simulink model "Hexalock.slx"  (R2026b)
(part 2 of 5)

  MultiStateImage8 : CustomWebBlock  LabelPosition=Hide  ShowInitialText=on  Configuration="{\"components\":[{\"name\":\"BackgroundImageComponent\",\"settings\":{\"image\":{\"size\":[0,0],\"src\":\"default\",\"srcOrientation\":\"Right\"},\"position\":[0,0,1,1],\"scaleMode\":\"0\"}},{\"name\":\"MultistateImageStateComponent\",\"settings\":{\"applyDefaults\":true,\"position\":[0,0,1,1],\"states\":[{\"image\":{\"size\":[0.7746478873239436,1],\"src\":\"data:image\\/svg+xml;base64,PHN2ZyB4bWxucz0iaHR0cDovL3d3dy53My5vcmcvMjAwMC9zdmciIHdpZHRoPSIyMjAiIGhlaWdodD0iMjg0IiB2aWV3Qm94PSIwIDAgMjIwIDI4NCIgcm9sZT0iaW1nIiA+Cjx0aXRsZT5IRVhBTE9DSyBtb2R1bGFyIGludGVyZmFjZSBhc3NldDwvdGl0bGU+CjxkZWZzPjwvZGVmcz4KICAgICAgPHJlY3QgeD0iOCIgeT0iOCIgd2lkdGg9IjIwNCIgaGVpZ2h0PSIyNjgiIHJ4PSIxNCIgZmlsbD0iIzExMUMyMiIgc3Ryb2tlPSIjNTM2NjZFIiBzdHJva2Utd2lkdGg9IjIiLz4KICAgICAgPHJlY3QgeD0iMTIiIHk9IjEyIiB3aWR0 ...(+3224 chars)\",\"srcOrientation\":\"Right\"},\"position\":[0,0,1,1],\"value\":[]},{\"image\":{\"size\":[0,0],\"src\":\"data:image\\/svg+xml;base64,PHN2ZyB4bWxucz0iaHR0cDovL3d3dy53My5vcmcvMjAwMC9zdmciIHdpZHRoPSIyMjAiIGhlaWdodD0iMjg0IiB2aWV3Qm94PSIwIDAgMjIwIDI4NCIgcm9sZT0iaW1nIiA+Cjx0aXRsZT5IRVhBTE9DSyBtb2R1bGFyIGludGVyZmFjZSBhc3NldDwvdGl0bGU+CjxkZWZzPjwvZGVmcz4KICAgICAgPHJlY3QgeD0iOCIgeT0iOCIgd2lkdGg9IjIwNCIgaGVpZ2h0PSIyNjgiIHJ4PSIxNCIgZmlsbD0iIzExMUMyMiIgc3Ryb2tlPSIjNTM2NjZFIiBzdHJva2Utd2lkdGg9IjIiLz4KICAgICAgPHJlY3QgeD0iMTIiIHk9IjEyIiB3aWR0 ...(+3224 chars)\",\"srcOrientation\":\"Right\"},\"position\":[0,0,1,1],\"value\":\"0\"},{\"image\":{\"size\":[0,0],\"src\":\"data:image\\/svg+xml;base64,PHN2ZyB4bWxucz0iaHR0cDovL3d3dy53My5vcmcvMjAwMC9zdmciIHdpZHRoPSIyMjAiIGhlaWdodD0iMjg0IiB2aWV3Qm94PSIwIDAgMjIwIDI4NCIgcm9sZT0iaW1nIiA+Cjx0aXRsZT5IRVhBTE9DSyBtb2R1bGFyIGludGVyZmFjZSBhc3NldDwvdGl0bGU+CjxkZWZzPjwvZGVmcz4KICAgICAgPHJlY3QgeD0iOCIgeT0iOCIgd2lkdGg9IjIwNCIgaGVpZ2h0PSIyNjgiIHJ4PSIxNCIgZmlsbD0iIzExMUMyMiIgc3Ryb2tlPSIjNTM2NjZFIiBzdHJva2Utd2lkdGg9IjIiLz4KICAgICAgPHJlY3QgeD0iMTIiIHk9IjEyIiB3aWR0 ...(+3220 chars)\",\"srcOrientation\":\"Right\"},\"position\":[0,0,1,1],\"value\":\"1\"},{\"image\":{\"size\":[0,0],\"src\":\"data:image\\/svg+xml;base64,PHN2ZyB4bWxucz0iaHR0cDovL3d3dy53My5vcmcvMjAwMC9zdmciIHdpZHRoPSIyMjAiIGhlaWdodD0iMjg0IiB2aWV3Qm94PSIwIDAgMjIwIDI4NCIgcm9sZT0iaW1nIiA+Cjx0aXRsZT5IRVhBTE9DSyBtb2R1bGFyIGludGVyZmFjZSBhc3NldDwvdGl0bGU+CjxkZWZzPjwvZGVmcz4KICAgICAgPHJlY3QgeD0iOCIgeT0iOCIgd2lkdGg9IjIwNCIgaGVpZ2h0PSIyNjgiIHJ4PSIxNCIgZmlsbD0iIzExMUMyMiIgc3Ryb2tlPSIjQjk4NTZFIiBzdHJva2Utd2lkdGg9IjIuNiIvPgogICAgICA8cmVjdCB4PSIxMiIgeT0iMTIiIHdp ...(+3488 chars)\",\"srcOrientation\":\"Right\"},\"position\":[0,0,1,1],\"value\":\"2\"},{\"image\":{\"size\":[0,0],\"src\":\"data:image\\/svg+xml;base64,PHN2ZyB4bWxucz0iaHR0cDovL3d3dy53My5vcmcvMjAwMC9zdmciIHdpZHRoPSIyMjAiIGhlaWdodD0iMjg0IiB2aWV3Qm94PSIwIDAgMjIwIDI4NCIgcm9sZT0iaW1nIiA+Cjx0aXRsZT5IRVhBTE9DSyBtb2R1bGFyIGludGVyZmFjZSBhc3NldDwvdGl0bGU+CjxkZWZzPjwvZGVmcz4KICAgICAgPHJlY3QgeD0iOCIgeT0iOCIgd2lkdGg9IjIwNCIgaGVpZ2h0PSIyNjgiIHJ4PSIxNCIgZmlsbD0iIzExMUMyMiIgc3Ryb2tlPSIjQjk4NTZFIiBzdHJva2Utd2lkdGg9IjIuNiIvPgogICAgICA8cmVjdCB4PSIxMiIgeT0iMTIiIHdp ...(+3484 chars)\",\"srcOrientation\":\"Right\"},\"position\":[0,0,1,1],\"value\":\"3\"},{\"image\":{\"size\":[0,0],\"src\":\"data:image\\/svg+xml;base64,PHN2ZyB4bWxucz0iaHR0cDovL3d3dy53My5vcmcvMjAwMC9zdmciIHdpZHRoPSIyMjAiIGhlaWdodD0iMjg0IiB2aWV3Qm94PSIwIDAgMjIwIDI4NCIgcm9sZT0iaW1nIiA+Cjx0aXRsZT5IRVhBTE9DSyBtb2R1bGFyIGludGVyZmFjZSBhc3NldDwvdGl0bGU+CjxkZWZzPjwvZGVmcz4KICAgICAgPHJlY3QgeD0iOCIgeT0iOCIgd2lkdGg9IjIwNCIgaGVpZ2h0PSIyNjgiIHJ4PSIxNCIgZmlsbD0iIzExMUMyMiIgc3Ryb2tlPSIjQjk4NTZFIiBzdHJva2Utd2lkdGg9IjIuNiIvPgogICAgICA8cmVjdCB4PSIxMiIgeT0iMTIiIHdp ...(+3532 chars)\",\"srcOrientation\":\"Right\"},\"position\":[0,0,1,1],\"value\":\"4\"},{\"image\":{\"size\":[0,0],\"src\":\"data:image\\/svg+xml;base64,PHN2ZyB4bWxucz0iaHR0cDovL3d3dy53My5vcmcvMjAwMC9zdmciIHdpZHRoPSIyMjAiIGhlaWdodD0iMjg0IiB2aWV3Qm94PSIwIDAgMjIwIDI4NCIgcm9sZT0iaW1nIiA+Cjx0aXRsZT5IRVhBTE9DSyBtb2R1bGFyIGludGVyZmFjZSBhc3NldDwvdGl0bGU+CjxkZWZzPjwvZGVmcz4KICAgICAgPHJlY3QgeD0iOCIgeT0iOCIgd2lkdGg9IjIwNCIgaGVpZ2h0PSIyNjgiIHJ4PSIxNCIgZmlsbD0iIzExMUMyMiIgc3Ryb2tlPSIjQjk4NTZFIiBzdHJva2Utd2lkdGg9IjIuNiIvPgogICAgICA8cmVjdCB4PSIxMiIgeT0iMTIiIHdp ...(+3532 chars)\",\"srcOrientation\":\"Right\"},\"position\":[0,0,1,1],\"value\":\"5\"},{\"image\":{\"size\":[0,0],\"src\":\"data:image\\/svg+xml;base64,PHN2ZyB4bWxucz0iaHR0cDovL3d3dy53My5vcmcvMjAwMC9zdmciIHdpZHRoPSIyMjAiIGhlaWdodD0iMjg0IiB2aWV3Qm94PSIwIDAgMjIwIDI4NCIgcm9sZT0iaW1nIiA+Cjx0aXRsZT5IRVhBTE9DSyBtb2R1bGFyIGludGVyZmFjZSBhc3NldDwvdGl0bGU+CjxkZWZzPjwvZGVmcz4KICAgICAgPHJlY3QgeD0iOCIgeT0iOCIgd2lkdGg9IjIwNCIgaGVpZ2h0PSIyNjgiIHJ4PSIxNCIgZmlsbD0iIzExMUMyMiIgc3Ryb2tlPSIjQjk4NTZFIiBzdHJva2Utd2lkdGg9IjIuNiIvPgogICAgICA8cmVjdCB4PSIxMiIgeT0iMTIiIHdp ...(+3532 chars)\",\"srcOrientation\":\"Right\"},\"position\":[0,0,1,1],\"value\":\"6\"},{\"image\":{\"size\":[0,0],\"src\":\"data:image\\/svg+xml;base64,PHN2ZyB4bWxucz0iaHR0cDovL3d3dy53My5vcmcvMjAwMC9zdmciIHdpZHRoPSIyMjAiIGhlaWdodD0iMjg0IiB2aWV3Qm94PSIwIDAgMjIwIDI4NCIgcm9sZT0iaW1nIiA+Cjx0aXRsZT5IRVhBTE9DSyBtb2R1bGFyIGludGVyZmFjZSBhc3NldDwvdGl0bGU+CjxkZWZzPjwvZGVmcz4KICAgICAgPHJlY3QgeD0iOCIgeT0iOCIgd2lkdGg9IjIwNCIgaGVpZ2h0PSIyNjgiIHJ4PSIxNCIgZmlsbD0iIzExMUMyMiIgc3Ryb2tlPSIjQjk4NTZFIiBzdHJva2Utd2lkdGg9IjIuNiIvPgogICAgICA8cmVjdCB4PSIxMiIgeT0iMTIiIHdp ...(+3524 chars)\",\"srcOrientation\":\"Right\"},\"position\":[0,0,1,1],\"value\":\"7\"},{\"image\":{\"size\":[0,0],\"src\":\"data:image\\/svg+xml;base64,PHN2ZyB4bWxucz0iaHR0cDovL3d3dy53My5vcmcvMjAwMC9zdmciIHdpZHRoPSIyMjAiIGhlaWdodD0iMjg0IiB2aWV3Qm94PSIwIDAgMjIwIDI4NCIgcm9sZT0iaW1nIiA+Cjx0aXRsZT5IRVhBTE9DSyBtb2R1bGFyIGludGVyZmFjZSBhc3NldDwvdGl0bGU+CjxkZWZzPjwvZGVmcz4KICAgICAgPHJlY3QgeD0iOCIgeT0iOCIgd2lkdGg9IjIwNCIgaGVpZ2h0PSIyNjgiIHJ4PSIxNCIgZmlsbD0iIzExMUMyMiIgc3Ryb2tlPSIjQjk4NTZFIiBzdHJva2Utd2lkdGg9IjIuNiIvPgogICAgICA8cmVjdCB4PSIxMiIgeT0iMTIiIHdp ...(+3532 chars)\",\"srcOrientation\":\"Right\"},\"position\":[0,0,1,1],\"value\":\"8\"},{\"image\":{\"size\":[0,0],\"src\":\"data:image\\/svg+xml;base64,PHN2ZyB4bWxucz0iaHR0cDovL3d3dy53My5vcmcvMjAwMC9zdmciIHdpZHRoPSIyMjAiIGhlaWdodD0iMjg0IiB2aWV3Qm94PSIwIDAgMjIwIDI4NCIgcm9sZT0iaW1nIiA+Cjx0aXRsZT5IRVhBTE9DSyBtb2R1bGFyIGludGVyZmFjZSBhc3NldDwvdGl0bGU+CjxkZWZzPjwvZGVmcz4KICAgICAgPHJlY3QgeD0iOCIgeT0iOCIgd2lkdGg9IjIwNCIgaGVpZ2h0PSIyNjgiIHJ4PSIxNCIgZmlsbD0iIzExMUMyMiIgc3Ryb2tlPSIjQjk4NTZFIiBzdHJva2Utd2lkdGg9IjIuNiIvPgogICAgICA8cmVjdCB4PSIxMiIgeT0iMTIiIHdp ...(+3532 chars)\",\"srcOrientation\":\"Right\"},\"position\":[0,0,1,1],\"value\":\"9\"},{\"image\":{\"size\":[0,0],\"src\":\"data:image\\/svg+xml;base64,PHN2ZyB4bWxucz0iaHR0cDovL3d3dy53My5vcmcvMjAwMC9zdmciIHdpZHRoPSIyMjAiIGhlaWdodD0iMjg0IiB2aWV3Qm94PSIwIDAgMjIwIDI4NCIgcm9sZT0iaW1nIiA+Cjx0aXRsZT5IRVhBTE9DSyBtb2R1bGFyIGludGVyZmFjZSBhc3NldDwvdGl0bGU+CjxkZWZzPjwvZGVmcz4KICAgICAgPHJlY3QgeD0iOCIgeT0iOCIgd2lkdGg9IjIwNCIgaGVpZ2h0PSIyNjgiIHJ4PSIxNCIgZmlsbD0iIzExMUMyMiIgc3Ryb2tlPSIjQjk4NTZFIiBzdHJva2Utd2lkdGg9IjIuNiIvPgogICAgICA8cmVjdCB4PSIxMiIgeT0iMTIiIHdp ...(+3532 chars)\",\"srcOrientation\":\"Right\"},\"position\":[0,0,1,1],\"value\":\"10\"},{\"image\":{\"size\":[0,0],\"src\":\"data:image\\/svg+xml;base64,PHN2ZyB4bWxucz0iaHR0cDovL3d3dy53My5vcmcvMjAwMC9zdmciIHdpZHRoPSIyMjAiIGhlaWdodD0iMjg0IiB2aWV3Qm94PSIwIDAgMjIwIDI4NCIgcm9sZT0iaW1nIiA+Cjx0aXRsZT5IRVhBTE9DSyBtb2R1bGFyIGludGVyZmFjZSBhc3NldDwvdGl0bGU+CjxkZWZzPjwvZGVmcz4KICAgICAgPHJlY3QgeD0iOCIgeT0iOCIgd2lkdGg9IjIwNCIgaGVpZ2h0PSIyNjgiIHJ4PSIxNCIgZmlsbD0iIzExMUMyMiIgc3Ryb2tlPSIjNTM2NjZFIiBzdHJva2Utd2lkdGg9IjIiLz4KICAgICAgPHJlY3QgeD0iMTIiIHk9IjEyIiB3aWR0 ...(+3220 chars)\",\"srcOrientation\":\"Right\"},\"position\":[0,0,1,1],\"value\":\"11\"},{\"image\":{\"size\":[0,0],\"src\":\"data:image\\/svg+xml;base64,PHN2ZyB4bWxucz0iaHR0cDovL3d3dy53My5vcmcvMjAwMC9zdmciIHdpZHRoPSIyMjAiIGhlaWdodD0iMjg0IiB2aWV3Qm94PSIwIDAgMjIwIDI4NCIgcm9sZT0iaW1nIiA+Cjx0aXRsZT5IRVhBTE9DSyBtb2R1bGFyIGludGVyZmFjZSBhc3NldDwvdGl0bGU+CjxkZWZzPjxsaW5lYXJHcmFkaWVudCBpZD0ia3JhZnRGcm9udCIgeDE9IjAiIHkxPSIwIiB4Mj0iMSIgeTI9IjEiPjxzdG9wIHN0b3AtY29sb3I9IiNEM0I5OUEiLz48c3RvcCBvZmZzZXQ9IjEiIHN0b3AtY29sb3I9IiNBMzgzNjMiLz48L2xpbmVhckdyYWRpZW50Pjxs ...(+4752 chars)\",\"srcOrientation\":\"Right\"},\"position\":[0,0,1,1],\"value\":\"20\"},{\"image\":{\"size\":[0,0],\"src\":\"data:image\\/svg+xml;base64,PHN2ZyB4bWxucz0iaHR0cDovL3d3dy53My5vcmcvMjAwMC9zdmciIHdpZHRoPSIyMjAiIGhlaWdodD0iMjg0IiB2aWV3Qm94PSIwIDAgMjIwIDI4NCIgcm9sZT0iaW1nIiA+Cjx0aXRsZT5IRVhBTE9DSyBtb2R1bGFyIGludGVyZmFjZSBhc3NldDwvdGl0bGU+CjxkZWZzPjxsaW5lYXJHcmFkaWVudCBpZD0ia3JhZnRGcm9udCIgeDE9IjAiIHkxPSIwIiB4Mj0iMSIgeTI9IjEiPjxzdG9wIHN0b3AtY29sb3I9IiNEM0I5OUEiLz48c3RvcCBvZmZzZXQ9IjEiIHN0b3AtY29sb3I9IiNBMzgzNjMiLz48L2xpbmVhckdyYWRpZW50Pjxs ...(+7264 chars)\",\"srcOrientation\":\"Right\"},\"position\":[0,0,1,1],\"value\":\"21\"},{\"image\":{\"size\":[0,0],\"src\":\"data:image\\/svg+xml;base64,PHN2ZyB4bWxucz0iaHR0cDovL3d3dy53My5vcmcvMjAwMC9zdmciIHdpZHRoPSIyMjAiIGhlaWdodD0iMjg0IiB2aWV3Qm94PSIwIDAgMjIwIDI4NCIgcm9sZT0iaW1nIiA+Cjx0aXRsZT5IRVhBTE9DSyBtb2R1bGFyIGludGVyZmFjZSBhc3NldDwvdGl0bGU+CjxkZWZzPjxsaW5lYXJHcmFkaWVudCBpZD0ia3JhZnRGcm9udCIgeDE9IjAiIHkxPSIwIiB4Mj0iMSIgeTI9IjEiPjxzdG9wIHN0b3AtY29sb3I9IiNEM0I5OUEiLz48c3RvcCBvZmZzZXQ9IjEiIHN0b3AtY29sb3I9IiNBMzgzNjMiLz48L2xpbmVhckdyYWRpZW50Pjxs ...(+7264 chars)\",\"srcOrientation\":\"Right\"},\"position\":[0,0,1,1],\"value\":\"22\"},{\"image\":{\"size\":[0,0],\"src\":\"data:image\\/svg+xml;base64,PHN2ZyB4bWxucz0iaHR0cDovL3d3dy53My5vcmcvMjAwMC9zdmciIHdpZHRoPSIyMjAiIGhlaWdodD0iMjg0IiB2aWV3Qm94PSIwIDAgMjIwIDI4NCIgcm9sZT0iaW1nIiA+Cjx0aXRsZT5IRVhBTE9DSyBtb2R1bGFyIGludGVyZmFjZSBhc3NldDwvdGl0bGU+CjxkZWZzPjxsaW5lYXJHcmFkaWVudCBpZD0ia3JhZnRGcm9udCIgeDE9IjAiIHkxPSIwIiB4Mj0iMSIgeTI9IjEiPjxzdG9wIHN0b3AtY29sb3I9IiNEM0I5OUEiLz48c3RvcCBvZmZzZXQ9IjEiIHN0b3AtY29sb3I9IiNBMzgzNjMiLz48L2xpbmVhckdyYWRpZW50Pjxs ...(+7264 chars)\",\"srcOrientation\":\"Right\"},\"position\":[0,0,1,1],\"value\":\"23\"},{\"image\":{\"size\":[0,0],\"src\":\"data:image\\/svg+xml;base64,PHN2ZyB4bWxucz0iaHR0cDovL3d3dy53My5vcmcvMjAwMC9zdmciIHdpZHRoPSIyMjAiIGhlaWdodD0iMjg0IiB2aWV3Qm94PSIwIDAgMjIwIDI4NCIgcm9sZT0iaW1nIiA+Cjx0aXRsZT5IRVhBTE9DSyBtb2R1bGFyIGludGVyZmFjZSBhc3NldDwvdGl0bGU+CjxkZWZzPjxsaW5lYXJHcmFkaWVudCBpZD0ia3JhZnRGcm9udCIgeDE9IjAiIHkxPSIwIiB4Mj0iMSIgeTI9IjEiPjxzdG9wIHN0b3AtY29sb3I9IiNEM0I5OUEiLz48c3RvcCBvZmZzZXQ9IjEiIHN0b3AtY29sb3I9IiNBMzgzNjMiLz48L2xpbmVhckdyYWRpZW50Pjxs ...(+7260 chars)\",\"srcOrientation\":\"Right\"},\"position\":[0,0,1,1],\"value\":\"24\"},{\"image\":{\"size\":[0,0],\"src\":\"data:image\\/svg+xml;base64,PHN2ZyB4bWxucz0iaHR0cDovL3d3dy53My5vcmcvMjAwMC9zdmciIHdpZHRoPSIyMjAiIGhlaWdodD0iMjg0IiB2aWV3Qm94PSIwIDAgMjIwIDI4NCIgcm9sZT0iaW1nIiA+Cjx0aXRsZT5IRVhBTE9DSyBtb2R1bGFyIGludGVyZmFjZSBhc3NldDwvdGl0bGU+CjxkZWZzPjxsaW5lYXJHcmFkaWVudCBpZD0ia3JhZnRGcm9udCIgeDE9IjAiIHkxPSIwIiB4Mj0iMSIgeTI9IjEiPjxzdG9wIHN0b3AtY29sb3I9IiNEM0I5OUEiLz48c3RvcCBvZmZzZXQ9IjEiIHN0b3AtY29sb3I9IiNBMzgzNjMiLz48L2xpbmVhckdyYWRpZW50Pjxs ...(+7264 chars)\",\"srcOrientation\":\"Right\"},\"position\":[0,0,1,1],\"value\":\"25\"},{\"image\":{\"size\":[0,0],\"src\":\"data:image\\/svg+xml;base64,PHN2ZyB4bWxucz0iaHR0cDovL3d3dy53My5vcmcvMjAwMC9zdmciIHdpZHRoPSIyMjAiIGhlaWdodD0iMjg0IiB2aWV3Qm94PSIwIDAgMjIwIDI4NCIgcm9sZT0iaW1nIiA+Cjx0aXRsZT5IRVhBTE9DSyBtb2R1bGFyIGludGVyZmFjZSBhc3NldDwvdGl0bGU+CjxkZWZzPjxsaW5lYXJHcmFkaWVudCBpZD0ia3JhZnRGcm9udCIgeDE9IjAiIHkxPSIwIiB4Mj0iMSIgeTI9IjEiPjxzdG9wIHN0b3AtY29sb3I9IiNEM0I5OUEiLz48c3RvcCBvZmZzZXQ9IjEiIHN0b3AtY29sb3I9IiNBMzgzNjMiLz48L2xpbmVhckdyYWRpZW50Pjxs ...(+7272 chars)\",\"srcOrientation\":\"Right\"},\"position\":[0,0,1,1],\"value\":\"26\"},{\"image\":{\"size\":[0,0],\"src\":\"data:image\\/svg+xml;base64,PHN2ZyB4bWxucz0iaHR0cDovL3d3dy53My5vcmcvMjAwMC9zdmciIHdpZHRoPSIyMjAiIGhlaWdodD0iMjg0IiB2aWV3Qm94PSIwIDAgMjIwIDI4NCIgcm9sZT0iaW1nIiA+Cjx0aXRsZT5IRVhBTE9DSyBtb2R1bGFyIGludGVyZmFjZSBhc3NldDwvdGl0bGU+CjxkZWZzPjxsaW5lYXJHcmFkaWVudCBpZD0ia3JhZnRGcm9udCIgeDE9IjAiIHkxPSIwIiB4Mj0iMSIgeTI9IjEiPjxzdG9wIHN0b3AtY29sb3I9IiNEM0I5OUEiLz48c3RvcCBvZmZzZXQ9IjEiIHN0b3AtY29sb3I9IiNBMzgzNjMiLz48L2xpbmVhckdyYWRpZW50Pjxs ...(+7264 chars)\",\"srcOrientation\":\"Right\"},\"position\":[0,0,1,1],\"value\":\"27\"},{\"image\":{\"size\":[0,0],\"src\":\"data:image\\/svg+xml;base64,PHN2ZyB4bWxucz0iaHR0cDovL3d3dy53My5vcmcvMjAwMC9zdmciIHdpZHRoPSIyMjAiIGhlaWdodD0iMjg0IiB2aWV3Qm94PSIwIDAgMjIwIDI4NCIgcm9sZT0iaW1nIiA+Cjx0aXRsZT5IRVhBTE9DSyBtb2R1bGFyIGludGVyZmFjZSBhc3NldDwvdGl0bGU+CjxkZWZzPjxsaW5lYXJHcmFkaWVudCBpZD0ia3JhZnRGcm9udCIgeDE9IjAiIHkxPSIwIiB4Mj0iMSIgeTI9IjEiPjxzdG9wIHN0b3AtY29sb3I9IiNEM0I5OUEiLz48c3RvcCBvZmZzZXQ9IjEiIHN0b3AtY29sb3I9IiNBMzgzNjMiLz48L2xpbmVhckdyYWRpZW50Pjxs ...(+7268 chars)\",\"srcOrientation\":\"Right\"},\"position\":[0,0,1,1],\"value\":\"28\"},{\"image\":{\"size\":[0,0],\"src\":\"data:image\\/svg+xml;base64,PHN2ZyB4bWxucz0iaHR0cDovL3d3dy53My5vcmcvMjAwMC9zdmciIHdpZHRoPSIyMjAiIGhlaWdodD0iMjg0IiB2aWV3Qm94PSIwIDAgMjIwIDI4NCIgcm9sZT0iaW1nIiA+Cjx0aXRsZT5IRVhBTE9DSyBtb2R1bGFyIGludGVyZmFjZSBhc3NldDwvdGl0bGU+CjxkZWZzPjxsaW5lYXJHcmFkaWVudCBpZD0ia3JhZnRGcm9udCIgeDE9IjAiIHkxPSIwIiB4Mj0iMSIgeTI9IjEiPjxzdG9wIHN0b3AtY29sb3I9IiNEM0I5OUEiLz48c3RvcCBvZmZzZXQ9IjEiIHN0b3AtY29sb3I9IiNBMzgzNjMiLz48L2xpbmVhckdyYWRpZW50Pjxs ...(+7268 chars)\",\"srcOrientation\":\"Right\"},\"position\":[0,0,1,1],\"value\":\"29\"},{\"image\":{\"size\":[0,0],\"src\":\"data:image\\/svg+xml;base64,PHN2ZyB4bWxucz0iaHR0cDovL3d3dy53My5vcmcvMjAwMC9zdmciIHdpZHRoPSIyMjAiIGhlaWdodD0iMjg0IiB2aWV3Qm94PSIwIDAgMjIwIDI4NCIgcm9sZT0iaW1nIiA+Cjx0aXRsZT5IRVhBTE9DSyBtb2R1bGFyIGludGVyZmFjZSBhc3NldDwvdGl0bGU+CjxkZWZzPjxsaW5lYXJHcmFkaWVudCBpZD0ia3JhZnRGcm9udCIgeDE9IjAiIHkxPSIwIiB4Mj0iMSIgeTI9IjEiPjxzdG9wIHN0b3AtY29sb3I9IiNEM0I5OUEiLz48c3RvcCBvZmZzZXQ9IjEiIHN0b3AtY29sb3I9IiNBMzgzNjMiLz48L2xpbmVhckdyYWRpZW50Pjxs ...(+7268 chars)\",\"srcOrientation\":\"Right\"},\"position\":[0,0,1,1],\"value\":\"30\"},{\"image\":{\"size\":[0,0],\"src\":\"data:image\\/svg+xml;base64,PHN2ZyB4bWxucz0iaHR0cDovL3d3dy53My5vcmcvMjAwMC9zdmciIHdpZHRoPSIyMjAiIGhlaWdodD0iMjg0IiB2aWV3Qm94PSIwIDAgMjIwIDI4NCIgcm9sZT0iaW1nIiA+Cjx0aXRsZT5IRVhBTE9DSyBtb2R1bGFyIGludGVyZmFjZSBhc3NldDwvdGl0bGU+CjxkZWZzPjxsaW5lYXJHcmFkaWVudCBpZD0ia3JhZnRGcm9udCIgeDE9IjAiIHkxPSIwIiB4Mj0iMSIgeTI9IjEiPjxzdG9wIHN0b3AtY29sb3I9IiNEM0I5OUEiLz48c3RvcCBvZmZzZXQ9IjEiIHN0b3AtY29sb3I9IiNBMzgzNjMiLz48L2xpbmVhckdyYWRpZW50Pjxs ...(+4756 chars)\",\"srcOrientation\":\"Right\"},\"position\":[0,0,1,1],\"value\":\"31\"},{\"image\":{\"size\":[0,0],\"src\":\"data:image\\/svg+xml;base64,PHN2ZyB4bWxucz0iaHR0cDovL3d3dy53My5vcmcvMjAwMC9zdmciIHdpZHRoPSIyMjAiIGhlaWdodD0iMjg0IiB2aWV3Qm94PSIwIDAgMjIwIDI4NCIgcm9sZT0iaW1nIiA+Cjx0aXRsZT5IRVhBTE9DSyBtb2R1bGFyIGludGVyZmFjZSBhc3NldDwvdGl0bGU+CjxkZWZzPjxsaW5lYXJHcmFkaWVudCBpZD0ia3JhZnRGcm9udCIgeDE9IjAiIHkxPSIwIiB4Mj0iMSIgeTI9IjEiPjxzdG9wIHN0b3AtY29sb3I9IiNEM0I5OUEiLz48c3RvcCBvZmZzZXQ9IjEiIHN0b3AtY29sb3I9IiNBMzgzNjMiLz48L2xpbmVhckdyYWRpZW50Pjxs ...(+4752 chars)\",\"srcOrientation\":\"Right\"},\"position\":[0,0,1,1],\"value\":\"32\"},{\"image\":{\"size\":[0,0],\"src\":\"data:image\\/svg+xml;base64,PHN2ZyB4bWxucz0iaHR0cDovL3d3dy53My5vcmcvMjAwMC9zdmciIHdpZHRoPSIyMjAiIGhlaWdodD0iMjg0IiB2aWV3Qm94PSIwIDAgMjIwIDI4NCIgcm9sZT0iaW1nIiA+Cjx0aXRsZT5IRVhBTE9DSyBtb2R1bGFyIGludGVyZmFjZSBhc3NldDwvdGl0bGU+CjxkZWZzPjxsaW5lYXJHcmFkaWVudCBpZD0ia3JhZnRGcm9udCIgeDE9IjAiIHkxPSIwIiB4Mj0iMSIgeTI9IjEiPjxzdG9wIHN0b3AtY29sb3I9IiNEM0I5OUEiLz48c3RvcCBvZmZzZXQ9IjEiIHN0b3AtY29sb3I9IiNBMzgzNjMiLz48L2xpbmVhckdyYWRpZW50Pjxs ...(+6860 chars)\",\"srcOrientation\":\"Right\"},\"position\":[0,0,1,1],\"value\":\"33\"},{\"image\":{\"size\":[0,0],\"src\":\"data:image\\/svg+xml;base64,PHN2ZyB4bWxucz0iaHR0cDovL3d3dy53My5vcmcvMjAwMC9zdmciIHdpZHRoPSIyMjAiIGhlaWdodD0iMjg0IiB2aWV3Qm94PSIwIDAgMjIwIDI4NCIgcm9sZT0iaW1nIiA+Cjx0aXRsZT5IRVhBTE9DSyBtb2R1bGFyIGludGVyZmFjZSBhc3NldDwvdGl0bGU+CjxkZWZzPjxsaW5lYXJHcmFkaWVudCBpZD0ia3JhZnRGcm9udCIgeDE9IjAiIHkxPSIwIiB4Mj0iMSIgeTI9IjEiPjxzdG9wIHN0b3AtY29sb3I9IiNEM0I5OUEiLz48c3RvcCBvZmZzZXQ9IjEiIHN0b3AtY29sb3I9IiNBMzgzNjMiLz48L2xpbmVhckdyYWRpZW50Pjxs ...(+6860 chars)\",\"srcOrientation\":\"Right\"},\"position\":[0,0,1,1],\"value\":\"34\"},{\"image\":{\"size\":[0,0],\"src\":\"data:image\\/svg+xml;base64,PHN2ZyB4bWxucz0iaHR0cDovL3d3dy53My5vcmcvMjAwMC9zdmciIHdpZHRoPSIyMjAiIGhlaWdodD0iMjg0IiB2aWV3Qm94PSIwIDAgMjIwIDI4NCIgcm9sZT0iaW1nIiA+Cjx0aXRsZT5IRVhBTE9DSyBtb2R1bGFyIGludGVyZmFjZSBhc3NldDwvdGl0bGU+CjxkZWZzPjxsaW5lYXJHcmFkaWVudCBpZD0ia3JhZnRGcm9udCIgeDE9IjAiIHkxPSIwIiB4Mj0iMSIgeTI9IjEiPjxzdG9wIHN0b3AtY29sb3I9IiNEM0I5OUEiLz48c3RvcCBvZmZzZXQ9IjEiIHN0b3AtY29sb3I9IiNBMzgzNjMiLz48L2xpbmVhckdyYWRpZW50Pjxs ...(+6860 chars)\",\"srcOrientation\":\"Right\"},\"position\":[0,0,1,1],\"value\":\"35\"},{\"image\":{\"size\":[0,0],\"src\":\"data:image\\/svg+xml;base64,PHN2ZyB4bWxucz0iaHR0cDovL3d3dy53My5vcmcvMjAwMC9zdmciIHdpZHRoPSIyMjAiIGhlaWdodD0iMjg0IiB2aWV3Qm94PSIwIDAgMjIwIDI4NCIgcm9sZT0iaW1nIiA+DQo8dGl0bGU+SEVYQUxPQ0sgbW9kdWxhciBpbnRlcmZhY2UgYXNzZXQ8L3RpdGxlPg0KPGRlZnM+PGxpbmVhckdyYWRpZW50IGlkPSJrcmFmdEZyb250IiB4MT0iMCIgeTE9IjAiIHgyPSIxIiB5Mj0iMSI+PHN0b3Agc3RvcC1jb2xvcj0iI0QzQjk5QSIvPjxzdG9wIG9mZnNldD0iMSIgc3RvcC1jb2xvcj0iI0EzODM2MyIvPjwvbGluZWFyR3JhZGllbnQ+ ...(+6912 chars)\",\"srcOrientation\":\"Right\"},\"position\":[0,0,1,1],\"value\":\"36\"},{\"image\":{\"size\":[0,0],\"src\":\"data:image\\/svg+xml;base64,PHN2ZyB4bWxucz0iaHR0cDovL3d3dy53My5vcmcvMjAwMC9zdmciIHdpZHRoPSIyMjAiIGhlaWdodD0iMjg0IiB2aWV3Qm94PSIwIDAgMjIwIDI4NCIgcm9sZT0iaW1nIiA+DQo8dGl0bGU+SEVYQUxPQ0sgbW9kdWxhciBpbnRlcmZhY2UgYXNzZXQ8L3RpdGxlPg0KPGRlZnM+PGxpbmVhckdyYWRpZW50IGlkPSJrcmFmdEZyb250IiB4MT0iMCIgeTE9IjAiIHgyPSIxIiB5Mj0iMSI+PHN0b3Agc3RvcC1jb2xvcj0iI0QzQjk5QSIvPjxzdG9wIG9mZnNldD0iMSIgc3RvcC1jb2xvcj0iI0EzODM2MyIvPjwvbGluZWFyR3JhZGllbnQ+ ...(+6912 chars)\",\"srcOrientation\":\"Right\"},\"position\":[0,0,1,1],\"value\":\"37\"},{\"image\":{\"size\":[0,0],\"src\":\"data:image\\/svg+xml;base64,PHN2ZyB4bWxucz0iaHR0cDovL3d3dy53My5vcmcvMjAwMC9zdmciIHdpZHRoPSIyMjAiIGhlaWdodD0iMjg0IiB2aWV3Qm94PSIwIDAgMjIwIDI4NCIgcm9sZT0iaW1nIiA+DQo8dGl0bGU+SEVYQUxPQ0sgbW9kdWxhciBpbnRlcmZhY2UgYXNzZXQ8L3RpdGxlPg0KPGRlZnM+PGxpbmVhckdyYWRpZW50IGlkPSJrcmFmdEZyb250IiB4MT0iMCIgeTE9IjAiIHgyPSIxIiB5Mj0iMSI+PHN0b3Agc3RvcC1jb2xvcj0iI0QzQjk5QSIvPjxzdG9wIG9mZnNldD0iMSIgc3RvcC1jb2xvcj0iI0EzODM2MyIvPjwvbGluZWFyR3JhZGllbnQ+ ...(+6912 chars)\",\"srcOrientation\":\"Right\"},\"position\":[0,0,1,1],\"value\":\"38\"}],\"valueType\":\"discrete\"}},{\"name\":\"ForegroundImageComponent\",\"settings\":{\"image\":{\"size\":[0,0],\"src\":\"default\",\"srcOrientation\":\"Right\"},\"isForeground\":1,\"position\":[0,0,1,1],\"scaleMode\":\"0\"}}],\"derived\":{\"blockParameters\":{\"DefaultImage\":\"data:image\\/svg+xml;base64,PHN2ZyB4bWxucz0iaHR0cDovL3d3dy53My5vcmcvMjAwMC9zdmciIHdpZHRoPSIyMjAiIGhlaWdodD0iMjg0IiB2aWV3Qm94PSIwIDAgMjIwIDI4NCIgcm9sZT0iaW1nIiA+Cjx0aXRsZT5IRVhBTE9DSyBtb2R1bGFyIGludGVyZmFjZSBhc3NldDwvdGl0bGU+CjxkZWZzPjwvZGVmcz4KICAgICAgPHJlY3QgeD0iOCIgeT0iOCIgd2lkdGg9IjIwNCIgaGVpZ2h0PSIyNjgiIHJ4PSIxNCIgZmlsbD0iIzExMUMyMiIgc3Ryb2tlPSIjNTM2NjZFIiBzdHJva2Utd2lkdGg9IjIiLz4KICAgICAgPHJlY3QgeD0iMTIiIHk9IjEyIiB3aWR0 ...(+3224 chars)\",\"StateValueType\":\"discrete\",\"States\":[{\"image\":\"data:image\\/svg+xml;base64,PHN2ZyB4bWxucz0iaHR0cDovL3d3dy53My5vcmcvMjAwMC9zdmciIHdpZHRoPSIyMjAiIGhlaWdodD0iMjg0IiB2aWV3Qm94PSIwIDAgMjIwIDI4NCIgcm9sZT0iaW1nIiA+Cjx0aXRsZT5IRVhBTE9DSyBtb2R1bGFyIGludGVyZmFjZSBhc3NldDwvdGl0bGU+CjxkZWZzPjwvZGVmcz4KICAgICAgPHJlY3QgeD0iOCIgeT0iOCIgd2lkdGg9IjIwNCIgaGVpZ2h0PSIyNjgiIHJ4PSIxNCIgZmlsbD0iIzExMUMyMiIgc3Ryb2tlPSIjNTM2NjZFIiBzdHJva2Utd2lkdGg9IjIiLz4KICAgICAgPHJlY3QgeD0iMTIiIHk9IjEyIiB3aWR0 ...(+3224 chars)\",\"value\":\"0\"},{\"image\":\"data:image\\/svg+xml;base64,PHN2ZyB4bWxucz0iaHR0cDovL3d3dy53My5vcmcvMjAwMC9zdmciIHdpZHRoPSIyMjAiIGhlaWdodD0iMjg0IiB2aWV3Qm94PSIwIDAgMjIwIDI4NCIgcm9sZT0iaW1nIiA+Cjx0aXRsZT5IRVhBTE9DSyBtb2R1bGFyIGludGVyZmFjZSBhc3NldDwvdGl0bGU+CjxkZWZzPjwvZGVmcz4KICAgICAgPHJlY3QgeD0iOCIgeT0iOCIgd2lkdGg9IjIwNCIgaGVpZ2h0PSIyNjgiIHJ4PSIxNCIgZmlsbD0iIzExMUMyMiIgc3Ryb2tlPSIjNTM2NjZFIiBzdHJva2Utd2lkdGg9IjIiLz4KICAgICAgPHJlY3QgeD0iMTIiIHk9IjEyIiB3aWR0 ...(+3220 chars)\",\"value\":\"1\"},{\"image\":\"data:image\\/svg+xml;base64,PHN2ZyB4bWxucz0iaHR0cDovL3d3dy53My5vcmcvMjAwMC9zdmciIHdpZHRoPSIyMjAiIGhlaWdodD0iMjg0IiB2aWV3Qm94PSIwIDAgMjIwIDI4NCIgcm9sZT0iaW1nIiA+Cjx0aXRsZT5IRVhBTE9DSyBtb2R1bGFyIGludGVyZmFjZSBhc3NldDwvdGl0bGU+CjxkZWZzPjwvZGVmcz4KICAgICAgPHJlY3QgeD0iOCIgeT0iOCIgd2lkdGg9IjIwNCIgaGVpZ2h0PSIyNjgiIHJ4PSIxNCIgZmlsbD0iIzExMUMyMiIgc3Ryb2tlPSIjQjk4NTZFIiBzdHJva2Utd2lkdGg9IjIuNiIvPgogICAgICA8cmVjdCB4PSIxMiIgeT0iMTIiIHdp ...(+3488 chars)\",\"value\":\"2\"},{\"image\":\"data:image\\/svg+xml;base64,PHN2ZyB4bWxucz0iaHR0cDovL3d3dy53My5vcmcvMjAwMC9zdmciIHdpZHRoPSIyMjAiIGhlaWdodD0iMjg0IiB2aWV3Qm94PSIwIDAgMjIwIDI4NCIgcm9sZT0iaW1nIiA+Cjx0aXRsZT5IRVhBTE9DSyBtb2R1bGFyIGludGVyZmFjZSBhc3NldDwvdGl0bGU+CjxkZWZzPjwvZGVmcz4KICAgICAgPHJlY3QgeD0iOCIgeT0iOCIgd2lkdGg9IjIwNCIgaGVpZ2h0PSIyNjgiIHJ4PSIxNCIgZmlsbD0iIzExMUMyMiIgc3Ryb2tlPSIjQjk4NTZFIiBzdHJva2Utd2lkdGg9IjIuNiIvPgogICAgICA8cmVjdCB4PSIxMiIgeT0iMTIiIHdp ...(+3484 chars)\",\"value\":\"3\"},{\"image\":\"data:image\\/svg+xml;base64,PHN2ZyB4bWxucz0iaHR0cDovL3d3dy53My5vcmcvMjAwMC9zdmciIHdpZHRoPSIyMjAiIGhlaWdodD0iMjg0IiB2aWV3Qm94PSIwIDAgMjIwIDI4NCIgcm9sZT0iaW1nIiA+Cjx0aXRsZT5IRVhBTE9DSyBtb2R1bGFyIGludGVyZmFjZSBhc3NldDwvdGl0bGU+CjxkZWZzPjwvZGVmcz4KICAgICAgPHJlY3QgeD0iOCIgeT0iOCIgd2lkdGg9IjIwNCIgaGVpZ2h0PSIyNjgiIHJ4PSIxNCIgZmlsbD0iIzExMUMyMiIgc3Ryb2tlPSIjQjk4NTZFIiBzdHJva2Utd2lkdGg9IjIuNiIvPgogICAgICA8cmVjdCB4PSIxMiIgeT0iMTIiIHdp ...(+3532 chars)\",\"value\":\"4\"},{\"image\":\"data:image\\/svg+xml;base64,PHN2ZyB4bWxucz0iaHR0cDovL3d3dy53My5vcmcvMjAwMC9zdmciIHdpZHRoPSIyMjAiIGhlaWdodD0iMjg0IiB2aWV3Qm94PSIwIDAgMjIwIDI4NCIgcm9sZT0iaW1nIiA+Cjx0aXRsZT5IRVhBTE9DSyBtb2R1bGFyIGludGVyZmFjZSBhc3NldDwvdGl0bGU+CjxkZWZzPjwvZGVmcz4KICAgICAgPHJlY3QgeD0iOCIgeT0iOCIgd2lkdGg9IjIwNCIgaGVpZ2h0PSIyNjgiIHJ4PSIxNCIgZmlsbD0iIzExMUMyMiIgc3Ryb2tlPSIjQjk4NTZFIiBzdHJva2Utd2lkdGg9IjIuNiIvPgogICAgICA8cmVjdCB4PSIxMiIgeT0iMTIiIHdp ...(+3532 chars)\",\"value\":\"5\"},{\"image\":\"data:image\\/svg+xml;base64,PHN2ZyB4bWxucz0iaHR0cDovL3d3dy53My5vcmcvMjAwMC9zdmciIHdpZHRoPSIyMjAiIGhlaWdodD0iMjg0IiB2aWV3Qm94PSIwIDAgMjIwIDI4NCIgcm9sZT0iaW1nIiA+Cjx0aXRsZT5IRVhBTE9DSyBtb2R1bGFyIGludGVyZmFjZSBhc3NldDwvdGl0bGU+CjxkZWZzPjwvZGVmcz4KICAgICAgPHJlY3QgeD0iOCIgeT0iOCIgd2lkdGg9IjIwNCIgaGVpZ2h0PSIyNjgiIHJ4PSIxNCIgZmlsbD0iIzExMUMyMiIgc3Ryb2tlPSIjQjk4NTZFIiBzdHJva2Utd2lkdGg9IjIuNiIvPgogICAgICA8cmVjdCB4PSIxMiIgeT0iMTIiIHdp ...(+3532 chars)\",\"value\":\"6\"},{\"image\":\"data:image\\/svg+xml;base64,PHN2ZyB4bWxucz0iaHR0cDovL3d3dy53My5vcmcvMjAwMC9zdmciIHdpZHRoPSIyMjAiIGhlaWdodD0iMjg0IiB2aWV3Qm94PSIwIDAgMjIwIDI4NCIgcm9sZT0iaW1nIiA+Cjx0aXRsZT5IRVhBTE9DSyBtb2R1bGFyIGludGVyZmFjZSBhc3NldDwvdGl0bGU+CjxkZWZzPjwvZGVmcz4KICAgICAgPHJlY3QgeD0iOCIgeT0iOCIgd2lkdGg9IjIwNCIgaGVpZ2h0PSIyNjgiIHJ4PSIxNCIgZmlsbD0iIzExMUMyMiIgc3Ryb2tlPSIjQjk4NTZFIiBzdHJva2Utd2lkdGg9IjIuNiIvPgogICAgICA8cmVjdCB4PSIxMiIgeT0iMTIiIHdp ...(+3524 chars)\",\"value\":\"7\"},{\"image\":\"data:image\\/svg+xml;base64,PHN2ZyB4bWxucz0iaHR0cDovL3d3dy53My5vcmcvMjAwMC9zdmciIHdpZHRoPSIyMjAiIGhlaWdodD0iMjg0IiB2aWV3Qm94PSIwIDAgMjIwIDI4NCIgcm9sZT0iaW1nIiA+Cjx0aXRsZT5IRVhBTE9DSyBtb2R1bGFyIGludGVyZmFjZSBhc3NldDwvdGl0bGU+CjxkZWZzPjwvZGVmcz4KICAgICAgPHJlY3QgeD0iOCIgeT0iOCIgd2lkdGg9IjIwNCIgaGVpZ2h0PSIyNjgiIHJ4PSIxNCIgZmlsbD0iIzExMUMyMiIgc3Ryb2tlPSIjQjk4NTZFIiBzdHJva2Utd2lkdGg9IjIuNiIvPgogICAgICA8cmVjdCB4PSIxMiIgeT0iMTIiIHdp ...(+3532 chars)\",\"value\":\"8\"},{\"image\":\"data:image\\/svg+xml;base64,PHN2ZyB4bWxucz0iaHR0cDovL3d3dy53My5vcmcvMjAwMC9zdmciIHdpZHRoPSIyMjAiIGhlaWdodD0iMjg0IiB2aWV3Qm94PSIwIDAgMjIwIDI4NCIgcm9sZT0iaW1nIiA+Cjx0aXRsZT5IRVhBTE9DSyBtb2R1bGFyIGludGVyZmFjZSBhc3NldDwvdGl0bGU+CjxkZWZzPjwvZGVmcz4KICAgICAgPHJlY3QgeD0iOCIgeT0iOCIgd2lkdGg9IjIwNCIgaGVpZ2h0PSIyNjgiIHJ4PSIxNCIgZmlsbD0iIzExMUMyMiIgc3Ryb2tlPSIjQjk4NTZFIiBzdHJva2Utd2lkdGg9IjIuNiIvPgogICAgICA8cmVjdCB4PSIxMiIgeT0iMTIiIHdp ...(+3532 chars)\",\"value\":\"9\"},{\"image\":\"data:image\\/svg+xml;base64,PHN2ZyB4bWxucz0iaHR0cDovL3d3dy53My5vcmcvMjAwMC9zdmciIHdpZHRoPSIyMjAiIGhlaWdodD0iMjg0IiB2aWV3Qm94PSIwIDAgMjIwIDI4NCIgcm9sZT0iaW1nIiA+Cjx0aXRsZT5IRVhBTE9DSyBtb2R1bGFyIGludGVyZmFjZSBhc3NldDwvdGl0bGU+CjxkZWZzPjwvZGVmcz4KICAgICAgPHJlY3QgeD0iOCIgeT0iOCIgd2lkdGg9IjIwNCIgaGVpZ2h0PSIyNjgiIHJ4PSIxNCIgZmlsbD0iIzExMUMyMiIgc3Ryb2tlPSIjQjk4NTZFIiBzdHJva2Utd2lkdGg9IjIuNiIvPgogICAgICA8cmVjdCB4PSIxMiIgeT0iMTIiIHdp ...(+3532 chars)\",\"value\":\"10\"},{\"image\":\"data:image\\/svg+xml;base64,PHN2ZyB4bWxucz0iaHR0cDovL3d3dy53My5vcmcvMjAwMC9zdmciIHdpZHRoPSIyMjAiIGhlaWdodD0iMjg0IiB2aWV3Qm94PSIwIDAgMjIwIDI4NCIgcm9sZT0iaW1nIiA+Cjx0aXRsZT5IRVhBTE9DSyBtb2R1bGFyIGludGVyZmFjZSBhc3NldDwvdGl0bGU+CjxkZWZzPjwvZGVmcz4KICAgICAgPHJlY3QgeD0iOCIgeT0iOCIgd2lkdGg9IjIwNCIgaGVpZ2h0PSIyNjgiIHJ4PSIxNCIgZmlsbD0iIzExMUMyMiIgc3Ryb2tlPSIjNTM2NjZFIiBzdHJva2Utd2lkdGg9IjIiLz4KICAgICAgPHJlY3QgeD0iMTIiIHk9IjEyIiB3aWR0 ...(+3220 chars)\",\"value\":\"11\"},{\"image\":\"data:image\\/svg+xml;base64,PHN2ZyB4bWxucz0iaHR0cDovL3d3dy53My5vcmcvMjAwMC9zdmciIHdpZHRoPSIyMjAiIGhlaWdodD0iMjg0IiB2aWV3Qm94PSIwIDAgMjIwIDI4NCIgcm9sZT0iaW1nIiA+Cjx0aXRsZT5IRVhBTE9DSyBtb2R1bGFyIGludGVyZmFjZSBhc3NldDwvdGl0bGU+CjxkZWZzPjxsaW5lYXJHcmFkaWVudCBpZD0ia3JhZnRGcm9udCIgeDE9IjAiIHkxPSIwIiB4Mj0iMSIgeTI9IjEiPjxzdG9wIHN0b3AtY29sb3I9IiNEM0I5OUEiLz48c3RvcCBvZmZzZXQ9IjEiIHN0b3AtY29sb3I9IiNBMzgzNjMiLz48L2xpbmVhckdyYWRpZW50Pjxs ...(+4752 chars)\",\"value\":\"20\"},{\"image\":\"data:image\\/svg+xml;base64,PHN2ZyB4bWxucz0iaHR0cDovL3d3dy53My5vcmcvMjAwMC9zdmciIHdpZHRoPSIyMjAiIGhlaWdodD0iMjg0IiB2aWV3Qm94PSIwIDAgMjIwIDI4NCIgcm9sZT0iaW1nIiA+Cjx0aXRsZT5IRVhBTE9DSyBtb2R1bGFyIGludGVyZmFjZSBhc3NldDwvdGl0bGU+CjxkZWZzPjxsaW5lYXJHcmFkaWVudCBpZD0ia3JhZnRGcm9udCIgeDE9IjAiIHkxPSIwIiB4Mj0iMSIgeTI9IjEiPjxzdG9wIHN0b3AtY29sb3I9IiNEM0I5OUEiLz48c3RvcCBvZmZzZXQ9IjEiIHN0b3AtY29sb3I9IiNBMzgzNjMiLz48L2xpbmVhckdyYWRpZW50Pjxs ...(+7264 chars)\",\"value\":\"21\"},{\"image\":\"data:image\\/svg+xml;base64,PHN2ZyB4bWxucz0iaHR0cDovL3d3dy53My5vcmcvMjAwMC9zdmciIHdpZHRoPSIyMjAiIGhlaWdodD0iMjg0IiB2aWV3Qm94PSIwIDAgMjIwIDI4NCIgcm9sZT0iaW1nIiA+Cjx0aXRsZT5IRVhBTE9DSyBtb2R1bGFyIGludGVyZmFjZSBhc3NldDwvdGl0bGU+CjxkZWZzPjxsaW5lYXJHcmFkaWVudCBpZD0ia3JhZnRGcm9udCIgeDE9IjAiIHkxPSIwIiB4Mj0iMSIgeTI9IjEiPjxzdG9wIHN0b3AtY29sb3I9IiNEM0I5OUEiLz48c3RvcCBvZmZzZXQ9IjEiIHN0b3AtY29sb3I9IiNBMzgzNjMiLz48L2xpbmVhckdyYWRpZW50Pjxs ...(+7264 chars)\",\"value\":\"22\"},{\"image\":\"data:image\\/svg+xml;base64,PHN2ZyB4bWxucz0iaHR0cDovL3d3dy53My5vcmcvMjAwMC9zdmciIHdpZHRoPSIyMjAiIGhlaWdodD0iMjg0IiB2aWV3Qm94PSIwIDAgMjIwIDI4NCIgcm9sZT0iaW1nIiA+Cjx0aXRsZT5IRVhBTE9DSyBtb2R1bGFyIGludGVyZmFjZSBhc3NldDwvdGl0bGU+CjxkZWZzPjxsaW5lYXJHcmFkaWVudCBpZD0ia3JhZnRGcm9udCIgeDE9IjAiIHkxPSIwIiB4Mj0iMSIgeTI9IjEiPjxzdG9wIHN0b3AtY29sb3I9IiNEM0I5OUEiLz48c3RvcCBvZmZzZXQ9IjEiIHN0b3AtY29sb3I9IiNBMzgzNjMiLz48L2xpbmVhckdyYWRpZW50Pjxs ...(+7264 chars)\",\"value\":\"23\"},{\"image\":\"data:image\\/svg+xml;base64,PHN2ZyB4bWxucz0iaHR0cDovL3d3dy53My5vcmcvMjAwMC9zdmciIHdpZHRoPSIyMjAiIGhlaWdodD0iMjg0IiB2aWV3Qm94PSIwIDAgMjIwIDI4NCIgcm9sZT0iaW1nIiA+Cjx0aXRsZT5IRVhBTE9DSyBtb2R1bGFyIGludGVyZmFjZSBhc3NldDwvdGl0bGU+CjxkZWZzPjxsaW5lYXJHcmFkaWVudCBpZD0ia3JhZnRGcm9udCIgeDE9IjAiIHkxPSIwIiB4Mj0iMSIgeTI9IjEiPjxzdG9wIHN0b3AtY29sb3I9IiNEM0I5OUEiLz48c3RvcCBvZmZzZXQ9IjEiIHN0b3AtY29sb3I9IiNBMzgzNjMiLz48L2xpbmVhckdyYWRpZW50Pjxs ...(+7260 chars)\",\"value\":\"24\"},{\"image\":\"data:image\\/svg+xml;base64,PHN2ZyB4bWxucz0iaHR0cDovL3d3dy53My5vcmcvMjAwMC9zdmciIHdpZHRoPSIyMjAiIGhlaWdodD0iMjg0IiB2aWV3Qm94PSIwIDAgMjIwIDI4NCIgcm9sZT0iaW1nIiA+Cjx0aXRsZT5IRVhBTE9DSyBtb2R1bGFyIGludGVyZmFjZSBhc3NldDwvdGl0bGU+CjxkZWZzPjxsaW5lYXJHcmFkaWVudCBpZD0ia3JhZnRGcm9udCIgeDE9IjAiIHkxPSIwIiB4Mj0iMSIgeTI9IjEiPjxzdG9wIHN0b3AtY29sb3I9IiNEM0I5OUEiLz48c3RvcCBvZmZzZXQ9IjEiIHN0b3AtY29sb3I9IiNBMzgzNjMiLz48L2xpbmVhckdyYWRpZW50Pjxs ...(+7264 chars)\",\"value\":\"25\"},{\"image\":\"data:image\\/svg+xml;base64,PHN2ZyB4bWxucz0iaHR0cDovL3d3dy53My5vcmcvMjAwMC9zdmciIHdpZHRoPSIyMjAiIGhlaWdodD0iMjg0IiB2aWV3Qm94PSIwIDAgMjIwIDI4NCIgcm9sZT0iaW1nIiA+Cjx0aXRsZT5IRVhBTE9DSyBtb2R1bGFyIGludGVyZmFjZSBhc3NldDwvdGl0bGU+CjxkZWZzPjxsaW5lYXJHcmFkaWVudCBpZD0ia3JhZnRGcm9udCIgeDE9IjAiIHkxPSIwIiB4Mj0iMSIgeTI9IjEiPjxzdG9wIHN0b3AtY29sb3I9IiNEM0I5OUEiLz48c3RvcCBvZmZzZXQ9IjEiIHN0b3AtY29sb3I9IiNBMzgzNjMiLz48L2xpbmVhckdyYWRpZW50Pjxs ...(+7272 chars)\",\"value\":\"26\"},{\"image\":\"data:image\\/svg+xml;base64,PHN2ZyB4bWxucz0iaHR0cDovL3d3dy53My5vcmcvMjAwMC9zdmciIHdpZHRoPSIyMjAiIGhlaWdodD0iMjg0IiB2aWV3Qm94PSIwIDAgMjIwIDI4NCIgcm9sZT0iaW1nIiA+Cjx0aXRsZT5IRVhBTE9DSyBtb2R1bGFyIGludGVyZmFjZSBhc3NldDwvdGl0bGU+CjxkZWZzPjxsaW5lYXJHcmFkaWVudCBpZD0ia3JhZnRGcm9udCIgeDE9IjAiIHkxPSIwIiB4Mj0iMSIgeTI9IjEiPjxzdG9wIHN0b3AtY29sb3I9IiNEM0I5OUEiLz48c3RvcCBvZmZzZXQ9IjEiIHN0b3AtY29sb3I9IiNBMzgzNjMiLz48L2xpbmVhckdyYWRpZW50Pjxs ...(+7264 chars)\",\"value\":\"27\"},{\"image\":\"data:image\\/svg+xml;base64,PHN2ZyB4bWxucz0iaHR0cDovL3d3dy53My5vcmcvMjAwMC9zdmciIHdpZHRoPSIyMjAiIGhlaWdodD0iMjg0IiB2aWV3Qm94PSIwIDAgMjIwIDI4NCIgcm9sZT0iaW1nIiA+Cjx0aXRsZT5IRVhBTE9DSyBtb2R1bGFyIGludGVyZmFjZSBhc3NldDwvdGl0bGU+CjxkZWZzPjxsaW5lYXJHcmFkaWVudCBpZD0ia3JhZnRGcm9udCIgeDE9IjAiIHkxPSIwIiB4Mj0iMSIgeTI9IjEiPjxzdG9wIHN0b3AtY29sb3I9IiNEM0I5OUEiLz48c3RvcCBvZmZzZXQ9IjEiIHN0b3AtY29sb3I9IiNBMzgzNjMiLz48L2xpbmVhckdyYWRpZW50Pjxs ...(+7268 chars)\",\"value\":\"28\"},{\"image\":\"data:image\\/svg+xml;base64,PHN2ZyB4bWxucz0iaHR0cDovL3d3dy53My5vcmcvMjAwMC9zdmciIHdpZHRoPSIyMjAiIGhlaWdodD0iMjg0IiB2aWV3Qm94PSIwIDAgMjIwIDI4NCIgcm9sZT0iaW1nIiA+Cjx0aXRsZT5IRVhBTE9DSyBtb2R1bGFyIGludGVyZmFjZSBhc3NldDwvdGl0bGU+CjxkZWZzPjxsaW5lYXJHcmFkaWVudCBpZD0ia3JhZnRGcm9udCIgeDE9IjAiIHkxPSIwIiB4Mj0iMSIgeTI9IjEiPjxzdG9wIHN0b3AtY29sb3I9IiNEM0I5OUEiLz48c3RvcCBvZmZzZXQ9IjEiIHN0b3AtY29sb3I9IiNBMzgzNjMiLz48L2xpbmVhckdyYWRpZW50Pjxs ...(+7268 chars)\",\"value\":\"29\"},{\"image\":\"data:image\\/svg+xml;base64,PHN2ZyB4bWxucz0iaHR0cDovL3d3dy53My5vcmcvMjAwMC9zdmciIHdpZHRoPSIyMjAiIGhlaWdodD0iMjg0IiB2aWV3Qm94PSIwIDAgMjIwIDI4NCIgcm9sZT0iaW1nIiA+Cjx0aXRsZT5IRVhBTE9DSyBtb2R1bGFyIGludGVyZmFjZSBhc3NldDwvdGl0bGU+CjxkZWZzPjxsaW5lYXJHcmFkaWVudCBpZD0ia3JhZnRGcm9udCIgeDE9IjAiIHkxPSIwIiB4Mj0iMSIgeTI9IjEiPjxzdG9wIHN0b3AtY29sb3I9IiNEM0I5OUEiLz48c3RvcCBvZmZzZXQ9IjEiIHN0b3AtY29sb3I9IiNBMzgzNjMiLz48L2xpbmVhckdyYWRpZW50Pjxs ...(+7268 chars)\",\"value\":\"30\"},{\"image\":\"data:image\\/svg+xml;base64,PHN2ZyB4bWxucz0iaHR0cDovL3d3dy53My5vcmcvMjAwMC9zdmciIHdpZHRoPSIyMjAiIGhlaWdodD0iMjg0IiB2aWV3Qm94PSIwIDAgMjIwIDI4NCIgcm9sZT0iaW1nIiA+Cjx0aXRsZT5IRVhBTE9DSyBtb2R1bGFyIGludGVyZmFjZSBhc3NldDwvdGl0bGU+CjxkZWZzPjxsaW5lYXJHcmFkaWVudCBpZD0ia3JhZnRGcm9udCIgeDE9IjAiIHkxPSIwIiB4Mj0iMSIgeTI9IjEiPjxzdG9wIHN0b3AtY29sb3I9IiNEM0I5OUEiLz48c3RvcCBvZmZzZXQ9IjEiIHN0b3AtY29sb3I9IiNBMzgzNjMiLz48L2xpbmVhckdyYWRpZW50Pjxs ...(+4756 chars)\",\"value\":\"31\"},{\"image\":\"data:image\\/svg+xml;base64,PHN2ZyB4bWxucz0iaHR0cDovL3d3dy53My5vcmcvMjAwMC9zdmciIHdpZHRoPSIyMjAiIGhlaWdodD0iMjg0IiB2aWV3Qm94PSIwIDAgMjIwIDI4NCIgcm9sZT0iaW1nIiA+Cjx0aXRsZT5IRVhBTE9DSyBtb2R1bGFyIGludGVyZmFjZSBhc3NldDwvdGl0bGU+CjxkZWZzPjxsaW5lYXJHcmFkaWVudCBpZD0ia3JhZnRGcm9udCIgeDE9IjAiIHkxPSIwIiB4Mj0iMSIgeTI9IjEiPjxzdG9wIHN0b3AtY29sb3I9IiNEM0I5OUEiLz48c3RvcCBvZmZzZXQ9IjEiIHN0b3AtY29sb3I9IiNBMzgzNjMiLz48L2xpbmVhckdyYWRpZW50Pjxs ...(+4752 chars)\",\"value\":\"32\"},{\"image\":\"data:image\\/svg+xml;base64,PHN2ZyB4bWxucz0iaHR0cDovL3d3dy53My5vcmcvMjAwMC9zdmciIHdpZHRoPSIyMjAiIGhlaWdodD0iMjg0IiB2aWV3Qm94PSIwIDAgMjIwIDI4NCIgcm9sZT0iaW1nIiA+Cjx0aXRsZT5IRVhBTE9DSyBtb2R1bGFyIGludGVyZmFjZSBhc3NldDwvdGl0bGU+CjxkZWZzPjxsaW5lYXJHcmFkaWVudCBpZD0ia3JhZnRGcm9udCIgeDE9IjAiIHkxPSIwIiB4Mj0iMSIgeTI9IjEiPjxzdG9wIHN0b3AtY29sb3I9IiNEM0I5OUEiLz48c3RvcCBvZmZzZXQ9IjEiIHN0b3AtY29sb3I9IiNBMzgzNjMiLz48L2xpbmVhckdyYWRpZW50Pjxs ...(+6860 chars)\",\"value\":\"33\"},{\"image\":\"data:image\\/svg+xml;base64,PHN2ZyB4bWxucz0iaHR0cDovL3d3dy53My5vcmcvMjAwMC9zdmciIHdpZHRoPSIyMjAiIGhlaWdodD0iMjg0IiB2aWV3Qm94PSIwIDAgMjIwIDI4NCIgcm9sZT0iaW1nIiA+Cjx0aXRsZT5IRVhBTE9DSyBtb2R1bGFyIGludGVyZmFjZSBhc3NldDwvdGl0bGU+CjxkZWZzPjxsaW5lYXJHcmFkaWVudCBpZD0ia3JhZnRGcm9udCIgeDE9IjAiIHkxPSIwIiB4Mj0iMSIgeTI9IjEiPjxzdG9wIHN0b3AtY29sb3I9IiNEM0I5OUEiLz48c3RvcCBvZmZzZXQ9IjEiIHN0b3AtY29sb3I9IiNBMzgzNjMiLz48L2xpbmVhckdyYWRpZW50Pjxs ...(+6860 chars)\",\"value\":\"34\"},{\"image\":\"data:image\\/svg+xml;base64,PHN2ZyB4bWxucz0iaHR0cDovL3d3dy53My5vcmcvMjAwMC9zdmciIHdpZHRoPSIyMjAiIGhlaWdodD0iMjg0IiB2aWV3Qm94PSIwIDAgMjIwIDI4NCIgcm9sZT0iaW1nIiA+Cjx0aXRsZT5IRVhBTE9DSyBtb2R1bGFyIGludGVyZmFjZSBhc3NldDwvdGl0bGU+CjxkZWZzPjxsaW5lYXJHcmFkaWVudCBpZD0ia3JhZnRGcm9udCIgeDE9IjAiIHkxPSIwIiB4Mj0iMSIgeTI9IjEiPjxzdG9wIHN0b3AtY29sb3I9IiNEM0I5OUEiLz48c3RvcCBvZmZzZXQ9IjEiIHN0b3AtY29sb3I9IiNBMzgzNjMiLz48L2xpbmVhckdyYWRpZW50Pjxs ...(+6860 chars)\",\"value\":\"35\"},{\"image\":\"data:image\\/svg+xml;base64,PHN2ZyB4bWxucz0iaHR0cDovL3d3dy53My5vcmcvMjAwMC9zdmciIHdpZHRoPSIyMjAiIGhlaWdodD0iMjg0IiB2aWV3Qm94PSIwIDAgMjIwIDI4NCIgcm9sZT0iaW1nIiA+DQo8dGl0bGU+SEVYQUxPQ0sgbW9kdWxhciBpbnRlcmZhY2UgYXNzZXQ8L3RpdGxlPg0KPGRlZnM+PGxpbmVhckdyYWRpZW50IGlkPSJrcmFmdEZyb250IiB4MT0iMCIgeTE9IjAiIHgyPSIxIiB5Mj0iMSI+PHN0b3Agc3RvcC1jb2xvcj0iI0QzQjk5QSIvPjxzdG9wIG9mZnNldD0iMSIgc3RvcC1jb2xvcj0iI0EzODM2MyIvPjwvbGluZWFyR3JhZGllbnQ+ ...(+6912 chars)\",\"value\":\"36\"},{\"image\":\"data:image\\/svg+xml;base64,PHN2ZyB4bWxucz0iaHR0cDovL3d3dy53My5vcmcvMjAwMC9zdmciIHdpZHRoPSIyMjAiIGhlaWdodD0iMjg0IiB2aWV3Qm94PSIwIDAgMjIwIDI4NCIgcm9sZT0iaW1nIiA+DQo8dGl0bGU+SEVYQUxPQ0sgbW9kdWxhciBpbnRlcmZhY2UgYXNzZXQ8L3RpdGxlPg0KPGRlZnM+PGxpbmVhckdyYWRpZW50IGlkPSJrcmFmdEZyb250IiB4MT0iMCIgeTE9IjAiIHgyPSIxIiB5Mj0iMSI+PHN0b3Agc3RvcC1jb2xvcj0iI0QzQjk5QSIvPjxzdG9wIG9mZnNldD0iMSIgc3RvcC1jb2xvcj0iI0EzODM2MyIvPjwvbGluZWFyR3JhZGllbnQ+ ...(+6912 chars)\",\"value\":\"37\"},{\"image\":\"data:image\\/svg+xml;base64,PHN2ZyB4bWxucz0iaHR0cDovL3d3dy53My5vcmcvMjAwMC9zdmciIHdpZHRoPSIyMjAiIGhlaWdodD0iMjg0IiB2aWV3Qm94PSIwIDAgMjIwIDI4NCIgcm9sZT0iaW1nIiA+DQo8dGl0bGU+SEVYQUxPQ0sgbW9kdWxhciBpbnRlcmZhY2UgYXNzZXQ8L3RpdGxlPg0KPGRlZnM+PGxpbmVhckdyYWRpZW50IGlkPSJrcmFmdEZyb250IiB4MT0iMCIgeTE9IjAiIHgyPSIxIiB5Mj0iMSI+PHN0b3Agc3RvcC1jb2xvcj0iI0QzQjk5QSIvPjxzdG9wIG9mZnNldD0iMSIgc3RvcC1jb2xvcj0iI0EzODM2MyIvPjwvbGluZWFyR3JhZGllbnQ+ ...(+6912 chars)\",\"value\":\"38\"}],\"fixedAspectRatio\":\"on\"}},\"settings\":{\"BindingType\":\"signal\",\"backgroundColor\":[0,0,0],\"backgroundOffset\":0.14,\"backgroundOpacity\":1,\"blockOrientation\":\"Right\",\"fixedAspectRatio\":\"on\",\"showBackgroundColor\":false,\"value\":0,\"version\":\"R2026b\"},\"type\":\"MultistateImage\"}"
  MultiStateImage9 : CustomWebBlock  LabelPosition=Hide  ShowInitialText=on  Configuration="{\"components\":[{\"name\":\"BackgroundImageComponent\",\"settings\":{\"image\":{\"size\":[0,0],\"src\":\"default\",\"srcOrientation\":\"Right\"},\"position\":[0,0,1,1],\"scaleMode\":\"0\"}},{\"name\":\"MultistateImageStateComponent\",\"settings\":{\"applyDefaults\":true,\"position\":[0,0,1,1],\"states\":[{\"image\":{\"size\":[0.7746478873239436,1],\"src\":\"data:image\\/svg+xml;base64,PHN2ZyB4bWxucz0iaHR0cDovL3d3dy53My5vcmcvMjAwMC9zdmciIHdpZHRoPSIyMjAiIGhlaWdodD0iMjg0IiB2aWV3Qm94PSIwIDAgMjIwIDI4NCIgcm9sZT0iaW1nIiA+Cjx0aXRsZT5IRVhBTE9DSyBtb2R1bGFyIGludGVyZmFjZSBhc3NldDwvdGl0bGU+CjxkZWZzPjwvZGVmcz4KICAgICAgPHJlY3QgeD0iOCIgeT0iOCIgd2lkdGg9IjIwNCIgaGVpZ2h0PSIyNjgiIHJ4PSIxNCIgZmlsbD0iIzExMUMyMiIgc3Ryb2tlPSIjNTM2NjZFIiBzdHJva2Utd2lkdGg9IjIiLz4KICAgICAgPHJlY3QgeD0iMTIiIHk9IjEyIiB3aWR0 ...(+3224 chars)\",\"srcOrientation\":\"Right\"},\"position\":[0,0,1,1],\"value\":[]},{\"image\":{\"size\":[0,0],\"src\":\"data:image\\/svg+xml;base64,PHN2ZyB4bWxucz0iaHR0cDovL3d3dy53My5vcmcvMjAwMC9zdmciIHdpZHRoPSIyMjAiIGhlaWdodD0iMjg0IiB2aWV3Qm94PSIwIDAgMjIwIDI4NCIgcm9sZT0iaW1nIiA+Cjx0aXRsZT5IRVhBTE9DSyBtb2R1bGFyIGludGVyZmFjZSBhc3NldDwvdGl0bGU+CjxkZWZzPjwvZGVmcz4KICAgICAgPHJlY3QgeD0iOCIgeT0iOCIgd2lkdGg9IjIwNCIgaGVpZ2h0PSIyNjgiIHJ4PSIxNCIgZmlsbD0iIzExMUMyMiIgc3Ryb2tlPSIjNTM2NjZFIiBzdHJva2Utd2lkdGg9IjIiLz4KICAgICAgPHJlY3QgeD0iMTIiIHk9IjEyIiB3aWR0 ...(+3224 chars)\",\"srcOrientation\":\"Right\"},\"position\":[0,0,1,1],\"value\":\"0\"},{\"image\":{\"size\":[0,0],\"src\":\"data:image\\/svg+xml;base64,PHN2ZyB4bWxucz0iaHR0cDovL3d3dy53My5vcmcvMjAwMC9zdmciIHdpZHRoPSIyMjAiIGhlaWdodD0iMjg0IiB2aWV3Qm94PSIwIDAgMjIwIDI4NCIgcm9sZT0iaW1nIiA+Cjx0aXRsZT5IRVhBTE9DSyBtb2R1bGFyIGludGVyZmFjZSBhc3NldDwvdGl0bGU+CjxkZWZzPjwvZGVmcz4KICAgICAgPHJlY3QgeD0iOCIgeT0iOCIgd2lkdGg9IjIwNCIgaGVpZ2h0PSIyNjgiIHJ4PSIxNCIgZmlsbD0iIzExMUMyMiIgc3Ryb2tlPSIjNTM2NjZFIiBzdHJva2Utd2lkdGg9IjIiLz4KICAgICAgPHJlY3QgeD0iMTIiIHk9IjEyIiB3aWR0 ...(+3220 chars)\",\"srcOrientation\":\"Right\"},\"position\":[0,0,1,1],\"value\":\"1\"},{\"image\":{\"size\":[0,0],\"src\":\"data:image\\/svg+xml;base64,PHN2ZyB4bWxucz0iaHR0cDovL3d3dy53My5vcmcvMjAwMC9zdmciIHdpZHRoPSIyMjAiIGhlaWdodD0iMjg0IiB2aWV3Qm94PSIwIDAgMjIwIDI4NCIgcm9sZT0iaW1nIiA+Cjx0aXRsZT5IRVhBTE9DSyBtb2R1bGFyIGludGVyZmFjZSBhc3NldDwvdGl0bGU+CjxkZWZzPjwvZGVmcz4KICAgICAgPHJlY3QgeD0iOCIgeT0iOCIgd2lkdGg9IjIwNCIgaGVpZ2h0PSIyNjgiIHJ4PSIxNCIgZmlsbD0iIzExMUMyMiIgc3Ryb2tlPSIjQjk4NTZFIiBzdHJva2Utd2lkdGg9IjIuNiIvPgogICAgICA8cmVjdCB4PSIxMiIgeT0iMTIiIHdp ...(+3488 chars)\",\"srcOrientation\":\"Right\"},\"position\":[0,0,1,1],\"value\":\"2\"},{\"image\":{\"size\":[0,0],\"src\":\"data:image\\/svg+xml;base64,PHN2ZyB4bWxucz0iaHR0cDovL3d3dy53My5vcmcvMjAwMC9zdmciIHdpZHRoPSIyMjAiIGhlaWdodD0iMjg0IiB2aWV3Qm94PSIwIDAgMjIwIDI4NCIgcm9sZT0iaW1nIiA+Cjx0aXRsZT5IRVhBTE9DSyBtb2R1bGFyIGludGVyZmFjZSBhc3NldDwvdGl0bGU+CjxkZWZzPjwvZGVmcz4KICAgICAgPHJlY3QgeD0iOCIgeT0iOCIgd2lkdGg9IjIwNCIgaGVpZ2h0PSIyNjgiIHJ4PSIxNCIgZmlsbD0iIzExMUMyMiIgc3Ryb2tlPSIjQjk4NTZFIiBzdHJva2Utd2lkdGg9IjIuNiIvPgogICAgICA8cmVjdCB4PSIxMiIgeT0iMTIiIHdp ...(+3484 chars)\",\"srcOrientation\":\"Right\"},\"position\":[0,0,1,1],\"value\":\"3\"},{\"image\":{\"size\":[0,0],\"src\":\"data:image\\/svg+xml;base64,PHN2ZyB4bWxucz0iaHR0cDovL3d3dy53My5vcmcvMjAwMC9zdmciIHdpZHRoPSIyMjAiIGhlaWdodD0iMjg0IiB2aWV3Qm94PSIwIDAgMjIwIDI4NCIgcm9sZT0iaW1nIiA+Cjx0aXRsZT5IRVhBTE9DSyBtb2R1bGFyIGludGVyZmFjZSBhc3NldDwvdGl0bGU+CjxkZWZzPjwvZGVmcz4KICAgICAgPHJlY3QgeD0iOCIgeT0iOCIgd2lkdGg9IjIwNCIgaGVpZ2h0PSIyNjgiIHJ4PSIxNCIgZmlsbD0iIzExMUMyMiIgc3Ryb2tlPSIjQjk4NTZFIiBzdHJva2Utd2lkdGg9IjIuNiIvPgogICAgICA8cmVjdCB4PSIxMiIgeT0iMTIiIHdp ...(+3532 chars)\",\"srcOrientation\":\"Right\"},\"position\":[0,0,1,1],\"value\":\"4\"},{\"image\":{\"size\":[0,0],\"src\":\"data:image\\/svg+xml;base64,PHN2ZyB4bWxucz0iaHR0cDovL3d3dy53My5vcmcvMjAwMC9zdmciIHdpZHRoPSIyMjAiIGhlaWdodD0iMjg0IiB2aWV3Qm94PSIwIDAgMjIwIDI4NCIgcm9sZT0iaW1nIiA+Cjx0aXRsZT5IRVhBTE9DSyBtb2R1bGFyIGludGVyZmFjZSBhc3NldDwvdGl0bGU+CjxkZWZzPjwvZGVmcz4KICAgICAgPHJlY3QgeD0iOCIgeT0iOCIgd2lkdGg9IjIwNCIgaGVpZ2h0PSIyNjgiIHJ4PSIxNCIgZmlsbD0iIzExMUMyMiIgc3Ryb2tlPSIjQjk4NTZFIiBzdHJva2Utd2lkdGg9IjIuNiIvPgogICAgICA8cmVjdCB4PSIxMiIgeT0iMTIiIHdp ...(+3532 chars)\",\"srcOrientation\":\"Right\"},\"position\":[0,0,1,1],\"value\":\"5\"},{\"image\":{\"size\":[0,0],\"src\":\"data:image\\/svg+xml;base64,PHN2ZyB4bWxucz0iaHR0cDovL3d3dy53My5vcmcvMjAwMC9zdmciIHdpZHRoPSIyMjAiIGhlaWdodD0iMjg0IiB2aWV3Qm94PSIwIDAgMjIwIDI4NCIgcm9sZT0iaW1nIiA+Cjx0aXRsZT5IRVhBTE9DSyBtb2R1bGFyIGludGVyZmFjZSBhc3NldDwvdGl0bGU+CjxkZWZzPjwvZGVmcz4KICAgICAgPHJlY3QgeD0iOCIgeT0iOCIgd2lkdGg9IjIwNCIgaGVpZ2h0PSIyNjgiIHJ4PSIxNCIgZmlsbD0iIzExMUMyMiIgc3Ryb2tlPSIjQjk4NTZFIiBzdHJva2Utd2lkdGg9IjIuNiIvPgogICAgICA8cmVjdCB4PSIxMiIgeT0iMTIiIHdp ...(+3532 chars)\",\"srcOrientation\":\"Right\"},\"position\":[0,0,1,1],\"value\":\"6\"},{\"image\":{\"size\":[0,0],\"src\":\"data:image\\/svg+xml;base64,PHN2ZyB4bWxucz0iaHR0cDovL3d3dy53My5vcmcvMjAwMC9zdmciIHdpZHRoPSIyMjAiIGhlaWdodD0iMjg0IiB2aWV3Qm94PSIwIDAgMjIwIDI4NCIgcm9sZT0iaW1nIiA+Cjx0aXRsZT5IRVhBTE9DSyBtb2R1bGFyIGludGVyZmFjZSBhc3NldDwvdGl0bGU+CjxkZWZzPjwvZGVmcz4KICAgICAgPHJlY3QgeD0iOCIgeT0iOCIgd2lkdGg9IjIwNCIgaGVpZ2h0PSIyNjgiIHJ4PSIxNCIgZmlsbD0iIzExMUMyMiIgc3Ryb2tlPSIjQjk4NTZFIiBzdHJva2Utd2lkdGg9IjIuNiIvPgogICAgICA8cmVjdCB4PSIxMiIgeT0iMTIiIHdp ...(+3524 chars)\",\"srcOrientation\":\"Right\"},\"position\":[0,0,1,1],\"value\":\"7\"},{\"image\":{\"size\":[0,0],\"src\":\"data:image\\/svg+xml;base64,PHN2ZyB4bWxucz0iaHR0cDovL3d3dy53My5vcmcvMjAwMC9zdmciIHdpZHRoPSIyMjAiIGhlaWdodD0iMjg0IiB2aWV3Qm94PSIwIDAgMjIwIDI4NCIgcm9sZT0iaW1nIiA+Cjx0aXRsZT5IRVhBTE9DSyBtb2R1bGFyIGludGVyZmFjZSBhc3NldDwvdGl0bGU+CjxkZWZzPjwvZGVmcz4KICAgICAgPHJlY3QgeD0iOCIgeT0iOCIgd2lkdGg9IjIwNCIgaGVpZ2h0PSIyNjgiIHJ4PSIxNCIgZmlsbD0iIzExMUMyMiIgc3Ryb2tlPSIjQjk4NTZFIiBzdHJva2Utd2lkdGg9IjIuNiIvPgogICAgICA8cmVjdCB4PSIxMiIgeT0iMTIiIHdp ...(+3532 chars)\",\"srcOrientation\":\"Right\"},\"position\":[0,0,1,1],\"value\":\"8\"},{\"image\":{\"size\":[0,0],\"src\":\"data:image\\/svg+xml;base64,PHN2ZyB4bWxucz0iaHR0cDovL3d3dy53My5vcmcvMjAwMC9zdmciIHdpZHRoPSIyMjAiIGhlaWdodD0iMjg0IiB2aWV3Qm94PSIwIDAgMjIwIDI4NCIgcm9sZT0iaW1nIiA+Cjx0aXRsZT5IRVhBTE9DSyBtb2R1bGFyIGludGVyZmFjZSBhc3NldDwvdGl0bGU+CjxkZWZzPjwvZGVmcz4KICAgICAgPHJlY3QgeD0iOCIgeT0iOCIgd2lkdGg9IjIwNCIgaGVpZ2h0PSIyNjgiIHJ4PSIxNCIgZmlsbD0iIzExMUMyMiIgc3Ryb2tlPSIjQjk4NTZFIiBzdHJva2Utd2lkdGg9IjIuNiIvPgogICAgICA8cmVjdCB4PSIxMiIgeT0iMTIiIHdp ...(+3532 chars)\",\"srcOrientation\":\"Right\"},\"position\":[0,0,1,1],\"value\":\"9\"},{\"image\":{\"size\":[0,0],\"src\":\"data:image\\/svg+xml;base64,PHN2ZyB4bWxucz0iaHR0cDovL3d3dy53My5vcmcvMjAwMC9zdmciIHdpZHRoPSIyMjAiIGhlaWdodD0iMjg0IiB2aWV3Qm94PSIwIDAgMjIwIDI4NCIgcm9sZT0iaW1nIiA+Cjx0aXRsZT5IRVhBTE9DSyBtb2R1bGFyIGludGVyZmFjZSBhc3NldDwvdGl0bGU+CjxkZWZzPjwvZGVmcz4KICAgICAgPHJlY3QgeD0iOCIgeT0iOCIgd2lkdGg9IjIwNCIgaGVpZ2h0PSIyNjgiIHJ4PSIxNCIgZmlsbD0iIzExMUMyMiIgc3Ryb2tlPSIjQjk4NTZFIiBzdHJva2Utd2lkdGg9IjIuNiIvPgogICAgICA8cmVjdCB4PSIxMiIgeT0iMTIiIHdp ...(+3532 chars)\",\"srcOrientation\":\"Right\"},\"position\":[0,0,1,1],\"value\":\"10\"},{\"image\":{\"size\":[0,0],\"src\":\"data:image\\/svg+xml;base64,PHN2ZyB4bWxucz0iaHR0cDovL3d3dy53My5vcmcvMjAwMC9zdmciIHdpZHRoPSIyMjAiIGhlaWdodD0iMjg0IiB2aWV3Qm94PSIwIDAgMjIwIDI4NCIgcm9sZT0iaW1nIiA+Cjx0aXRsZT5IRVhBTE9DSyBtb2R1bGFyIGludGVyZmFjZSBhc3NldDwvdGl0bGU+CjxkZWZzPjwvZGVmcz4KICAgICAgPHJlY3QgeD0iOCIgeT0iOCIgd2lkdGg9IjIwNCIgaGVpZ2h0PSIyNjgiIHJ4PSIxNCIgZmlsbD0iIzExMUMyMiIgc3Ryb2tlPSIjNTM2NjZFIiBzdHJva2Utd2lkdGg9IjIiLz4KICAgICAgPHJlY3QgeD0iMTIiIHk9IjEyIiB3aWR0 ...(+3220 chars)\",\"srcOrientation\":\"Right\"},\"position\":[0,0,1,1],\"value\":\"11\"},{\"image\":{\"size\":[0,0],\"src\":\"data:image\\/svg+xml;base64,PHN2ZyB4bWxucz0iaHR0cDovL3d3dy53My5vcmcvMjAwMC9zdmciIHdpZHRoPSIyMjAiIGhlaWdodD0iMjg0IiB2aWV3Qm94PSIwIDAgMjIwIDI4NCIgcm9sZT0iaW1nIiA+Cjx0aXRsZT5IRVhBTE9DSyBtb2R1bGFyIGludGVyZmFjZSBhc3NldDwvdGl0bGU+CjxkZWZzPjxsaW5lYXJHcmFkaWVudCBpZD0ia3JhZnRGcm9udCIgeDE9IjAiIHkxPSIwIiB4Mj0iMSIgeTI9IjEiPjxzdG9wIHN0b3AtY29sb3I9IiNEM0I5OUEiLz48c3RvcCBvZmZzZXQ9IjEiIHN0b3AtY29sb3I9IiNBMzgzNjMiLz48L2xpbmVhckdyYWRpZW50Pjxs ...(+4752 chars)\",\"srcOrientation\":\"Right\"},\"position\":[0,0,1,1],\"value\":\"20\"},{\"image\":{\"size\":[0,0],\"src\":\"data:image\\/svg+xml;base64,PHN2ZyB4bWxucz0iaHR0cDovL3d3dy53My5vcmcvMjAwMC9zdmciIHdpZHRoPSIyMjAiIGhlaWdodD0iMjg0IiB2aWV3Qm94PSIwIDAgMjIwIDI4NCIgcm9sZT0iaW1nIiA+Cjx0aXRsZT5IRVhBTE9DSyBtb2R1bGFyIGludGVyZmFjZSBhc3NldDwvdGl0bGU+CjxkZWZzPjxsaW5lYXJHcmFkaWVudCBpZD0ia3JhZnRGcm9udCIgeDE9IjAiIHkxPSIwIiB4Mj0iMSIgeTI9IjEiPjxzdG9wIHN0b3AtY29sb3I9IiNEM0I5OUEiLz48c3RvcCBvZmZzZXQ9IjEiIHN0b3AtY29sb3I9IiNBMzgzNjMiLz48L2xpbmVhckdyYWRpZW50Pjxs ...(+7264 chars)\",\"srcOrientation\":\"Right\"},\"position\":[0,0,1,1],\"value\":\"21\"},{\"image\":{\"size\":[0,0],\"src\":\"data:image\\/svg+xml;base64,PHN2ZyB4bWxucz0iaHR0cDovL3d3dy53My5vcmcvMjAwMC9zdmciIHdpZHRoPSIyMjAiIGhlaWdodD0iMjg0IiB2aWV3Qm94PSIwIDAgMjIwIDI4NCIgcm9sZT0iaW1nIiA+Cjx0aXRsZT5IRVhBTE9DSyBtb2R1bGFyIGludGVyZmFjZSBhc3NldDwvdGl0bGU+CjxkZWZzPjxsaW5lYXJHcmFkaWVudCBpZD0ia3JhZnRGcm9udCIgeDE9IjAiIHkxPSIwIiB4Mj0iMSIgeTI9IjEiPjxzdG9wIHN0b3AtY29sb3I9IiNEM0I5OUEiLz48c3RvcCBvZmZzZXQ9IjEiIHN0b3AtY29sb3I9IiNBMzgzNjMiLz48L2xpbmVhckdyYWRpZW50Pjxs ...(+7264 chars)\",\"srcOrientation\":\"Right\"},\"position\":[0,0,1,1],\"value\":\"22\"},{\"image\":{\"size\":[0,0],\"src\":\"data:image\\/svg+xml;base64,PHN2ZyB4bWxucz0iaHR0cDovL3d3dy53My5vcmcvMjAwMC9zdmciIHdpZHRoPSIyMjAiIGhlaWdodD0iMjg0IiB2aWV3Qm94PSIwIDAgMjIwIDI4NCIgcm9sZT0iaW1nIiA+Cjx0aXRsZT5IRVhBTE9DSyBtb2R1bGFyIGludGVyZmFjZSBhc3NldDwvdGl0bGU+CjxkZWZzPjxsaW5lYXJHcmFkaWVudCBpZD0ia3JhZnRGcm9udCIgeDE9IjAiIHkxPSIwIiB4Mj0iMSIgeTI9IjEiPjxzdG9wIHN0b3AtY29sb3I9IiNEM0I5OUEiLz48c3RvcCBvZmZzZXQ9IjEiIHN0b3AtY29sb3I9IiNBMzgzNjMiLz48L2xpbmVhckdyYWRpZW50Pjxs ...(+7264 chars)\",\"srcOrientation\":\"Right\"},\"position\":[0,0,1,1],\"value\":\"23\"},{\"image\":{\"size\":[0,0],\"src\":\"data:image\\/svg+xml;base64,PHN2ZyB4bWxucz0iaHR0cDovL3d3dy53My5vcmcvMjAwMC9zdmciIHdpZHRoPSIyMjAiIGhlaWdodD0iMjg0IiB2aWV3Qm94PSIwIDAgMjIwIDI4NCIgcm9sZT0iaW1nIiA+Cjx0aXRsZT5IRVhBTE9DSyBtb2R1bGFyIGludGVyZmFjZSBhc3NldDwvdGl0bGU+CjxkZWZzPjxsaW5lYXJHcmFkaWVudCBpZD0ia3JhZnRGcm9udCIgeDE9IjAiIHkxPSIwIiB4Mj0iMSIgeTI9IjEiPjxzdG9wIHN0b3AtY29sb3I9IiNEM0I5OUEiLz48c3RvcCBvZmZzZXQ9IjEiIHN0b3AtY29sb3I9IiNBMzgzNjMiLz48L2xpbmVhckdyYWRpZW50Pjxs ...(+7260 chars)\",\"srcOrientation\":\"Right\"},\"position\":[0,0,1,1],\"value\":\"24\"},{\"image\":{\"size\":[0,0],\"src\":\"data:image\\/svg+xml;base64,PHN2ZyB4bWxucz0iaHR0cDovL3d3dy53My5vcmcvMjAwMC9zdmciIHdpZHRoPSIyMjAiIGhlaWdodD0iMjg0IiB2aWV3Qm94PSIwIDAgMjIwIDI4NCIgcm9sZT0iaW1nIiA+Cjx0aXRsZT5IRVhBTE9DSyBtb2R1bGFyIGludGVyZmFjZSBhc3NldDwvdGl0bGU+CjxkZWZzPjxsaW5lYXJHcmFkaWVudCBpZD0ia3JhZnRGcm9udCIgeDE9IjAiIHkxPSIwIiB4Mj0iMSIgeTI9IjEiPjxzdG9wIHN0b3AtY29sb3I9IiNEM0I5OUEiLz48c3RvcCBvZmZzZXQ9IjEiIHN0b3AtY29sb3I9IiNBMzgzNjMiLz48L2xpbmVhckdyYWRpZW50Pjxs ...(+7264 chars)\",\"srcOrientation\":\"Right\"},\"position\":[0,0,1,1],\"value\":\"25\"},{\"image\":{\"size\":[0,0],\"src\":\"data:image\\/svg+xml;base64,PHN2ZyB4bWxucz0iaHR0cDovL3d3dy53My5vcmcvMjAwMC9zdmciIHdpZHRoPSIyMjAiIGhlaWdodD0iMjg0IiB2aWV3Qm94PSIwIDAgMjIwIDI4NCIgcm9sZT0iaW1nIiA+Cjx0aXRsZT5IRVhBTE9DSyBtb2R1bGFyIGludGVyZmFjZSBhc3NldDwvdGl0bGU+CjxkZWZzPjxsaW5lYXJHcmFkaWVudCBpZD0ia3JhZnRGcm9udCIgeDE9IjAiIHkxPSIwIiB4Mj0iMSIgeTI9IjEiPjxzdG9wIHN0b3AtY29sb3I9IiNEM0I5OUEiLz48c3RvcCBvZmZzZXQ9IjEiIHN0b3AtY29sb3I9IiNBMzgzNjMiLz48L2xpbmVhckdyYWRpZW50Pjxs ...(+7272 chars)\",\"srcOrientation\":\"Right\"},\"position\":[0,0,1,1],\"value\":\"26\"},{\"image\":{\"size\":[0,0],\"src\":\"data:image\\/svg+xml;base64,PHN2ZyB4bWxucz0iaHR0cDovL3d3dy53My5vcmcvMjAwMC9zdmciIHdpZHRoPSIyMjAiIGhlaWdodD0iMjg0IiB2aWV3Qm94PSIwIDAgMjIwIDI4NCIgcm9sZT0iaW1nIiA+Cjx0aXRsZT5IRVhBTE9DSyBtb2R1bGFyIGludGVyZmFjZSBhc3NldDwvdGl0bGU+CjxkZWZzPjxsaW5lYXJHcmFkaWVudCBpZD0ia3JhZnRGcm9udCIgeDE9IjAiIHkxPSIwIiB4Mj0iMSIgeTI9IjEiPjxzdG9wIHN0b3AtY29sb3I9IiNEM0I5OUEiLz48c3RvcCBvZmZzZXQ9IjEiIHN0b3AtY29sb3I9IiNBMzgzNjMiLz48L2xpbmVhckdyYWRpZW50Pjxs ...(+7264 chars)\",\"srcOrientation\":\"Right\"},\"position\":[0,0,1,1],\"value\":\"27\"},{\"image\":{\"size\":[0,0],\"src\":\"data:image\\/svg+xml;base64,PHN2ZyB4bWxucz0iaHR0cDovL3d3dy53My5vcmcvMjAwMC9zdmciIHdpZHRoPSIyMjAiIGhlaWdodD0iMjg0IiB2aWV3Qm94PSIwIDAgMjIwIDI4NCIgcm9sZT0iaW1nIiA+Cjx0aXRsZT5IRVhBTE9DSyBtb2R1bGFyIGludGVyZmFjZSBhc3NldDwvdGl0bGU+CjxkZWZzPjxsaW5lYXJHcmFkaWVudCBpZD0ia3JhZnRGcm9udCIgeDE9IjAiIHkxPSIwIiB4Mj0iMSIgeTI9IjEiPjxzdG9wIHN0b3AtY29sb3I9IiNEM0I5OUEiLz48c3RvcCBvZmZzZXQ9IjEiIHN0b3AtY29sb3I9IiNBMzgzNjMiLz48L2xpbmVhckdyYWRpZW50Pjxs ...(+7268 chars)\",\"srcOrientation\":\"Right\"},\"position\":[0,0,1,1],\"value\":\"28\"},{\"image\":{\"size\":[0,0],\"src\":\"data:image\\/svg+xml;base64,PHN2ZyB4bWxucz0iaHR0cDovL3d3dy53My5vcmcvMjAwMC9zdmciIHdpZHRoPSIyMjAiIGhlaWdodD0iMjg0IiB2aWV3Qm94PSIwIDAgMjIwIDI4NCIgcm9sZT0iaW1nIiA+Cjx0aXRsZT5IRVhBTE9DSyBtb2R1bGFyIGludGVyZmFjZSBhc3NldDwvdGl0bGU+CjxkZWZzPjxsaW5lYXJHcmFkaWVudCBpZD0ia3JhZnRGcm9udCIgeDE9IjAiIHkxPSIwIiB4Mj0iMSIgeTI9IjEiPjxzdG9wIHN0b3AtY29sb3I9IiNEM0I5OUEiLz48c3RvcCBvZmZzZXQ9IjEiIHN0b3AtY29sb3I9IiNBMzgzNjMiLz48L2xpbmVhckdyYWRpZW50Pjxs ...(+7268 chars)\",\"srcOrientation\":\"Right\"},\"position\":[0,0,1,1],\"value\":\"29\"},{\"image\":{\"size\":[0,0],\"src\":\"data:image\\/svg+xml;base64,PHN2ZyB4bWxucz0iaHR0cDovL3d3dy53My5vcmcvMjAwMC9zdmciIHdpZHRoPSIyMjAiIGhlaWdodD0iMjg0IiB2aWV3Qm94PSIwIDAgMjIwIDI4NCIgcm9sZT0iaW1nIiA+Cjx0aXRsZT5IRVhBTE9DSyBtb2R1bGFyIGludGVyZmFjZSBhc3NldDwvdGl0bGU+CjxkZWZzPjxsaW5lYXJHcmFkaWVudCBpZD0ia3JhZnRGcm9udCIgeDE9IjAiIHkxPSIwIiB4Mj0iMSIgeTI9IjEiPjxzdG9wIHN0b3AtY29sb3I9IiNEM0I5OUEiLz48c3RvcCBvZmZzZXQ9IjEiIHN0b3AtY29sb3I9IiNBMzgzNjMiLz48L2xpbmVhckdyYWRpZW50Pjxs ...(+7268 chars)\",\"srcOrientation\":\"Right\"},\"position\":[0,0,1,1],\"value\":\"30\"},{\"image\":{\"size\":[0,0],\"src\":\"data:image\\/svg+xml;base64,PHN2ZyB4bWxucz0iaHR0cDovL3d3dy53My5vcmcvMjAwMC9zdmciIHdpZHRoPSIyMjAiIGhlaWdodD0iMjg0IiB2aWV3Qm94PSIwIDAgMjIwIDI4NCIgcm9sZT0iaW1nIiA+Cjx0aXRsZT5IRVhBTE9DSyBtb2R1bGFyIGludGVyZmFjZSBhc3NldDwvdGl0bGU+CjxkZWZzPjxsaW5lYXJHcmFkaWVudCBpZD0ia3JhZnRGcm9udCIgeDE9IjAiIHkxPSIwIiB4Mj0iMSIgeTI9IjEiPjxzdG9wIHN0b3AtY29sb3I9IiNEM0I5OUEiLz48c3RvcCBvZmZzZXQ9IjEiIHN0b3AtY29sb3I9IiNBMzgzNjMiLz48L2xpbmVhckdyYWRpZW50Pjxs ...(+4756 chars)\",\"srcOrientation\":\"Right\"},\"position\":[0,0,1,1],\"value\":\"31\"},{\"image\":{\"size\":[0,0],\"src\":\"data:image\\/svg+xml;base64,PHN2ZyB4bWxucz0iaHR0cDovL3d3dy53My5vcmcvMjAwMC9zdmciIHdpZHRoPSIyMjAiIGhlaWdodD0iMjg0IiB2aWV3Qm94PSIwIDAgMjIwIDI4NCIgcm9sZT0iaW1nIiA+Cjx0aXRsZT5IRVhBTE9DSyBtb2R1bGFyIGludGVyZmFjZSBhc3NldDwvdGl0bGU+CjxkZWZzPjxsaW5lYXJHcmFkaWVudCBpZD0ia3JhZnRGcm9udCIgeDE9IjAiIHkxPSIwIiB4Mj0iMSIgeTI9IjEiPjxzdG9wIHN0b3AtY29sb3I9IiNEM0I5OUEiLz48c3RvcCBvZmZzZXQ9IjEiIHN0b3AtY29sb3I9IiNBMzgzNjMiLz48L2xpbmVhckdyYWRpZW50Pjxs ...(+4752 chars)\",\"srcOrientation\":\"Right\"},\"position\":[0,0,1,1],\"value\":\"32\"},{\"image\":{\"size\":[0,0],\"src\":\"data:image\\/svg+xml;base64,PHN2ZyB4bWxucz0iaHR0cDovL3d3dy53My5vcmcvMjAwMC9zdmciIHdpZHRoPSIyMjAiIGhlaWdodD0iMjg0IiB2aWV3Qm94PSIwIDAgMjIwIDI4NCIgcm9sZT0iaW1nIiA+Cjx0aXRsZT5IRVhBTE9DSyBtb2R1bGFyIGludGVyZmFjZSBhc3NldDwvdGl0bGU+CjxkZWZzPjxsaW5lYXJHcmFkaWVudCBpZD0ia3JhZnRGcm9udCIgeDE9IjAiIHkxPSIwIiB4Mj0iMSIgeTI9IjEiPjxzdG9wIHN0b3AtY29sb3I9IiNEM0I5OUEiLz48c3RvcCBvZmZzZXQ9IjEiIHN0b3AtY29sb3I9IiNBMzgzNjMiLz48L2xpbmVhckdyYWRpZW50Pjxs ...(+6860 chars)\",\"srcOrientation\":\"Right\"},\"position\":[0,0,1,1],\"value\":\"33\"},{\"image\":{\"size\":[0,0],\"src\":\"data:image\\/svg+xml;base64,PHN2ZyB4bWxucz0iaHR0cDovL3d3dy53My5vcmcvMjAwMC9zdmciIHdpZHRoPSIyMjAiIGhlaWdodD0iMjg0IiB2aWV3Qm94PSIwIDAgMjIwIDI4NCIgcm9sZT0iaW1nIiA+Cjx0aXRsZT5IRVhBTE9DSyBtb2R1bGFyIGludGVyZmFjZSBhc3NldDwvdGl0bGU+CjxkZWZzPjxsaW5lYXJHcmFkaWVudCBpZD0ia3JhZnRGcm9udCIgeDE9IjAiIHkxPSIwIiB4Mj0iMSIgeTI9IjEiPjxzdG9wIHN0b3AtY29sb3I9IiNEM0I5OUEiLz48c3RvcCBvZmZzZXQ9IjEiIHN0b3AtY29sb3I9IiNBMzgzNjMiLz48L2xpbmVhckdyYWRpZW50Pjxs ...(+6860 chars)\",\"srcOrientation\":\"Right\"},\"position\":[0,0,1,1],\"value\":\"34\"},{\"image\":{\"size\":[0,0],\"src\":\"data:image\\/svg+xml;base64,PHN2ZyB4bWxucz0iaHR0cDovL3d3dy53My5vcmcvMjAwMC9zdmciIHdpZHRoPSIyMjAiIGhlaWdodD0iMjg0IiB2aWV3Qm94PSIwIDAgMjIwIDI4NCIgcm9sZT0iaW1nIiA+Cjx0aXRsZT5IRVhBTE9DSyBtb2R1bGFyIGludGVyZmFjZSBhc3NldDwvdGl0bGU+CjxkZWZzPjxsaW5lYXJHcmFkaWVudCBpZD0ia3JhZnRGcm9udCIgeDE9IjAiIHkxPSIwIiB4Mj0iMSIgeTI9IjEiPjxzdG9wIHN0b3AtY29sb3I9IiNEM0I5OUEiLz48c3RvcCBvZmZzZXQ9IjEiIHN0b3AtY29sb3I9IiNBMzgzNjMiLz48L2xpbmVhckdyYWRpZW50Pjxs ...(+6860 chars)\",\"srcOrientation\":\"Right\"},\"position\":[0,0,1,1],\"value\":\"35\"},{\"image\":{\"size\":[0,0],\"src\":\"data:image\\/svg+xml;base64,PHN2ZyB4bWxucz0iaHR0cDovL3d3dy53My5vcmcvMjAwMC9zdmciIHdpZHRoPSIyMjAiIGhlaWdodD0iMjg0IiB2aWV3Qm94PSIwIDAgMjIwIDI4NCIgcm9sZT0iaW1nIiA+DQo8dGl0bGU+SEVYQUxPQ0sgbW9kdWxhciBpbnRlcmZhY2UgYXNzZXQ8L3RpdGxlPg0KPGRlZnM+PGxpbmVhckdyYWRpZW50IGlkPSJrcmFmdEZyb250IiB4MT0iMCIgeTE9IjAiIHgyPSIxIiB5Mj0iMSI+PHN0b3Agc3RvcC1jb2xvcj0iI0QzQjk5QSIvPjxzdG9wIG9mZnNldD0iMSIgc3RvcC1jb2xvcj0iI0EzODM2MyIvPjwvbGluZWFyR3JhZGllbnQ+ ...(+6912 chars)\",\"srcOrientation\":\"Right\"},\"position\":[0,0,1,1],\"value\":\"36\"},{\"image\":{\"size\":[0,0],\"src\":\"data:image\\/svg+xml;base64,PHN2ZyB4bWxucz0iaHR0cDovL3d3dy53My5vcmcvMjAwMC9zdmciIHdpZHRoPSIyMjAiIGhlaWdodD0iMjg0IiB2aWV3Qm94PSIwIDAgMjIwIDI4NCIgcm9sZT0iaW1nIiA+DQo8dGl0bGU+SEVYQUxPQ0sgbW9kdWxhciBpbnRlcmZhY2UgYXNzZXQ8L3RpdGxlPg0KPGRlZnM+PGxpbmVhckdyYWRpZW50IGlkPSJrcmFmdEZyb250IiB4MT0iMCIgeTE9IjAiIHgyPSIxIiB5Mj0iMSI+PHN0b3Agc3RvcC1jb2xvcj0iI0QzQjk5QSIvPjxzdG9wIG9mZnNldD0iMSIgc3RvcC1jb2xvcj0iI0EzODM2MyIvPjwvbGluZWFyR3JhZGllbnQ+ ...(+6912 chars)\",\"srcOrientation\":\"Right\"},\"position\":[0,0,1,1],\"value\":\"37\"},{\"image\":{\"size\":[0,0],\"src\":\"data:image\\/svg+xml;base64,PHN2ZyB4bWxucz0iaHR0cDovL3d3dy53My5vcmcvMjAwMC9zdmciIHdpZHRoPSIyMjAiIGhlaWdodD0iMjg0IiB2aWV3Qm94PSIwIDAgMjIwIDI4NCIgcm9sZT0iaW1nIiA+DQo8dGl0bGU+SEVYQUxPQ0sgbW9kdWxhciBpbnRlcmZhY2UgYXNzZXQ8L3RpdGxlPg0KPGRlZnM+PGxpbmVhckdyYWRpZW50IGlkPSJrcmFmdEZyb250IiB4MT0iMCIgeTE9IjAiIHgyPSIxIiB5Mj0iMSI+PHN0b3Agc3RvcC1jb2xvcj0iI0QzQjk5QSIvPjxzdG9wIG9mZnNldD0iMSIgc3RvcC1jb2xvcj0iI0EzODM2MyIvPjwvbGluZWFyR3JhZGllbnQ+ ...(+6912 chars)\",\"srcOrientation\":\"Right\"},\"position\":[0,0,1,1],\"value\":\"38\"}],\"valueType\":\"discrete\"}},{\"name\":\"ForegroundImageComponent\",\"settings\":{\"image\":{\"size\":[0,0],\"src\":\"default\",\"srcOrientation\":\"Right\"},\"isForeground\":1,\"position\":[0,0,1,1],\"scaleMode\":\"0\"}}],\"derived\":{\"blockParameters\":{\"DefaultImage\":\"data:image\\/svg+xml;base64,PHN2ZyB4bWxucz0iaHR0cDovL3d3dy53My5vcmcvMjAwMC9zdmciIHdpZHRoPSIyMjAiIGhlaWdodD0iMjg0IiB2aWV3Qm94PSIwIDAgMjIwIDI4NCIgcm9sZT0iaW1nIiA+Cjx0aXRsZT5IRVhBTE9DSyBtb2R1bGFyIGludGVyZmFjZSBhc3NldDwvdGl0bGU+CjxkZWZzPjwvZGVmcz4KICAgICAgPHJlY3QgeD0iOCIgeT0iOCIgd2lkdGg9IjIwNCIgaGVpZ2h0PSIyNjgiIHJ4PSIxNCIgZmlsbD0iIzExMUMyMiIgc3Ryb2tlPSIjNTM2NjZFIiBzdHJva2Utd2lkdGg9IjIiLz4KICAgICAgPHJlY3QgeD0iMTIiIHk9IjEyIiB3aWR0 ...(+3224 chars)\",\"StateValueType\":\"discrete\",\"States\":[{\"image\":\"data:image\\/svg+xml;base64,PHN2ZyB4bWxucz0iaHR0cDovL3d3dy53My5vcmcvMjAwMC9zdmciIHdpZHRoPSIyMjAiIGhlaWdodD0iMjg0IiB2aWV3Qm94PSIwIDAgMjIwIDI4NCIgcm9sZT0iaW1nIiA+Cjx0aXRsZT5IRVhBTE9DSyBtb2R1bGFyIGludGVyZmFjZSBhc3NldDwvdGl0bGU+CjxkZWZzPjwvZGVmcz4KICAgICAgPHJlY3QgeD0iOCIgeT0iOCIgd2lkdGg9IjIwNCIgaGVpZ2h0PSIyNjgiIHJ4PSIxNCIgZmlsbD0iIzExMUMyMiIgc3Ryb2tlPSIjNTM2NjZFIiBzdHJva2Utd2lkdGg9IjIiLz4KICAgICAgPHJlY3QgeD0iMTIiIHk9IjEyIiB3aWR0 ...(+3224 chars)\",\"value\":\"0\"},{\"image\":\"data:image\\/svg+xml;base64,PHN2ZyB4bWxucz0iaHR0cDovL3d3dy53My5vcmcvMjAwMC9zdmciIHdpZHRoPSIyMjAiIGhlaWdodD0iMjg0IiB2aWV3Qm94PSIwIDAgMjIwIDI4NCIgcm9sZT0iaW1nIiA+Cjx0aXRsZT5IRVhBTE9DSyBtb2R1bGFyIGludGVyZmFjZSBhc3NldDwvdGl0bGU+CjxkZWZzPjwvZGVmcz4KICAgICAgPHJlY3QgeD0iOCIgeT0iOCIgd2lkdGg9IjIwNCIgaGVpZ2h0PSIyNjgiIHJ4PSIxNCIgZmlsbD0iIzExMUMyMiIgc3Ryb2tlPSIjNTM2NjZFIiBzdHJva2Utd2lkdGg9IjIiLz4KICAgICAgPHJlY3QgeD0iMTIiIHk9IjEyIiB3aWR0 ...(+3220 chars)\",\"value\":\"1\"},{\"image\":\"data:image\\/svg+xml;base64,PHN2ZyB4bWxucz0iaHR0cDovL3d3dy53My5vcmcvMjAwMC9zdmciIHdpZHRoPSIyMjAiIGhlaWdodD0iMjg0IiB2aWV3Qm94PSIwIDAgMjIwIDI4NCIgcm9sZT0iaW1nIiA+Cjx0aXRsZT5IRVhBTE9DSyBtb2R1bGFyIGludGVyZmFjZSBhc3NldDwvdGl0bGU+CjxkZWZzPjwvZGVmcz4KICAgICAgPHJlY3QgeD0iOCIgeT0iOCIgd2lkdGg9IjIwNCIgaGVpZ2h0PSIyNjgiIHJ4PSIxNCIgZmlsbD0iIzExMUMyMiIgc3Ryb2tlPSIjQjk4NTZFIiBzdHJva2Utd2lkdGg9IjIuNiIvPgogICAgICA8cmVjdCB4PSIxMiIgeT0iMTIiIHdp ...(+3488 chars)\",\"value\":\"2\"},{\"image\":\"data:image\\/svg+xml;base64,PHN2ZyB4bWxucz0iaHR0cDovL3d3dy53My5vcmcvMjAwMC9zdmciIHdpZHRoPSIyMjAiIGhlaWdodD0iMjg0IiB2aWV3Qm94PSIwIDAgMjIwIDI4NCIgcm9sZT0iaW1nIiA+Cjx0aXRsZT5IRVhBTE9DSyBtb2R1bGFyIGludGVyZmFjZSBhc3NldDwvdGl0bGU+CjxkZWZzPjwvZGVmcz4KICAgICAgPHJlY3QgeD0iOCIgeT0iOCIgd2lkdGg9IjIwNCIgaGVpZ2h0PSIyNjgiIHJ4PSIxNCIgZmlsbD0iIzExMUMyMiIgc3Ryb2tlPSIjQjk4NTZFIiBzdHJva2Utd2lkdGg9IjIuNiIvPgogICAgICA8cmVjdCB4PSIxMiIgeT0iMTIiIHdp ...(+3484 chars)\",\"value\":\"3\"},{\"image\":\"data:image\\/svg+xml;base64,PHN2ZyB4bWxucz0iaHR0cDovL3d3dy53My5vcmcvMjAwMC9zdmciIHdpZHRoPSIyMjAiIGhlaWdodD0iMjg0IiB2aWV3Qm94PSIwIDAgMjIwIDI4NCIgcm9sZT0iaW1nIiA+Cjx0aXRsZT5IRVhBTE9DSyBtb2R1bGFyIGludGVyZmFjZSBhc3NldDwvdGl0bGU+CjxkZWZzPjwvZGVmcz4KICAgICAgPHJlY3QgeD0iOCIgeT0iOCIgd2lkdGg9IjIwNCIgaGVpZ2h0PSIyNjgiIHJ4PSIxNCIgZmlsbD0iIzExMUMyMiIgc3Ryb2tlPSIjQjk4NTZFIiBzdHJva2Utd2lkdGg9IjIuNiIvPgogICAgICA8cmVjdCB4PSIxMiIgeT0iMTIiIHdp ...(+3532 chars)\",\"value\":\"4\"},{\"image\":\"data:image\\/svg+xml;base64,PHN2ZyB4bWxucz0iaHR0cDovL3d3dy53My5vcmcvMjAwMC9zdmciIHdpZHRoPSIyMjAiIGhlaWdodD0iMjg0IiB2aWV3Qm94PSIwIDAgMjIwIDI4NCIgcm9sZT0iaW1nIiA+Cjx0aXRsZT5IRVhBTE9DSyBtb2R1bGFyIGludGVyZmFjZSBhc3NldDwvdGl0bGU+CjxkZWZzPjwvZGVmcz4KICAgICAgPHJlY3QgeD0iOCIgeT0iOCIgd2lkdGg9IjIwNCIgaGVpZ2h0PSIyNjgiIHJ4PSIxNCIgZmlsbD0iIzExMUMyMiIgc3Ryb2tlPSIjQjk4NTZFIiBzdHJva2Utd2lkdGg9IjIuNiIvPgogICAgICA8cmVjdCB4PSIxMiIgeT0iMTIiIHdp ...(+3532 chars)\",\"value\":\"5\"},{\"image\":\"data:image\\/svg+xml;base64,PHN2ZyB4bWxucz0iaHR0cDovL3d3dy53My5vcmcvMjAwMC9zdmciIHdpZHRoPSIyMjAiIGhlaWdodD0iMjg0IiB2aWV3Qm94PSIwIDAgMjIwIDI4NCIgcm9sZT0iaW1nIiA+Cjx0aXRsZT5IRVhBTE9DSyBtb2R1bGFyIGludGVyZmFjZSBhc3NldDwvdGl0bGU+CjxkZWZzPjwvZGVmcz4KICAgICAgPHJlY3QgeD0iOCIgeT0iOCIgd2lkdGg9IjIwNCIgaGVpZ2h0PSIyNjgiIHJ4PSIxNCIgZmlsbD0iIzExMUMyMiIgc3Ryb2tlPSIjQjk4NTZFIiBzdHJva2Utd2lkdGg9IjIuNiIvPgogICAgICA8cmVjdCB4PSIxMiIgeT0iMTIiIHdp ...(+3532 chars)\",\"value\":\"6\"},{\"image\":\"data:image\\/svg+xml;base64,PHN2ZyB4bWxucz0iaHR0cDovL3d3dy53My5vcmcvMjAwMC9zdmciIHdpZHRoPSIyMjAiIGhlaWdodD0iMjg0IiB2aWV3Qm94PSIwIDAgMjIwIDI4NCIgcm9sZT0iaW1nIiA+Cjx0aXRsZT5IRVhBTE9DSyBtb2R1bGFyIGludGVyZmFjZSBhc3NldDwvdGl0bGU+CjxkZWZzPjwvZGVmcz4KICAgICAgPHJlY3QgeD0iOCIgeT0iOCIgd2lkdGg9IjIwNCIgaGVpZ2h0PSIyNjgiIHJ4PSIxNCIgZmlsbD0iIzExMUMyMiIgc3Ryb2tlPSIjQjk4NTZFIiBzdHJva2Utd2lkdGg9IjIuNiIvPgogICAgICA8cmVjdCB4PSIxMiIgeT0iMTIiIHdp ...(+3524 chars)\",\"value\":\"7\"},{\"image\":\"data:image\\/svg+xml;base64,PHN2ZyB4bWxucz0iaHR0cDovL3d3dy53My5vcmcvMjAwMC9zdmciIHdpZHRoPSIyMjAiIGhlaWdodD0iMjg0IiB2aWV3Qm94PSIwIDAgMjIwIDI4NCIgcm9sZT0iaW1nIiA+Cjx0aXRsZT5IRVhBTE9DSyBtb2R1bGFyIGludGVyZmFjZSBhc3NldDwvdGl0bGU+CjxkZWZzPjwvZGVmcz4KICAgICAgPHJlY3QgeD0iOCIgeT0iOCIgd2lkdGg9IjIwNCIgaGVpZ2h0PSIyNjgiIHJ4PSIxNCIgZmlsbD0iIzExMUMyMiIgc3Ryb2tlPSIjQjk4NTZFIiBzdHJva2Utd2lkdGg9IjIuNiIvPgogICAgICA8cmVjdCB4PSIxMiIgeT0iMTIiIHdp ...(+3532 chars)\",\"value\":\"8\"},{\"image\":\"data:image\\/svg+xml;base64,PHN2ZyB4bWxucz0iaHR0cDovL3d3dy53My5vcmcvMjAwMC9zdmciIHdpZHRoPSIyMjAiIGhlaWdodD0iMjg0IiB2aWV3Qm94PSIwIDAgMjIwIDI4NCIgcm9sZT0iaW1nIiA+Cjx0aXRsZT5IRVhBTE9DSyBtb2R1bGFyIGludGVyZmFjZSBhc3NldDwvdGl0bGU+CjxkZWZzPjwvZGVmcz4KICAgICAgPHJlY3QgeD0iOCIgeT0iOCIgd2lkdGg9IjIwNCIgaGVpZ2h0PSIyNjgiIHJ4PSIxNCIgZmlsbD0iIzExMUMyMiIgc3Ryb2tlPSIjQjk4NTZFIiBzdHJva2Utd2lkdGg9IjIuNiIvPgogICAgICA8cmVjdCB4PSIxMiIgeT0iMTIiIHdp ...(+3532 chars)\",\"value\":\"9\"},{\"image\":\"data:image\\/svg+xml;base64,PHN2ZyB4bWxucz0iaHR0cDovL3d3dy53My5vcmcvMjAwMC9zdmciIHdpZHRoPSIyMjAiIGhlaWdodD0iMjg0IiB2aWV3Qm94PSIwIDAgMjIwIDI4NCIgcm9sZT0iaW1nIiA+Cjx0aXRsZT5IRVhBTE9DSyBtb2R1bGFyIGludGVyZmFjZSBhc3NldDwvdGl0bGU+CjxkZWZzPjwvZGVmcz4KICAgICAgPHJlY3QgeD0iOCIgeT0iOCIgd2lkdGg9IjIwNCIgaGVpZ2h0PSIyNjgiIHJ4PSIxNCIgZmlsbD0iIzExMUMyMiIgc3Ryb2tlPSIjQjk4NTZFIiBzdHJva2Utd2lkdGg9IjIuNiIvPgogICAgICA8cmVjdCB4PSIxMiIgeT0iMTIiIHdp ...(+3532 chars)\",\"value\":\"10\"},{\"image\":\"data:image\\/svg+xml;base64,PHN2ZyB4bWxucz0iaHR0cDovL3d3dy53My5vcmcvMjAwMC9zdmciIHdpZHRoPSIyMjAiIGhlaWdodD0iMjg0IiB2aWV3Qm94PSIwIDAgMjIwIDI4NCIgcm9sZT0iaW1nIiA+Cjx0aXRsZT5IRVhBTE9DSyBtb2R1bGFyIGludGVyZmFjZSBhc3NldDwvdGl0bGU+CjxkZWZzPjwvZGVmcz4KICAgICAgPHJlY3QgeD0iOCIgeT0iOCIgd2lkdGg9IjIwNCIgaGVpZ2h0PSIyNjgiIHJ4PSIxNCIgZmlsbD0iIzExMUMyMiIgc3Ryb2tlPSIjNTM2NjZFIiBzdHJva2Utd2lkdGg9IjIiLz4KICAgICAgPHJlY3QgeD0iMTIiIHk9IjEyIiB3aWR0 ...(+3220 chars)\",\"value\":\"11\"},{\"image\":\"data:image\\/svg+xml;base64,PHN2ZyB4bWxucz0iaHR0cDovL3d3dy53My5vcmcvMjAwMC9zdmciIHdpZHRoPSIyMjAiIGhlaWdodD0iMjg0IiB2aWV3Qm94PSIwIDAgMjIwIDI4NCIgcm9sZT0iaW1nIiA+Cjx0aXRsZT5IRVhBTE9DSyBtb2R1bGFyIGludGVyZmFjZSBhc3NldDwvdGl0bGU+CjxkZWZzPjxsaW5lYXJHcmFkaWVudCBpZD0ia3JhZnRGcm9udCIgeDE9IjAiIHkxPSIwIiB4Mj0iMSIgeTI9IjEiPjxzdG9wIHN0b3AtY29sb3I9IiNEM0I5OUEiLz48c3RvcCBvZmZzZXQ9IjEiIHN0b3AtY29sb3I9IiNBMzgzNjMiLz48L2xpbmVhckdyYWRpZW50Pjxs ...(+4752 chars)\",\"value\":\"20\"},{\"image\":\"data:image\\/svg+xml;base64,PHN2ZyB4bWxucz0iaHR0cDovL3d3dy53My5vcmcvMjAwMC9zdmciIHdpZHRoPSIyMjAiIGhlaWdodD0iMjg0IiB2aWV3Qm94PSIwIDAgMjIwIDI4NCIgcm9sZT0iaW1nIiA+Cjx0aXRsZT5IRVhBTE9DSyBtb2R1bGFyIGludGVyZmFjZSBhc3NldDwvdGl0bGU+CjxkZWZzPjxsaW5lYXJHcmFkaWVudCBpZD0ia3JhZnRGcm9udCIgeDE9IjAiIHkxPSIwIiB4Mj0iMSIgeTI9IjEiPjxzdG9wIHN0b3AtY29sb3I9IiNEM0I5OUEiLz48c3RvcCBvZmZzZXQ9IjEiIHN0b3AtY29sb3I9IiNBMzgzNjMiLz48L2xpbmVhckdyYWRpZW50Pjxs ...(+7264 chars)\",\"value\":\"21\"},{\"image\":\"data:image\\/svg+xml;base64,PHN2ZyB4bWxucz0iaHR0cDovL3d3dy53My5vcmcvMjAwMC9zdmciIHdpZHRoPSIyMjAiIGhlaWdodD0iMjg0IiB2aWV3Qm94PSIwIDAgMjIwIDI4NCIgcm9sZT0iaW1nIiA+Cjx0aXRsZT5IRVhBTE9DSyBtb2R1bGFyIGludGVyZmFjZSBhc3NldDwvdGl0bGU+CjxkZWZzPjxsaW5lYXJHcmFkaWVudCBpZD0ia3JhZnRGcm9udCIgeDE9IjAiIHkxPSIwIiB4Mj0iMSIgeTI9IjEiPjxzdG9wIHN0b3AtY29sb3I9IiNEM0I5OUEiLz48c3RvcCBvZmZzZXQ9IjEiIHN0b3AtY29sb3I9IiNBMzgzNjMiLz48L2xpbmVhckdyYWRpZW50Pjxs ...(+7264 chars)\",\"value\":\"22\"},{\"image\":\"data:image\\/svg+xml;base64,PHN2ZyB4bWxucz0iaHR0cDovL3d3dy53My5vcmcvMjAwMC9zdmciIHdpZHRoPSIyMjAiIGhlaWdodD0iMjg0IiB2aWV3Qm94PSIwIDAgMjIwIDI4NCIgcm9sZT0iaW1nIiA+Cjx0aXRsZT5IRVhBTE9DSyBtb2R1bGFyIGludGVyZmFjZSBhc3NldDwvdGl0bGU+CjxkZWZzPjxsaW5lYXJHcmFkaWVudCBpZD0ia3JhZnRGcm9udCIgeDE9IjAiIHkxPSIwIiB4Mj0iMSIgeTI9IjEiPjxzdG9wIHN0b3AtY29sb3I9IiNEM0I5OUEiLz48c3RvcCBvZmZzZXQ9IjEiIHN0b3AtY29sb3I9IiNBMzgzNjMiLz48L2xpbmVhckdyYWRpZW50Pjxs ...(+7264 chars)\",\"value\":\"23\"},{\"image\":\"data:image\\/svg+xml;base64,PHN2ZyB4bWxucz0iaHR0cDovL3d3dy53My5vcmcvMjAwMC9zdmciIHdpZHRoPSIyMjAiIGhlaWdodD0iMjg0IiB2aWV3Qm94PSIwIDAgMjIwIDI4NCIgcm9sZT0iaW1nIiA+Cjx0aXRsZT5IRVhBTE9DSyBtb2R1bGFyIGludGVyZmFjZSBhc3NldDwvdGl0bGU+CjxkZWZzPjxsaW5lYXJHcmFkaWVudCBpZD0ia3JhZnRGcm9udCIgeDE9IjAiIHkxPSIwIiB4Mj0iMSIgeTI9IjEiPjxzdG9wIHN0b3AtY29sb3I9IiNEM0I5OUEiLz48c3RvcCBvZmZzZXQ9IjEiIHN0b3AtY29sb3I9IiNBMzgzNjMiLz48L2xpbmVhckdyYWRpZW50Pjxs ...(+7260 chars)\",\"value\":\"24\"},{\"image\":\"data:image\\/svg+xml;base64,PHN2ZyB4bWxucz0iaHR0cDovL3d3dy53My5vcmcvMjAwMC9zdmciIHdpZHRoPSIyMjAiIGhlaWdodD0iMjg0IiB2aWV3Qm94PSIwIDAgMjIwIDI4NCIgcm9sZT0iaW1nIiA+Cjx0aXRsZT5IRVhBTE9DSyBtb2R1bGFyIGludGVyZmFjZSBhc3NldDwvdGl0bGU+CjxkZWZzPjxsaW5lYXJHcmFkaWVudCBpZD0ia3JhZnRGcm9udCIgeDE9IjAiIHkxPSIwIiB4Mj0iMSIgeTI9IjEiPjxzdG9wIHN0b3AtY29sb3I9IiNEM0I5OUEiLz48c3RvcCBvZmZzZXQ9IjEiIHN0b3AtY29sb3I9IiNBMzgzNjMiLz48L2xpbmVhckdyYWRpZW50Pjxs ...(+7264 chars)\",\"value\":\"25\"},{\"image\":\"data:image\\/svg+xml;base64,PHN2ZyB4bWxucz0iaHR0cDovL3d3dy53My5vcmcvMjAwMC9zdmciIHdpZHRoPSIyMjAiIGhlaWdodD0iMjg0IiB2aWV3Qm94PSIwIDAgMjIwIDI4NCIgcm9sZT0iaW1nIiA+Cjx0aXRsZT5IRVhBTE9DSyBtb2R1bGFyIGludGVyZmFjZSBhc3NldDwvdGl0bGU+CjxkZWZzPjxsaW5lYXJHcmFkaWVudCBpZD0ia3JhZnRGcm9udCIgeDE9IjAiIHkxPSIwIiB4Mj0iMSIgeTI9IjEiPjxzdG9wIHN0b3AtY29sb3I9IiNEM0I5OUEiLz48c3RvcCBvZmZzZXQ9IjEiIHN0b3AtY29sb3I9IiNBMzgzNjMiLz48L2xpbmVhckdyYWRpZW50Pjxs ...(+7272 chars)\",\"value\":\"26\"},{\"image\":\"data:image\\/svg+xml;base64,PHN2ZyB4bWxucz0iaHR0cDovL3d3dy53My5vcmcvMjAwMC9zdmciIHdpZHRoPSIyMjAiIGhlaWdodD0iMjg0IiB2aWV3Qm94PSIwIDAgMjIwIDI4NCIgcm9sZT0iaW1nIiA+Cjx0aXRsZT5IRVhBTE9DSyBtb2R1bGFyIGludGVyZmFjZSBhc3NldDwvdGl0bGU+CjxkZWZzPjxsaW5lYXJHcmFkaWVudCBpZD0ia3JhZnRGcm9udCIgeDE9IjAiIHkxPSIwIiB4Mj0iMSIgeTI9IjEiPjxzdG9wIHN0b3AtY29sb3I9IiNEM0I5OUEiLz48c3RvcCBvZmZzZXQ9IjEiIHN0b3AtY29sb3I9IiNBMzgzNjMiLz48L2xpbmVhckdyYWRpZW50Pjxs ...(+7264 chars)\",\"value\":\"27\"},{\"image\":\"data:image\\/svg+xml;base64,PHN2ZyB4bWxucz0iaHR0cDovL3d3dy53My5vcmcvMjAwMC9zdmciIHdpZHRoPSIyMjAiIGhlaWdodD0iMjg0IiB2aWV3Qm94PSIwIDAgMjIwIDI4NCIgcm9sZT0iaW1nIiA+Cjx0aXRsZT5IRVhBTE9DSyBtb2R1bGFyIGludGVyZmFjZSBhc3NldDwvdGl0bGU+CjxkZWZzPjxsaW5lYXJHcmFkaWVudCBpZD0ia3JhZnRGcm9udCIgeDE9IjAiIHkxPSIwIiB4Mj0iMSIgeTI9IjEiPjxzdG9wIHN0b3AtY29sb3I9IiNEM0I5OUEiLz48c3RvcCBvZmZzZXQ9IjEiIHN0b3AtY29sb3I9IiNBMzgzNjMiLz48L2xpbmVhckdyYWRpZW50Pjxs ...(+7268 chars)\",\"value\":\"28\"},{\"image\":\"data:image\\/svg+xml;base64,PHN2ZyB4bWxucz0iaHR0cDovL3d3dy53My5vcmcvMjAwMC9zdmciIHdpZHRoPSIyMjAiIGhlaWdodD0iMjg0IiB2aWV3Qm94PSIwIDAgMjIwIDI4NCIgcm9sZT0iaW1nIiA+Cjx0aXRsZT5IRVhBTE9DSyBtb2R1bGFyIGludGVyZmFjZSBhc3NldDwvdGl0bGU+CjxkZWZzPjxsaW5lYXJHcmFkaWVudCBpZD0ia3JhZnRGcm9udCIgeDE9IjAiIHkxPSIwIiB4Mj0iMSIgeTI9IjEiPjxzdG9wIHN0b3AtY29sb3I9IiNEM0I5OUEiLz48c3RvcCBvZmZzZXQ9IjEiIHN0b3AtY29sb3I9IiNBMzgzNjMiLz48L2xpbmVhckdyYWRpZW50Pjxs ...(+7268 chars)\",\"value\":\"29\"},{\"image\":\"data:image\\/svg+xml;base64,PHN2ZyB4bWxucz0iaHR0cDovL3d3dy53My5vcmcvMjAwMC9zdmciIHdpZHRoPSIyMjAiIGhlaWdodD0iMjg0IiB2aWV3Qm94PSIwIDAgMjIwIDI4NCIgcm9sZT0iaW1nIiA+Cjx0aXRsZT5IRVhBTE9DSyBtb2R1bGFyIGludGVyZmFjZSBhc3NldDwvdGl0bGU+CjxkZWZzPjxsaW5lYXJHcmFkaWVudCBpZD0ia3JhZnRGcm9udCIgeDE9IjAiIHkxPSIwIiB4Mj0iMSIgeTI9IjEiPjxzdG9wIHN0b3AtY29sb3I9IiNEM0I5OUEiLz48c3RvcCBvZmZzZXQ9IjEiIHN0b3AtY29sb3I9IiNBMzgzNjMiLz48L2xpbmVhckdyYWRpZW50Pjxs ...(+7268 chars)\",\"value\":\"30\"},{\"image\":\"data:image\\/svg+xml;base64,PHN2ZyB4bWxucz0iaHR0cDovL3d3dy53My5vcmcvMjAwMC9zdmciIHdpZHRoPSIyMjAiIGhlaWdodD0iMjg0IiB2aWV3Qm94PSIwIDAgMjIwIDI4NCIgcm9sZT0iaW1nIiA+Cjx0aXRsZT5IRVhBTE9DSyBtb2R1bGFyIGludGVyZmFjZSBhc3NldDwvdGl0bGU+CjxkZWZzPjxsaW5lYXJHcmFkaWVudCBpZD0ia3JhZnRGcm9udCIgeDE9IjAiIHkxPSIwIiB4Mj0iMSIgeTI9IjEiPjxzdG9wIHN0b3AtY29sb3I9IiNEM0I5OUEiLz48c3RvcCBvZmZzZXQ9IjEiIHN0b3AtY29sb3I9IiNBMzgzNjMiLz48L2xpbmVhckdyYWRpZW50Pjxs ...(+4756 chars)\",\"value\":\"31\"},{\"image\":\"data:image\\/svg+xml;base64,PHN2ZyB4bWxucz0iaHR0cDovL3d3dy53My5vcmcvMjAwMC9zdmciIHdpZHRoPSIyMjAiIGhlaWdodD0iMjg0IiB2aWV3Qm94PSIwIDAgMjIwIDI4NCIgcm9sZT0iaW1nIiA+Cjx0aXRsZT5IRVhBTE9DSyBtb2R1bGFyIGludGVyZmFjZSBhc3NldDwvdGl0bGU+CjxkZWZzPjxsaW5lYXJHcmFkaWVudCBpZD0ia3JhZnRGcm9udCIgeDE9IjAiIHkxPSIwIiB4Mj0iMSIgeTI9IjEiPjxzdG9wIHN0b3AtY29sb3I9IiNEM0I5OUEiLz48c3RvcCBvZmZzZXQ9IjEiIHN0b3AtY29sb3I9IiNBMzgzNjMiLz48L2xpbmVhckdyYWRpZW50Pjxs ...(+4752 chars)\",\"value\":\"32\"},{\"image\":\"data:image\\/svg+xml;base64,PHN2ZyB4bWxucz0iaHR0cDovL3d3dy53My5vcmcvMjAwMC9zdmciIHdpZHRoPSIyMjAiIGhlaWdodD0iMjg0IiB2aWV3Qm94PSIwIDAgMjIwIDI4NCIgcm9sZT0iaW1nIiA+Cjx0aXRsZT5IRVhBTE9DSyBtb2R1bGFyIGludGVyZmFjZSBhc3NldDwvdGl0bGU+CjxkZWZzPjxsaW5lYXJHcmFkaWVudCBpZD0ia3JhZnRGcm9udCIgeDE9IjAiIHkxPSIwIiB4Mj0iMSIgeTI9IjEiPjxzdG9wIHN0b3AtY29sb3I9IiNEM0I5OUEiLz48c3RvcCBvZmZzZXQ9IjEiIHN0b3AtY29sb3I9IiNBMzgzNjMiLz48L2xpbmVhckdyYWRpZW50Pjxs ...(+6860 chars)\",\"value\":\"33\"},{\"image\":\"data:image\\/svg+xml;base64,PHN2ZyB4bWxucz0iaHR0cDovL3d3dy53My5vcmcvMjAwMC9zdmciIHdpZHRoPSIyMjAiIGhlaWdodD0iMjg0IiB2aWV3Qm94PSIwIDAgMjIwIDI4NCIgcm9sZT0iaW1nIiA+Cjx0aXRsZT5IRVhBTE9DSyBtb2R1bGFyIGludGVyZmFjZSBhc3NldDwvdGl0bGU+CjxkZWZzPjxsaW5lYXJHcmFkaWVudCBpZD0ia3JhZnRGcm9udCIgeDE9IjAiIHkxPSIwIiB4Mj0iMSIgeTI9IjEiPjxzdG9wIHN0b3AtY29sb3I9IiNEM0I5OUEiLz48c3RvcCBvZmZzZXQ9IjEiIHN0b3AtY29sb3I9IiNBMzgzNjMiLz48L2xpbmVhckdyYWRpZW50Pjxs ...(+6860 chars)\",\"value\":\"34\"},{\"image\":\"data:image\\/svg+xml;base64,PHN2ZyB4bWxucz0iaHR0cDovL3d3dy53My5vcmcvMjAwMC9zdmciIHdpZHRoPSIyMjAiIGhlaWdodD0iMjg0IiB2aWV3Qm94PSIwIDAgMjIwIDI4NCIgcm9sZT0iaW1nIiA+Cjx0aXRsZT5IRVhBTE9DSyBtb2R1bGFyIGludGVyZmFjZSBhc3NldDwvdGl0bGU+CjxkZWZzPjxsaW5lYXJHcmFkaWVudCBpZD0ia3JhZnRGcm9udCIgeDE9IjAiIHkxPSIwIiB4Mj0iMSIgeTI9IjEiPjxzdG9wIHN0b3AtY29sb3I9IiNEM0I5OUEiLz48c3RvcCBvZmZzZXQ9IjEiIHN0b3AtY29sb3I9IiNBMzgzNjMiLz48L2xpbmVhckdyYWRpZW50Pjxs ...(+6860 chars)\",\"value\":\"35\"},{\"image\":\"data:image\\/svg+xml;base64,PHN2ZyB4bWxucz0iaHR0cDovL3d3dy53My5vcmcvMjAwMC9zdmciIHdpZHRoPSIyMjAiIGhlaWdodD0iMjg0IiB2aWV3Qm94PSIwIDAgMjIwIDI4NCIgcm9sZT0iaW1nIiA+DQo8dGl0bGU+SEVYQUxPQ0sgbW9kdWxhciBpbnRlcmZhY2UgYXNzZXQ8L3RpdGxlPg0KPGRlZnM+PGxpbmVhckdyYWRpZW50IGlkPSJrcmFmdEZyb250IiB4MT0iMCIgeTE9IjAiIHgyPSIxIiB5Mj0iMSI+PHN0b3Agc3RvcC1jb2xvcj0iI0QzQjk5QSIvPjxzdG9wIG9mZnNldD0iMSIgc3RvcC1jb2xvcj0iI0EzODM2MyIvPjwvbGluZWFyR3JhZGllbnQ+ ...(+6912 chars)\",\"value\":\"36\"},{\"image\":\"data:image\\/svg+xml;base64,PHN2ZyB4bWxucz0iaHR0cDovL3d3dy53My5vcmcvMjAwMC9zdmciIHdpZHRoPSIyMjAiIGhlaWdodD0iMjg0IiB2aWV3Qm94PSIwIDAgMjIwIDI4NCIgcm9sZT0iaW1nIiA+DQo8dGl0bGU+SEVYQUxPQ0sgbW9kdWxhciBpbnRlcmZhY2UgYXNzZXQ8L3RpdGxlPg0KPGRlZnM+PGxpbmVhckdyYWRpZW50IGlkPSJrcmFmdEZyb250IiB4MT0iMCIgeTE9IjAiIHgyPSIxIiB5Mj0iMSI+PHN0b3Agc3RvcC1jb2xvcj0iI0QzQjk5QSIvPjxzdG9wIG9mZnNldD0iMSIgc3RvcC1jb2xvcj0iI0EzODM2MyIvPjwvbGluZWFyR3JhZGllbnQ+ ...(+6912 chars)\",\"value\":\"37\"},{\"image\":\"data:image\\/svg+xml;base64,PHN2ZyB4bWxucz0iaHR0cDovL3d3dy53My5vcmcvMjAwMC9zdmciIHdpZHRoPSIyMjAiIGhlaWdodD0iMjg0IiB2aWV3Qm94PSIwIDAgMjIwIDI4NCIgcm9sZT0iaW1nIiA+DQo8dGl0bGU+SEVYQUxPQ0sgbW9kdWxhciBpbnRlcmZhY2UgYXNzZXQ8L3RpdGxlPg0KPGRlZnM+PGxpbmVhckdyYWRpZW50IGlkPSJrcmFmdEZyb250IiB4MT0iMCIgeTE9IjAiIHgyPSIxIiB5Mj0iMSI+PHN0b3Agc3RvcC1jb2xvcj0iI0QzQjk5QSIvPjxzdG9wIG9mZnNldD0iMSIgc3RvcC1jb2xvcj0iI0EzODM2MyIvPjwvbGluZWFyR3JhZGllbnQ+ ...(+6912 chars)\",\"value\":\"38\"}],\"fixedAspectRatio\":\"on\"}},\"settings\":{\"BindingType\":\"signal\",\"backgroundColor\":[0,0,0],\"backgroundOffset\":0.14,\"backgroundOpacity\":1,\"blockOrientation\":\"Right\",\"fixedAspectRatio\":\"on\",\"showBackgroundColor\":false,\"value\":0,\"version\":\"R2026b\"},\"type\":\"MultistateImage\"}"
  Push Button : CustomTuningWebBlock  LabelPosition=Hide  ShowInitialText=on  Configuration="{\"components\":[{\"name\":\"BackgroundImageComponent\",\"settings\":{\"image\":{\"size\":[0,0],\"src\":\"default\",\"srcOrientation\":\"horizontal\"},\"position\":[0,0,1,1],\"scaleMode\":\"0\"}},{\"name\":\"ButtonStateComponent\",\"settings\":{\"buttonType\":\"momentary\",\"clickFcn\":\"\",\"image\":{\"size\":[180,45],\"srcOrientation\":\"Right\"},\"latched\":false,\"offValue\":[],\"onValue\":\"1\",\"position\":[0,0,1,1],\"pressDelay\":\"500\",\"pressFcn\":\"\",\"repeatInterval\":\"0\",\"states\":[{\"horizontalAlignment\":\"center\",\"image\":{\"position\":[0,0,1,1],\"size\":[1,1],\"src\":\"data:image\\/svg+xml;base64,PHN2ZyB3aWR0aD0iMzIwIiBoZWlnaHQ9IjExMCIgdmlld0JveD0iMCAwIDMyMCAxMTAiIGZpbGw9Im5vbmUiIHhtbG5zPSJodHRwOi8vd3d3LnczLm9yZy8yMDAwL3N2ZyI+CiAgPGRlZnM+CiAgICA8bGluZWFyR3JhZGllbnQgaWQ9ImJnIiB4MT0iMCIgeTE9IjAiIHgyPSIwIiB5Mj0iMTEwIiBncmFkaWVudFVuaXRzPSJ1c2VyU3BhY2VPblVzZSI+CiAgICAgIDxzdG9wIG9mZnNldD0iMCIgc3RvcC1jb2xvcj0iIzQ2NTE1QSIvPgogICAgICA8c3RvcCBvZmZzZXQ9IjAuNSIgc3RvcC1jb2xvcj0iIzM2NDE0OSIvPgogICAgICA8c3RvcCBvZmZzZXQ9IjEiIHN0b3AtY29sb3I9IiMyQjM0M0IiLz4KICAgIDwvbGluZWFyR3JhZGllbnQ+CiAgICA8bGluZWFyR3JhZGllbnQgaWQ9ImlubmVyR2xvdyIgeDE9IjAiIHkxPSIwIiB4Mj0iMzIwIiB5Mj0iMCIgZ3JhZGllbnRVbml0cz0idXNlclNwYWNlT25Vc2UiPgogICAgICA8c3RvcCBvZmZzZXQ9IjAiIHN0b3AtY29sb3I9IiNBMDVENDIiIHN0b3Atb3BhY2l0eT0iMC4xMiIvPgogICAgICA8c3RvcCBvZmZzZXQ9IjAuNSIgc3RvcC1jb2xvcj0iI0YwRDhDNyIgc3RvcC1vcGFjaXR5PSIwLjE4Ii8+CiAgICAgIDxzdG9wIG9mZnNldD0iMSIgc3RvcC1jb2xvcj0iI0EwNUQ0MiIgc3RvcC1vcGFjaXR5PSIwLjEyIi8+CiAgICA8L2xpbmVhckdyYWRpZW50PgogICAgPGZpbHRlciBpZD0ic2hhZG93IiB4PSItMjAiIHk9Ii0yMCIgd2lkdGg9IjM2MCIgaGVpZ2h0PSIxNTAiIGZpbHRlclVuaXRzPSJ1c2VyU3BhY2VPblVzZSI+CiAgICAgIDxmZURyb3BTaGFkb3cgZHg9IjAiIGR5PSI4IiBzdGREZXZpYXRpb249IjgiIGZsb29kLWNvbG9yPSIjMTQxODFCIiBmbG9vZC1vcGFjaXR5PSIwLjM1Ii8+CiAgICA8L2ZpbHRlcj4KICA8L2RlZnM+CiAgPGcgZmlsdGVyPSJ1cmwoI3NoYWRvdykiPgogICAgPHJlY3QgeD0iOCIgeT0iOCIgd2lkdGg9IjMwNCIgaGVpZ2h0PSI5NCIgcng9IjIyIiBmaWxsPSIjMjAyNjJCIi8+CiAgICA8cmVjdCB4PSIxMCIgeT0iMTAiIHdpZHRoPSIzMDAiIGhlaWdodD0iOTAiIHJ4PSIyMCIgZmlsbD0iI0I0NkE0QSIvPgogICAgPHJlY3QgeD0iMTMiIHk9IjEzIiB3aWR0aD0iMjk0IiBoZWlnaHQ9Ijg0IiByeD0iMTgiIGZpbGw9InVybCgjYmcpIi8+CiAgICA8cGF0aCBkPSJNMjUgMjBIMjk1QzMwMSAyMCAzMDYgMjUgMzA2IDMxVjQwSDE0VjMxQzE0IDI1IDE5IDIwIDI1IDIwWiIgZmlsbD0id2hpdGUiIGZpbGwtb3BhY2l0eT0iMC4wOCIvPgogICAgPHJlY3QgeD0iMTgiIHk9IjE4IiB3aWR0aD0iMjg0IiBoZWlnaHQ9Ijc0IiByeD0iMTQiIHN0cm9rZT0idXJsKCNpbm5lckdsb3cpIiBzdHJva2Utd2lkdGg9IjIiLz4KICAgIDxwYXRoIGQ9Ik0yOCA4NkgyOTIiIHN0cm9rZT0iIzE0MTgxQiIgc3Ryb2tlLW9wYWNpdHk9IjAuNTUiIHN0cm9rZS13aWR0aD0iMiIgc3Ryb2tlLWxpbmVjYXA9InJvdW5kIi8+CiAgPC9nPgo8L3N2Zz4K\",\"srcOrientation\":\"Right\"},\"label\":{\"color\":[0.9647058823529412,0.9490196078431372,0.9137254901960784],\"icon\":{\"size\":[0,0],\"src\":\"default\",\"srcOrientation\":\"Right\"},\"iconOffset\":0,\"iconPlacement\":\"left\",\"opacity\":1,\"show\":true,\"text\":{\"content\":\"1\",\"font\":\"Helvetica\"}},\"labelOffset\":[-0.025,0],\"verticalAlignment\":\"middle\"},{\"horizontalAlignment\":\"center\",\"image\":{\"position\":[0,0,1,1],\"size\":[1,1],\"src\":\"data:image\\/svg+xml;base64,PHN2ZyB3aWR0aD0iMzIwIiBoZWlnaHQ9IjExMCIgdmlld0JveD0iMCAwIDMyMCAxMTAiIGZpbGw9Im5vbmUiIHhtbG5zPSJodHRwOi8vd3d3LnczLm9yZy8yMDAwL3N2ZyI+CiAgPGRlZnM+CiAgICA8bGluZWFyR3JhZGllbnQgaWQ9ImJnUHJlc3NlZCIgeDE9IjAiIHkxPSIwIiB4Mj0iMCIgeTI9IjExMCIgZ3JhZGllbnRVbml0cz0idXNlclNwYWNlT25Vc2UiPgogICAgICA8c3RvcCBvZmZzZXQ9IjAiIHN0b3AtY29sb3I9IiNDMDdBNTgiLz4KICAgICAgPHN0b3Agb2Zmc2V0PSIwLjUiIHN0b3AtY29sb3I9IiNBOTVFM0UiLz4KICAgICAgPHN0b3Agb2Zmc2V0PSIxIiBzdG9wLWNvbG9yPSIjOEU0RDMzIi8+CiAgICA8L2xpbmVhckdyYWRpZW50PgogICAgPGZpbHRlciBpZD0ic2hhZG93UHJlc3NlZCIgeD0iLTIwIiB5PSItMjAiIHdpZHRoPSIzNjAiIGhlaWdodD0iMTUwIiBmaWx0ZXJVbml0cz0idXNlclNwYWNlT25Vc2UiPgogICAgICA8ZmVEcm9wU2hhZG93IGR4PSIwIiBkeT0iNCIgc3RkRGV2aWF0aW9uPSI1IiBmbG9vZC1jb2xvcj0iIzE0MTgxQiIgZmxvb2Qtb3BhY2l0eT0iMC4yNSIvPgogICAgPC9maWx0ZXI+CiAgPC9kZWZzPgogIDxnIGZpbHRlcj0idXJsKCNzaGFkb3dQcmVzc2VkKSI+CiAgICA8cmVjdCB4PSI4IiB5PSIxMiIgd2lkdGg9IjMwNCIgaGVpZ2h0PSI4OCIgcng9IjIyIiBmaWxsPSIjMjAyNjJCIi8+CiAgICA8cmVjdCB4PSIxMCIgeT0iMTQiIHdpZHRoPSIzMDAiIGhlaWdodD0iODQiIHJ4PSIyMCIgZmlsbD0iI0Q2QTE4NCIvPgogICAgPHJlY3QgeD0iMTMiIHk9IjE3IiB3aWR0aD0iMjk0IiBoZWlnaHQ9Ijc4IiByeD0iMTgiIGZpbGw9InVybCgjYmdQcmVzc2VkKSIvPgogICAgPHBhdGggZD0iTTI1IDIzSDI5NUMzMDEgMjMgMzA2IDI4IDMwNiAzNFY0MUgxNFYzNEMxNCAyOCAxOSAyMyAyNSAyM1oiIGZpbGw9IndoaXRlIiBmaWxsLW9wYWNpdHk9IjAuMTAiLz4KICAgIDxyZWN0IHg9IjE4IiB5PSIyMiIgd2lkdGg9IjI4NCIgaGVpZ2h0PSI2OCIgcng9IjE0IiBzdHJva2U9IiNGM0Q3QzQiIHN0cm9rZS1vcGFjaXR5PSIwLjQ1IiBzdHJva2Utd2lkdGg9IjIiLz4KICAgIDxwYXRoIGQ9Ik0yOCA4MkgyOTIiIHN0cm9rZT0iIzZGM0MyOCIgc3Ryb2tlLW9wYWNpdHk9IjAuNDUiIHN0cm9rZS13aWR0aD0iMiIgc3Ryb2tlLWxpbmVjYXA9InJvdW5kIi8+CiAgPC9nPgo8L3N2Zz4K\",\"srcOrientation\":\"Right\"},\"label\":{\"color\":[1,1,0.78,1],\"icon\":{\"size\":[0,0],\"src\":\"default\",\"srcOrientation\":\"Right\"},\"iconOffset\":0,\"iconPlacement\":\"left\",\"opacity\":1,\"show\":true,\"text\":{\"content\":\"1\",\"font\":\"Helvetica\"}},\"labelOffset\":[0,0],\"verticalAlignment\":\"middle\"},{\"horizontalAlignment\":\"center\",\"image\":{\"position\":[0.05,0.015,0.98,0.9],\"size\":[0.98,0.9],\"src\":\"data:image\\/svg+xml;base64,PHN2ZyB4bWxucz0iaHR0cDovL3d3dy53My5vcmcvMjAwMC9zdmciIHhtbG5zOnhsaW5rPSJodHRwOi8vd3d3LnczLm9yZy8xOTk5L3hsaW5rIiB2aWV3Qm94PSIwIDAgMTc3LjI1IDQwLjg4Ij48ZGVmcz48c3R5bGU+LmNscy0xe2ZpbGw6dXJsKCNyYWRpYWwtZ3JhZGllbnQpO30uY2xzLTJ7ZmlsbDp1cmwoI2xpbmVhci1ncmFkaWVudCk7fS5jbHMtM3tmaWxsOnVybCgjbGluZWFyLWdyYWRpZW50LTIpO308L3N0eWxlPjxyYWRpYWxHcmFkaWVudCBpZD0icmFkaWFsLWdyYWRpZW50IiBjeD0iOTAuMDkiIGN5PSIyMi42NiIgcj0i ...(+2212 chars)\",\"srcOrientation\":\"Right\"},\"label\":{\"color\":[1,1,0.78,1],\"icon\":{\"size\":[1.2,1.2],\"src\":\"data:image\\/svg+xml;base64,PHN2ZyB4bWxucz0iaHR0cDovL3d3dy53My5vcmcvMjAwMC9zdmciIHhtbG5zOnhsaW5rPSJodHRwOi8vd3d3LnczLm9yZy8xOTk5L3hsaW5rIiB2aWV3Qm94PSIwIDAgNTAgNTAiPjxkZWZzPjxzdHlsZT4uY2xzLTF7ZmlsbDojNmFiZDQ1O3N0cm9rZTojMjcyNjI2O3N0cm9rZS1taXRlcmxpbWl0OjEwO3N0cm9rZS13aWR0aDozcHg7fS5jbHMtMntmaWxsOnVybCgjbGluZWFyLWdyYWRpZW50KTt9PC9zdHlsZT48bGluZWFyR3JhZGllbnQgaWQ9ImxpbmVhci1ncmFkaWVudCIgeDE9IjI1IiB5MT0iOSIgeDI9IjI1IiB5Mj0iMzciIGdyYWRpZW50VW5pdHM9InVzZXJTcGFjZU9uVXNlIj48c3RvcCBvZmZzZXQ9IjAiIHN0b3AtY29sb3I9IiNmZmYiIHN0b3Atb3BhY2l0eT0iMC43NSIvPjxzdG9wIG9mZnNldD0iMSIgc3RvcC1jb2xvcj0iI2ZmZiIgc3RvcC1vcGFjaXR5PSIwIi8+PC9saW5lYXJHcmFkaWVudD48L2RlZnM+PGcgaWQ9Ik9uIj48Y2lyY2xlIGNsYXNzPSJjbHMtMSIgY3g9IjI1IiBjeT0iMjUiIHI9IjIwIi8+PGNpcmNsZSBjbGFzcz0iY2xzLTIiIGN4PSIyNSIgY3k9IjIzIiByPSIxNCIvPjwvZz48L3N2Zz4=\",\"srcOrientation\":\"Right\"},\"iconOffset\":0,\"iconPlacement\":\"left\",\"opacity\":1,\"show\":true,\"text\":{\"content\":\"1\",\"font\":\"Helvetica\"}},\"labelOffset\":[-0.025,0],\"verticalAlignment\":\"middle\"},{\"horizontalAlignment\":\"center\",\"image\":{\"position\":[0.05,0.015,0.98,0.9],\"size\":[0.98,0.9],\"src\":\"data:image\\/svg+xml;base64,PHN2ZyB4bWxucz0iaHR0cDovL3d3dy53My5vcmcvMjAwMC9zdmciIHhtbG5zOnhsaW5rPSJodHRwOi8vd3d3LnczLm9yZy8xOTk5L3hsaW5rIiB2aWV3Qm94PSIwIDAgMTc3LjI1IDQwLjg4Ij48ZGVmcz48c3R5bGU+LmNscy0xe2ZpbGw6dXJsKCNyYWRpYWwtZ3JhZGllbnQpO30uY2xzLTJ7ZmlsbDp1cmwoI2xpbmVhci1ncmFkaWVudCk7fS5jbHMtM3tmaWxsOnVybCgjbGluZWFyLWdyYWRpZW50LTIpO308L3N0eWxlPjxyYWRpYWxHcmFkaWVudCBpZD0icmFkaWFsLWdyYWRpZW50IiBjeD0iOTAuMDkiIGN5PSIyMi42NiIgcj0i ...(+2216 chars)\",\"srcOrientation\":\"Right\"},\"label\":{\"color\":[1,1,0.78,1],\"icon\":{\"size\":[1.2,1.2],\"src\":\"data:image\\/svg+xml;base64,PHN2ZyBpZD0iT2ZmIiB4bWxucz0iaHR0cDovL3d3dy53My5vcmcvMjAwMC9zdmciIHhtbG5zOnhsaW5rPSJodHRwOi8vd3d3LnczLm9yZy8xOTk5L3hsaW5rIiB2aWV3Qm94PSIwIDAgNTAgNTAiPjxkZWZzPjxzdHlsZT4uY2xzLTF7ZmlsbDojN2Y4MDgwO3N0cm9rZTojMjcyNjI2O3N0cm9rZS1taXRlcmxpbWl0OjEwO3N0cm9rZS13aWR0aDozcHg7fS5jbHMtMntmaWxsOnVybCgjbGluZWFyLWdyYWRpZW50KTt9PC9zdHlsZT48bGluZWFyR3JhZGllbnQgaWQ9ImxpbmVhci1ncmFkaWVudCIgeDE9IjI1IiB5MT0iOSIgeDI9IjI1IiB5Mj0iMzciIGdyYWRpZW50VW5pdHM9InVzZXJTcGFjZU9uVXNlIj48c3RvcCBvZmZzZXQ9IjAiIHN0b3AtY29sb3I9IiNmZmYiIHN0b3Atb3BhY2l0eT0iMC43NSIvPjxzdG9wIG9mZnNldD0iMSIgc3RvcC1jb2xvcj0iI2ZmZiIgc3RvcC1vcGFjaXR5PSIwIi8+PC9saW5lYXJHcmFkaWVudD48L2RlZnM+PGNpcmNsZSBjbGFzcz0iY2xzLTEiIGN4PSIyNSIgY3k9IjI1IiByPSIyMCIvPjxjaXJjbGUgY2xhc3M9ImNscy0yIiBjeD0iMjUiIGN5PSIyMyIgcj0iMTQiLz48L3N2Zz4=\",\"srcOrientation\":\"Right\"},\"iconOffset\":0,\"iconPlacement\":\"left\",\"opacity\":1,\"show\":true,\"text\":{\"content\":\"1\",\"font\":\"Helvetica\"}},\"labelOffset\":[0,0],\"verticalAlignment\":\"middle\"}]}},{\"name\":\"ForegroundImageComponent\",\"settings\":{\"image\":{\"size\":[0,0],\"src\":\"default\",\"srcOrientation\":\"horizontal\"},\"isForeground\":1,\"position\":[0,0,1,1],\"scaleMode\":\"0\"}}],\"derived\":{\"blockParameters\":{\"AutoActivate\":false,\"ButtonText\":\"1\",\"ButtonType\":\"Momentary\",\"ClickFcn\":\"\",\"OnValue\":\"1\",\"PressDelay\":\"500\",\"PressFcn\":\"\",\"RepeatInterval\":\"0\",\"fixedAspectRatio\":\"on\"}},\"settings\":{\"BindingType\":\"param\",\"aspectRatio\":3.7777777777777777,\"autoActivate\":false,\"backgroundColor\":[0,0,0,\"1\"],\"backgroundOffset\":0,\"backgroundOpacity\":1,\"fixedAspectRatio\":\"on\",\"foregroundColor\":[252,252,196],\"showBackgroundColor\":false,\"variant\":\"push\",\"version\":\"R2025a\"},\"type\":\"Button\"}"
  Push Button1 : CustomTuningWebBlock  LabelPosition=Hide  ShowInitialText=on  Configuration="{\"components\":[{\"name\":\"BackgroundImageComponent\",\"settings\":{\"image\":{\"size\":[0,0],\"src\":\"default\",\"srcOrientation\":\"horizontal\"},\"position\":[0,0,1,1],\"scaleMode\":\"0\"}},{\"name\":\"ButtonStateComponent\",\"settings\":{\"buttonType\":\"momentary\",\"clickFcn\":\"\",\"image\":{\"size\":[180,45],\"srcOrientation\":\"Right\"},\"latched\":false,\"offValue\":[],\"onValue\":\"2\",\"position\":[0,0,1,1],\"pressDelay\":\"500\",\"pressFcn\":\"\",\"repeatInterval\":\"0\",\"states\":[{\"horizontalAlignment\":\"center\",\"image\":{\"position\":[0,0,1,1],\"size\":[1,1],\"src\":\"data:image\\/svg+xml;base64,PHN2ZyB3aWR0aD0iMzIwIiBoZWlnaHQ9IjExMCIgdmlld0JveD0iMCAwIDMyMCAxMTAiIGZpbGw9Im5vbmUiIHhtbG5zPSJodHRwOi8vd3d3LnczLm9yZy8yMDAwL3N2ZyI+CiAgPGRlZnM+CiAgICA8bGluZWFyR3JhZGllbnQgaWQ9ImJnIiB4MT0iMCIgeTE9IjAiIHgyPSIwIiB5Mj0iMTEwIiBncmFkaWVudFVuaXRzPSJ1c2VyU3BhY2VPblVzZSI+CiAgICAgIDxzdG9wIG9mZnNldD0iMCIgc3RvcC1jb2xvcj0iIzQ2NTE1QSIvPgogICAgICA8c3RvcCBvZmZzZXQ9IjAuNSIgc3RvcC1jb2xvcj0iIzM2NDE0OSIvPgogICAgICA8c3RvcCBvZmZzZXQ9IjEiIHN0b3AtY29sb3I9IiMyQjM0M0IiLz4KICAgIDwvbGluZWFyR3JhZGllbnQ+CiAgICA8bGluZWFyR3JhZGllbnQgaWQ9ImlubmVyR2xvdyIgeDE9IjAiIHkxPSIwIiB4Mj0iMzIwIiB5Mj0iMCIgZ3JhZGllbnRVbml0cz0idXNlclNwYWNlT25Vc2UiPgogICAgICA8c3RvcCBvZmZzZXQ9IjAiIHN0b3AtY29sb3I9IiNBMDVENDIiIHN0b3Atb3BhY2l0eT0iMC4xMiIvPgogICAgICA8c3RvcCBvZmZzZXQ9IjAuNSIgc3RvcC1jb2xvcj0iI0YwRDhDNyIgc3RvcC1vcGFjaXR5PSIwLjE4Ii8+CiAgICAgIDxzdG9wIG9mZnNldD0iMSIgc3RvcC1jb2xvcj0iI0EwNUQ0MiIgc3RvcC1vcGFjaXR5PSIwLjEyIi8+CiAgICA8L2xpbmVhckdyYWRpZW50PgogICAgPGZpbHRlciBpZD0ic2hhZG93IiB4PSItMjAiIHk9Ii0yMCIgd2lkdGg9IjM2MCIgaGVpZ2h0PSIxNTAiIGZpbHRlclVuaXRzPSJ1c2VyU3BhY2VPblVzZSI+CiAgICAgIDxmZURyb3BTaGFkb3cgZHg9IjAiIGR5PSI4IiBzdGREZXZpYXRpb249IjgiIGZsb29kLWNvbG9yPSIjMTQxODFCIiBmbG9vZC1vcGFjaXR5PSIwLjM1Ii8+CiAgICA8L2ZpbHRlcj4KICA8L2RlZnM+CiAgPGcgZmlsdGVyPSJ1cmwoI3NoYWRvdykiPgogICAgPHJlY3QgeD0iOCIgeT0iOCIgd2lkdGg9IjMwNCIgaGVpZ2h0PSI5NCIgcng9IjIyIiBmaWxsPSIjMjAyNjJCIi8+CiAgICA8cmVjdCB4PSIxMCIgeT0iMTAiIHdpZHRoPSIzMDAiIGhlaWdodD0iOTAiIHJ4PSIyMCIgZmlsbD0iI0I0NkE0QSIvPgogICAgPHJlY3QgeD0iMTMiIHk9IjEzIiB3aWR0aD0iMjk0IiBoZWlnaHQ9Ijg0IiByeD0iMTgiIGZpbGw9InVybCgjYmcpIi8+CiAgICA8cGF0aCBkPSJNMjUgMjBIMjk1QzMwMSAyMCAzMDYgMjUgMzA2IDMxVjQwSDE0VjMxQzE0IDI1IDE5IDIwIDI1IDIwWiIgZmlsbD0id2hpdGUiIGZpbGwtb3BhY2l0eT0iMC4wOCIvPgogICAgPHJlY3QgeD0iMTgiIHk9IjE4IiB3aWR0aD0iMjg0IiBoZWlnaHQ9Ijc0IiByeD0iMTQiIHN0cm9rZT0idXJsKCNpbm5lckdsb3cpIiBzdHJva2Utd2lkdGg9IjIiLz4KICAgIDxwYXRoIGQ9Ik0yOCA4NkgyOTIiIHN0cm9rZT0iIzE0MTgxQiIgc3Ryb2tlLW9wYWNpdHk9IjAuNTUiIHN0cm9rZS13aWR0aD0iMiIgc3Ryb2tlLWxpbmVjYXA9InJvdW5kIi8+CiAgPC9nPgo8L3N2Zz4K\",\"srcOrientation\":\"Right\"},\"label\":{\"color\":[0.9647058823529412,0.9490196078431372,0.9137254901960784],\"icon\":{\"size\":[0,0],\"src\":\"default\",\"srcOrientation\":\"Right\"},\"iconOffset\":0,\"iconPlacement\":\"left\",\"opacity\":1,\"show\":true,\"text\":{\"content\":\"2\",\"font\":\"Helvetica\"}},\"labelOffset\":[-0.025,0],\"verticalAlignment\":\"middle\"},{\"horizontalAlignment\":\"center\",\"image\":{\"position\":[0,0,1,1],\"size\":[1,1],\"src\":\"data:image\\/svg+xml;base64,PHN2ZyB3aWR0aD0iMzIwIiBoZWlnaHQ9IjExMCIgdmlld0JveD0iMCAwIDMyMCAxMTAiIGZpbGw9Im5vbmUiIHhtbG5zPSJodHRwOi8vd3d3LnczLm9yZy8yMDAwL3N2ZyI+CiAgPGRlZnM+CiAgICA8bGluZWFyR3JhZGllbnQgaWQ9ImJnUHJlc3NlZCIgeDE9IjAiIHkxPSIwIiB4Mj0iMCIgeTI9IjExMCIgZ3JhZGllbnRVbml0cz0idXNlclNwYWNlT25Vc2UiPgogICAgICA8c3RvcCBvZmZzZXQ9IjAiIHN0b3AtY29sb3I9IiNDMDdBNTgiLz4KICAgICAgPHN0b3Agb2Zmc2V0PSIwLjUiIHN0b3AtY29sb3I9IiNBOTVFM0UiLz4KICAgICAgPHN0b3Agb2Zmc2V0PSIxIiBzdG9wLWNvbG9yPSIjOEU0RDMzIi8+CiAgICA8L2xpbmVhckdyYWRpZW50PgogICAgPGZpbHRlciBpZD0ic2hhZG93UHJlc3NlZCIgeD0iLTIwIiB5PSItMjAiIHdpZHRoPSIzNjAiIGhlaWdodD0iMTUwIiBmaWx0ZXJVbml0cz0idXNlclNwYWNlT25Vc2UiPgogICAgICA8ZmVEcm9wU2hhZG93IGR4PSIwIiBkeT0iNCIgc3RkRGV2aWF0aW9uPSI1IiBmbG9vZC1jb2xvcj0iIzE0MTgxQiIgZmxvb2Qtb3BhY2l0eT0iMC4yNSIvPgogICAgPC9maWx0ZXI+CiAgPC9kZWZzPgogIDxnIGZpbHRlcj0idXJsKCNzaGFkb3dQcmVzc2VkKSI+CiAgICA8cmVjdCB4PSI4IiB5PSIxMiIgd2lkdGg9IjMwNCIgaGVpZ2h0PSI4OCIgcng9IjIyIiBmaWxsPSIjMjAyNjJCIi8+CiAgICA8cmVjdCB4PSIxMCIgeT0iMTQiIHdpZHRoPSIzMDAiIGhlaWdodD0iODQiIHJ4PSIyMCIgZmlsbD0iI0Q2QTE4NCIvPgogICAgPHJlY3QgeD0iMTMiIHk9IjE3IiB3aWR0aD0iMjk0IiBoZWlnaHQ9Ijc4IiByeD0iMTgiIGZpbGw9InVybCgjYmdQcmVzc2VkKSIvPgogICAgPHBhdGggZD0iTTI1IDIzSDI5NUMzMDEgMjMgMzA2IDI4IDMwNiAzNFY0MUgxNFYzNEMxNCAyOCAxOSAyMyAyNSAyM1oiIGZpbGw9IndoaXRlIiBmaWxsLW9wYWNpdHk9IjAuMTAiLz4KICAgIDxyZWN0IHg9IjE4IiB5PSIyMiIgd2lkdGg9IjI4NCIgaGVpZ2h0PSI2OCIgcng9IjE0IiBzdHJva2U9IiNGM0Q3QzQiIHN0cm9rZS1vcGFjaXR5PSIwLjQ1IiBzdHJva2Utd2lkdGg9IjIiLz4KICAgIDxwYXRoIGQ9Ik0yOCA4MkgyOTIiIHN0cm9rZT0iIzZGM0MyOCIgc3Ryb2tlLW9wYWNpdHk9IjAuNDUiIHN0cm9rZS13aWR0aD0iMiIgc3Ryb2tlLWxpbmVjYXA9InJvdW5kIi8+CiAgPC9nPgo8L3N2Zz4K\",\"srcOrientation\":\"Right\"},\"label\":{\"color\":[1,1,0.78,1],\"icon\":{\"size\":[0,0],\"src\":\"default\",\"srcOrientation\":\"Right\"},\"iconOffset\":0,\"iconPlacement\":\"left\",\"opacity\":1,\"show\":true,\"text\":{\"content\":\"2\",\"font\":\"Helvetica\"}},\"labelOffset\":[0,0],\"verticalAlignment\":\"middle\"},{\"horizontalAlignment\":\"center\",\"image\":{\"position\":[0.05,0.015,0.98,0.9],\"size\":[0.98,0.9],\"src\":\"data:image\\/svg+xml;base64,PHN2ZyB4bWxucz0iaHR0cDovL3d3dy53My5vcmcvMjAwMC9zdmciIHhtbG5zOnhsaW5rPSJodHRwOi8vd3d3LnczLm9yZy8xOTk5L3hsaW5rIiB2aWV3Qm94PSIwIDAgMTc3LjI1IDQwLjg4Ij48ZGVmcz48c3R5bGU+LmNscy0xe2ZpbGw6dXJsKCNyYWRpYWwtZ3JhZGllbnQpO30uY2xzLTJ7ZmlsbDp1cmwoI2xpbmVhci1ncmFkaWVudCk7fS5jbHMtM3tmaWxsOnVybCgjbGluZWFyLWdyYWRpZW50LTIpO308L3N0eWxlPjxyYWRpYWxHcmFkaWVudCBpZD0icmFkaWFsLWdyYWRpZW50IiBjeD0iOTAuMDkiIGN5PSIyMi42NiIgcj0i ...(+2212 chars)\",\"srcOrientation\":\"Right\"},\"label\":{\"color\":[1,1,0.78,1],\"icon\":{\"size\":[1.2,1.2],\"src\":\"data:image\\/svg+xml;base64,PHN2ZyB4bWxucz0iaHR0cDovL3d3dy53My5vcmcvMjAwMC9zdmciIHhtbG5zOnhsaW5rPSJodHRwOi8vd3d3LnczLm9yZy8xOTk5L3hsaW5rIiB2aWV3Qm94PSIwIDAgNTAgNTAiPjxkZWZzPjxzdHlsZT4uY2xzLTF7ZmlsbDojNmFiZDQ1O3N0cm9rZTojMjcyNjI2O3N0cm9rZS1taXRlcmxpbWl0OjEwO3N0cm9rZS13aWR0aDozcHg7fS5jbHMtMntmaWxsOnVybCgjbGluZWFyLWdyYWRpZW50KTt9PC9zdHlsZT48bGluZWFyR3JhZGllbnQgaWQ9ImxpbmVhci1ncmFkaWVudCIgeDE9IjI1IiB5MT0iOSIgeDI9IjI1IiB5Mj0iMzciIGdyYWRpZW50VW5pdHM9InVzZXJTcGFjZU9uVXNlIj48c3RvcCBvZmZzZXQ9IjAiIHN0b3AtY29sb3I9IiNmZmYiIHN0b3Atb3BhY2l0eT0iMC43NSIvPjxzdG9wIG9mZnNldD0iMSIgc3RvcC1jb2xvcj0iI2ZmZiIgc3RvcC1vcGFjaXR5PSIwIi8+PC9saW5lYXJHcmFkaWVudD48L2RlZnM+PGcgaWQ9Ik9uIj48Y2lyY2xlIGNsYXNzPSJjbHMtMSIgY3g9IjI1IiBjeT0iMjUiIHI9IjIwIi8+PGNpcmNsZSBjbGFzcz0iY2xzLTIiIGN4PSIyNSIgY3k9IjIzIiByPSIxNCIvPjwvZz48L3N2Zz4=\",\"srcOrientation\":\"Right\"},\"iconOffset\":0,\"iconPlacement\":\"left\",\"opacity\":1,\"show\":true,\"text\":{\"content\":\"2\",\"font\":\"Helvetica\"}},\"labelOffset\":[-0.025,0],\"verticalAlignment\":\"middle\"},{\"horizontalAlignment\":\"center\",\"image\":{\"position\":[0.05,0.015,0.98,0.9],\"size\":[0.98,0.9],\"src\":\"data:image\\/svg+xml;base64,PHN2ZyB4bWxucz0iaHR0cDovL3d3dy53My5vcmcvMjAwMC9zdmciIHhtbG5zOnhsaW5rPSJodHRwOi8vd3d3LnczLm9yZy8xOTk5L3hsaW5rIiB2aWV3Qm94PSIwIDAgMTc3LjI1IDQwLjg4Ij48ZGVmcz48c3R5bGU+LmNscy0xe2ZpbGw6dXJsKCNyYWRpYWwtZ3JhZGllbnQpO30uY2xzLTJ7ZmlsbDp1cmwoI2xpbmVhci1ncmFkaWVudCk7fS5jbHMtM3tmaWxsOnVybCgjbGluZWFyLWdyYWRpZW50LTIpO308L3N0eWxlPjxyYWRpYWxHcmFkaWVudCBpZD0icmFkaWFsLWdyYWRpZW50IiBjeD0iOTAuMDkiIGN5PSIyMi42NiIgcj0i ...(+2216 chars)\",\"srcOrientation\":\"Right\"},\"label\":{\"color\":[1,1,0.78,1],\"icon\":{\"size\":[1.2,1.2],\"src\":\"data:image\\/svg+xml;base64,PHN2ZyBpZD0iT2ZmIiB4bWxucz0iaHR0cDovL3d3dy53My5vcmcvMjAwMC9zdmciIHhtbG5zOnhsaW5rPSJodHRwOi8vd3d3LnczLm9yZy8xOTk5L3hsaW5rIiB2aWV3Qm94PSIwIDAgNTAgNTAiPjxkZWZzPjxzdHlsZT4uY2xzLTF7ZmlsbDojN2Y4MDgwO3N0cm9rZTojMjcyNjI2O3N0cm9rZS1taXRlcmxpbWl0OjEwO3N0cm9rZS13aWR0aDozcHg7fS5jbHMtMntmaWxsOnVybCgjbGluZWFyLWdyYWRpZW50KTt9PC9zdHlsZT48bGluZWFyR3JhZGllbnQgaWQ9ImxpbmVhci1ncmFkaWVudCIgeDE9IjI1IiB5MT0iOSIgeDI9IjI1IiB5Mj0iMzciIGdyYWRpZW50VW5pdHM9InVzZXJTcGFjZU9uVXNlIj48c3RvcCBvZmZzZXQ9IjAiIHN0b3AtY29sb3I9IiNmZmYiIHN0b3Atb3BhY2l0eT0iMC43NSIvPjxzdG9wIG9mZnNldD0iMSIgc3RvcC1jb2xvcj0iI2ZmZiIgc3RvcC1vcGFjaXR5PSIwIi8+PC9saW5lYXJHcmFkaWVudD48L2RlZnM+PGNpcmNsZSBjbGFzcz0iY2xzLTEiIGN4PSIyNSIgY3k9IjI1IiByPSIyMCIvPjxjaXJjbGUgY2xhc3M9ImNscy0yIiBjeD0iMjUiIGN5PSIyMyIgcj0iMTQiLz48L3N2Zz4=\",\"srcOrientation\":\"Right\"},\"iconOffset\":0,\"iconPlacement\":\"left\",\"opacity\":1,\"show\":true,\"text\":{\"content\":\"2\",\"font\":\"Helvetica\"}},\"labelOffset\":[0,0],\"verticalAlignment\":\"middle\"}]}},{\"name\":\"ForegroundImageComponent\",\"settings\":{\"image\":{\"size\":[0,0],\"src\":\"default\",\"srcOrientation\":\"horizontal\"},\"isForeground\":1,\"position\":[0,0,1,1],\"scaleMode\":\"0\"}}],\"derived\":{\"blockParameters\":{\"AutoActivate\":false,\"ButtonText\":\"2\",\"ButtonType\":\"Momentary\",\"ClickFcn\":\"\",\"OnValue\":\"2\",\"PressDelay\":\"500\",\"PressFcn\":\"\",\"RepeatInterval\":\"0\",\"fixedAspectRatio\":\"on\"}},\"settings\":{\"BindingType\":\"param\",\"aspectRatio\":3.7777777777777777,\"autoActivate\":false,\"backgroundColor\":[0,0,0,\"1\"],\"backgroundOffset\":0,\"backgroundOpacity\":1,\"fixedAspectRatio\":\"on\",\"foregroundColor\":[252,252,196],\"showBackgroundColor\":false,\"variant\":\"push\",\"version\":\"R2025a\"},\"type\":\"Button\"}"
  Push Button10 : CustomTuningWebBlock  LabelPosition=Hide  ShowInitialText=on  Configuration="{\"components\":[{\"name\":\"BackgroundImageComponent\",\"settings\":{\"image\":{\"size\":[0,0],\"src\":\"default\",\"srcOrientation\":\"horizontal\"},\"position\":[0,0,1,1],\"scaleMode\":\"0\"}},{\"name\":\"ButtonStateComponent\",\"settings\":{\"buttonType\":\"momentary\",\"clickFcn\":\"\",\"image\":{\"size\":[180,45],\"srcOrientation\":\"Right\"},\"latched\":false,\"offValue\":[],\"onValue\":\"11\",\"position\":[0,0,1,1],\"pressDelay\":\"500\",\"pressFcn\":\"\",\"repeatInterval\":\"0\",\"states\":[{\"horizontalAlignment\":\"center\",\"image\":{\"position\":[0,0,1,1],\"size\":[1,1],\"src\":\"data:image\\/svg+xml;base64,PHN2ZyB3aWR0aD0iMzIwIiBoZWlnaHQ9IjExMCIgdmlld0JveD0iMCAwIDMyMCAxMTAiIGZpbGw9Im5vbmUiIHhtbG5zPSJodHRwOi8vd3d3LnczLm9yZy8yMDAwL3N2ZyI+CiAgPGRlZnM+CiAgICA8bGluZWFyR3JhZGllbnQgaWQ9ImJnIiB4MT0iMCIgeTE9IjAiIHgyPSIwIiB5Mj0iMTEwIiBncmFkaWVudFVuaXRzPSJ1c2VyU3BhY2VPblVzZSI+CiAgICAgIDxzdG9wIG9mZnNldD0iMCIgc3RvcC1jb2xvcj0iIzQ2NTE1QSIvPgogICAgICA8c3RvcCBvZmZzZXQ9IjAuNSIgc3RvcC1jb2xvcj0iIzM2NDE0OSIvPgogICAgICA8c3RvcCBvZmZzZXQ9IjEiIHN0b3AtY29sb3I9IiMyQjM0M0IiLz4KICAgIDwvbGluZWFyR3JhZGllbnQ+CiAgICA8bGluZWFyR3JhZGllbnQgaWQ9ImlubmVyR2xvdyIgeDE9IjAiIHkxPSIwIiB4Mj0iMzIwIiB5Mj0iMCIgZ3JhZGllbnRVbml0cz0idXNlclNwYWNlT25Vc2UiPgogICAgICA8c3RvcCBvZmZzZXQ9IjAiIHN0b3AtY29sb3I9IiNBMDVENDIiIHN0b3Atb3BhY2l0eT0iMC4xMiIvPgogICAgICA8c3RvcCBvZmZzZXQ9IjAuNSIgc3RvcC1jb2xvcj0iI0YwRDhDNyIgc3RvcC1vcGFjaXR5PSIwLjE4Ii8+CiAgICAgIDxzdG9wIG9mZnNldD0iMSIgc3RvcC1jb2xvcj0iI0EwNUQ0MiIgc3RvcC1vcGFjaXR5PSIwLjEyIi8+CiAgICA8L2xpbmVhckdyYWRpZW50PgogICAgPGZpbHRlciBpZD0ic2hhZG93IiB4PSItMjAiIHk9Ii0yMCIgd2lkdGg9IjM2MCIgaGVpZ2h0PSIxNTAiIGZpbHRlclVuaXRzPSJ1c2VyU3BhY2VPblVzZSI+CiAgICAgIDxmZURyb3BTaGFkb3cgZHg9IjAiIGR5PSI4IiBzdGREZXZpYXRpb249IjgiIGZsb29kLWNvbG9yPSIjMTQxODFCIiBmbG9vZC1vcGFjaXR5PSIwLjM1Ii8+CiAgICA8L2ZpbHRlcj4KICA8L2RlZnM+CiAgPGcgZmlsdGVyPSJ1cmwoI3NoYWRvdykiPgogICAgPHJlY3QgeD0iOCIgeT0iOCIgd2lkdGg9IjMwNCIgaGVpZ2h0PSI5NCIgcng9IjIyIiBmaWxsPSIjMjAyNjJCIi8+CiAgICA8cmVjdCB4PSIxMCIgeT0iMTAiIHdpZHRoPSIzMDAiIGhlaWdodD0iOTAiIHJ4PSIyMCIgZmlsbD0iI0I0NkE0QSIvPgogICAgPHJlY3QgeD0iMTMiIHk9IjEzIiB3aWR0aD0iMjk0IiBoZWlnaHQ9Ijg0IiByeD0iMTgiIGZpbGw9InVybCgjYmcpIi8+CiAgICA8cGF0aCBkPSJNMjUgMjBIMjk1QzMwMSAyMCAzMDYgMjUgMzA2IDMxVjQwSDE0VjMxQzE0IDI1IDE5IDIwIDI1IDIwWiIgZmlsbD0id2hpdGUiIGZpbGwtb3BhY2l0eT0iMC4wOCIvPgogICAgPHJlY3QgeD0iMTgiIHk9IjE4IiB3aWR0aD0iMjg0IiBoZWlnaHQ9Ijc0IiByeD0iMTQiIHN0cm9rZT0idXJsKCNpbm5lckdsb3cpIiBzdHJva2Utd2lkdGg9IjIiLz4KICAgIDxwYXRoIGQ9Ik0yOCA4NkgyOTIiIHN0cm9rZT0iIzE0MTgxQiIgc3Ryb2tlLW9wYWNpdHk9IjAuNTUiIHN0cm9rZS13aWR0aD0iMiIgc3Ryb2tlLWxpbmVjYXA9InJvdW5kIi8+CiAgPC9nPgo8L3N2Zz4K\",\"srcOrientation\":\"Right\"},\"label\":{\"color\":[0.9647058823529412,0.9490196078431372,0.9137254901960784],\"icon\":{\"size\":[0,0],\"src\":\"default\",\"srcOrientation\":\"Right\"},\"iconOffset\":0,\"iconPlacement\":\"left\",\"opacity\":1,\"show\":true,\"text\":{\"content\":\"*\",\"font\":\"Helvetica\"}},\"labelOffset\":[-0.025,0],\"verticalAlignment\":\"middle\"},{\"horizontalAlignment\":\"center\",\"image\":{\"position\":[0,0,1,1],\"size\":[1,1],\"src\":\"data:image\\/svg+xml;base64,PHN2ZyB3aWR0aD0iMzIwIiBoZWlnaHQ9IjExMCIgdmlld0JveD0iMCAwIDMyMCAxMTAiIGZpbGw9Im5vbmUiIHhtbG5zPSJodHRwOi8vd3d3LnczLm9yZy8yMDAwL3N2ZyI+CiAgPGRlZnM+CiAgICA8bGluZWFyR3JhZGllbnQgaWQ9ImJnUHJlc3NlZCIgeDE9IjAiIHkxPSIwIiB4Mj0iMCIgeTI9IjExMCIgZ3JhZGllbnRVbml0cz0idXNlclNwYWNlT25Vc2UiPgogICAgICA8c3RvcCBvZmZzZXQ9IjAiIHN0b3AtY29sb3I9IiNDMDdBNTgiLz4KICAgICAgPHN0b3Agb2Zmc2V0PSIwLjUiIHN0b3AtY29sb3I9IiNBOTVFM0UiLz4KICAgICAgPHN0b3Agb2Zmc2V0PSIxIiBzdG9wLWNvbG9yPSIjOEU0RDMzIi8+CiAgICA8L2xpbmVhckdyYWRpZW50PgogICAgPGZpbHRlciBpZD0ic2hhZG93UHJlc3NlZCIgeD0iLTIwIiB5PSItMjAiIHdpZHRoPSIzNjAiIGhlaWdodD0iMTUwIiBmaWx0ZXJVbml0cz0idXNlclNwYWNlT25Vc2UiPgogICAgICA8ZmVEcm9wU2hhZG93IGR4PSIwIiBkeT0iNCIgc3RkRGV2aWF0aW9uPSI1IiBmbG9vZC1jb2xvcj0iIzE0MTgxQiIgZmxvb2Qtb3BhY2l0eT0iMC4yNSIvPgogICAgPC9maWx0ZXI+CiAgPC9kZWZzPgogIDxnIGZpbHRlcj0idXJsKCNzaGFkb3dQcmVzc2VkKSI+CiAgICA8cmVjdCB4PSI4IiB5PSIxMiIgd2lkdGg9IjMwNCIgaGVpZ2h0PSI4OCIgcng9IjIyIiBmaWxsPSIjMjAyNjJCIi8+CiAgICA8cmVjdCB4PSIxMCIgeT0iMTQiIHdpZHRoPSIzMDAiIGhlaWdodD0iODQiIHJ4PSIyMCIgZmlsbD0iI0Q2QTE4NCIvPgogICAgPHJlY3QgeD0iMTMiIHk9IjE3IiB3aWR0aD0iMjk0IiBoZWlnaHQ9Ijc4IiByeD0iMTgiIGZpbGw9InVybCgjYmdQcmVzc2VkKSIvPgogICAgPHBhdGggZD0iTTI1IDIzSDI5NUMzMDEgMjMgMzA2IDI4IDMwNiAzNFY0MUgxNFYzNEMxNCAyOCAxOSAyMyAyNSAyM1oiIGZpbGw9IndoaXRlIiBmaWxsLW9wYWNpdHk9IjAuMTAiLz4KICAgIDxyZWN0IHg9IjE4IiB5PSIyMiIgd2lkdGg9IjI4NCIgaGVpZ2h0PSI2OCIgcng9IjE0IiBzdHJva2U9IiNGM0Q3QzQiIHN0cm9rZS1vcGFjaXR5PSIwLjQ1IiBzdHJva2Utd2lkdGg9IjIiLz4KICAgIDxwYXRoIGQ9Ik0yOCA4MkgyOTIiIHN0cm9rZT0iIzZGM0MyOCIgc3Ryb2tlLW9wYWNpdHk9IjAuNDUiIHN0cm9rZS13aWR0aD0iMiIgc3Ryb2tlLWxpbmVjYXA9InJvdW5kIi8+CiAgPC9nPgo8L3N2Zz4K\",\"srcOrientation\":\"Right\"},\"label\":{\"color\":[1,1,0.78,1],\"icon\":{\"size\":[0,0],\"src\":\"default\",\"srcOrientation\":\"Right\"},\"iconOffset\":0,\"iconPlacement\":\"left\",\"opacity\":1,\"show\":true,\"text\":{\"content\":\"*\",\"font\":\"Helvetica\"}},\"labelOffset\":[0,0],\"verticalAlignment\":\"middle\"},{\"horizontalAlignment\":\"center\",\"image\":{\"position\":[0.05,0.015,0.98,0.9],\"size\":[0.98,0.9],\"src\":\"data:image\\/svg+xml;base64,PHN2ZyB4bWxucz0iaHR0cDovL3d3dy53My5vcmcvMjAwMC9zdmciIHhtbG5zOnhsaW5rPSJodHRwOi8vd3d3LnczLm9yZy8xOTk5L3hsaW5rIiB2aWV3Qm94PSIwIDAgMTc3LjI1IDQwLjg4Ij48ZGVmcz48c3R5bGU+LmNscy0xe2ZpbGw6dXJsKCNyYWRpYWwtZ3JhZGllbnQpO30uY2xzLTJ7ZmlsbDp1cmwoI2xpbmVhci1ncmFkaWVudCk7fS5jbHMtM3tmaWxsOnVybCgjbGluZWFyLWdyYWRpZW50LTIpO308L3N0eWxlPjxyYWRpYWxHcmFkaWVudCBpZD0icmFkaWFsLWdyYWRpZW50IiBjeD0iOTAuMDkiIGN5PSIyMi42NiIgcj0i ...(+2212 chars)\",\"srcOrientation\":\"Right\"},\"label\":{\"color\":[1,1,0.78,1],\"icon\":{\"size\":[1.2,1.2],\"src\":\"data:image\\/svg+xml;base64,PHN2ZyB4bWxucz0iaHR0cDovL3d3dy53My5vcmcvMjAwMC9zdmciIHhtbG5zOnhsaW5rPSJodHRwOi8vd3d3LnczLm9yZy8xOTk5L3hsaW5rIiB2aWV3Qm94PSIwIDAgNTAgNTAiPjxkZWZzPjxzdHlsZT4uY2xzLTF7ZmlsbDojNmFiZDQ1O3N0cm9rZTojMjcyNjI2O3N0cm9rZS1taXRlcmxpbWl0OjEwO3N0cm9rZS13aWR0aDozcHg7fS5jbHMtMntmaWxsOnVybCgjbGluZWFyLWdyYWRpZW50KTt9PC9zdHlsZT48bGluZWFyR3JhZGllbnQgaWQ9ImxpbmVhci1ncmFkaWVudCIgeDE9IjI1IiB5MT0iOSIgeDI9IjI1IiB5Mj0iMzciIGdyYWRpZW50VW5pdHM9InVzZXJTcGFjZU9uVXNlIj48c3RvcCBvZmZzZXQ9IjAiIHN0b3AtY29sb3I9IiNmZmYiIHN0b3Atb3BhY2l0eT0iMC43NSIvPjxzdG9wIG9mZnNldD0iMSIgc3RvcC1jb2xvcj0iI2ZmZiIgc3RvcC1vcGFjaXR5PSIwIi8+PC9saW5lYXJHcmFkaWVudD48L2RlZnM+PGcgaWQ9Ik9uIj48Y2lyY2xlIGNsYXNzPSJjbHMtMSIgY3g9IjI1IiBjeT0iMjUiIHI9IjIwIi8+PGNpcmNsZSBjbGFzcz0iY2xzLTIiIGN4PSIyNSIgY3k9IjIzIiByPSIxNCIvPjwvZz48L3N2Zz4=\",\"srcOrientation\":\"Right\"},\"iconOffset\":0,\"iconPlacement\":\"left\",\"opacity\":1,\"show\":true,\"text\":{\"content\":\"*\",\"font\":\"Helvetica\"}},\"labelOffset\":[-0.025,0],\"verticalAlignment\":\"middle\"},{\"horizontalAlignment\":\"center\",\"image\":{\"position\":[0.05,0.015,0.98,0.9],\"size\":[0.98,0.9],\"src\":\"data:image\\/svg+xml;base64,PHN2ZyB4bWxucz0iaHR0cDovL3d3dy53My5vcmcvMjAwMC9zdmciIHhtbG5zOnhsaW5rPSJodHRwOi8vd3d3LnczLm9yZy8xOTk5L3hsaW5rIiB2aWV3Qm94PSIwIDAgMTc3LjI1IDQwLjg4Ij48ZGVmcz48c3R5bGU+LmNscy0xe2ZpbGw6dXJsKCNyYWRpYWwtZ3JhZGllbnQpO30uY2xzLTJ7ZmlsbDp1cmwoI2xpbmVhci1ncmFkaWVudCk7fS5jbHMtM3tmaWxsOnVybCgjbGluZWFyLWdyYWRpZW50LTIpO308L3N0eWxlPjxyYWRpYWxHcmFkaWVudCBpZD0icmFkaWFsLWdyYWRpZW50IiBjeD0iOTAuMDkiIGN5PSIyMi42NiIgcj0i ...(+2216 chars)\",\"srcOrientation\":\"Right\"},\"label\":{\"color\":[1,1,0.78,1],\"icon\":{\"size\":[1.2,1.2],\"src\":\"data:image\\/svg+xml;base64,PHN2ZyBpZD0iT2ZmIiB4bWxucz0iaHR0cDovL3d3dy53My5vcmcvMjAwMC9zdmciIHhtbG5zOnhsaW5rPSJodHRwOi8vd3d3LnczLm9yZy8xOTk5L3hsaW5rIiB2aWV3Qm94PSIwIDAgNTAgNTAiPjxkZWZzPjxzdHlsZT4uY2xzLTF7ZmlsbDojN2Y4MDgwO3N0cm9rZTojMjcyNjI2O3N0cm9rZS1taXRlcmxpbWl0OjEwO3N0cm9rZS13aWR0aDozcHg7fS5jbHMtMntmaWxsOnVybCgjbGluZWFyLWdyYWRpZW50KTt9PC9zdHlsZT48bGluZWFyR3JhZGllbnQgaWQ9ImxpbmVhci1ncmFkaWVudCIgeDE9IjI1IiB5MT0iOSIgeDI9IjI1IiB5Mj0iMzciIGdyYWRpZW50VW5pdHM9InVzZXJTcGFjZU9uVXNlIj48c3RvcCBvZmZzZXQ9IjAiIHN0b3AtY29sb3I9IiNmZmYiIHN0b3Atb3BhY2l0eT0iMC43NSIvPjxzdG9wIG9mZnNldD0iMSIgc3RvcC1jb2xvcj0iI2ZmZiIgc3RvcC1vcGFjaXR5PSIwIi8+PC9saW5lYXJHcmFkaWVudD48L2RlZnM+PGNpcmNsZSBjbGFzcz0iY2xzLTEiIGN4PSIyNSIgY3k9IjI1IiByPSIyMCIvPjxjaXJjbGUgY2xhc3M9ImNscy0yIiBjeD0iMjUiIGN5PSIyMyIgcj0iMTQiLz48L3N2Zz4=\",\"srcOrientation\":\"Right\"},\"iconOffset\":0,\"iconPlacement\":\"left\",\"opacity\":1,\"show\":true,\"text\":{\"content\":\"*\",\"font\":\"Helvetica\"}},\"labelOffset\":[0,0],\"verticalAlignment\":\"middle\"}]}},{\"name\":\"ForegroundImageComponent\",\"settings\":{\"image\":{\"size\":[0,0],\"src\":\"default\",\"srcOrientation\":\"horizontal\"},\"isForeground\":1,\"position\":[0,0,1,1],\"scaleMode\":\"0\"}}],\"derived\":{\"blockParameters\":{\"AutoActivate\":false,\"ButtonText\":\"*\",\"ButtonType\":\"Momentary\",\"ClickFcn\":\"\",\"OnValue\":\"11\",\"PressDelay\":\"500\",\"PressFcn\":\"\",\"RepeatInterval\":\"0\",\"fixedAspectRatio\":\"on\"}},\"settings\":{\"BindingType\":\"param\",\"aspectRatio\":3.7777777777777777,\"autoActivate\":false,\"backgroundColor\":[0,0,0,\"1\"],\"backgroundOffset\":0,\"backgroundOpacity\":1,\"fixedAspectRatio\":\"on\",\"foregroundColor\":[252,252,196],\"showBackgroundColor\":false,\"variant\":\"push\",\"version\":\"R2025a\"},\"type\":\"Button\"}"
  Push Button11 : CustomTuningWebBlock  LabelPosition=Hide  ShowInitialText=on  Configuration="{\"components\":[{\"name\":\"BackgroundImageComponent\",\"settings\":{\"image\":{\"size\":[0,0],\"src\":\"default\",\"srcOrientation\":\"horizontal\"},\"position\":[0,0,1,1],\"scaleMode\":\"0\"}},{\"name\":\"ButtonStateComponent\",\"settings\":{\"buttonType\":\"momentary\",\"clickFcn\":\"\",\"image\":{\"size\":[180,45],\"srcOrientation\":\"Right\"},\"latched\":false,\"offValue\":[],\"onValue\":\"12\",\"position\":[0,0,1,1],\"pressDelay\":\"500\",\"pressFcn\":\"\",\"repeatInterval\":\"0\",\"states\":[{\"horizontalAlignment\":\"center\",\"image\":{\"position\":[0,0,1,1],\"size\":[1,1],\"src\":\"data:image\\/svg+xml;base64,PHN2ZyB3aWR0aD0iMzIwIiBoZWlnaHQ9IjExMCIgdmlld0JveD0iMCAwIDMyMCAxMTAiIGZpbGw9Im5vbmUiIHhtbG5zPSJodHRwOi8vd3d3LnczLm9yZy8yMDAwL3N2ZyI+CiAgPGRlZnM+CiAgICA8bGluZWFyR3JhZGllbnQgaWQ9ImJnIiB4MT0iMCIgeTE9IjAiIHgyPSIwIiB5Mj0iMTEwIiBncmFkaWVudFVuaXRzPSJ1c2VyU3BhY2VPblVzZSI+CiAgICAgIDxzdG9wIG9mZnNldD0iMCIgc3RvcC1jb2xvcj0iIzQ2NTE1QSIvPgogICAgICA8c3RvcCBvZmZzZXQ9IjAuNSIgc3RvcC1jb2xvcj0iIzM2NDE0OSIvPgogICAgICA8c3RvcCBvZmZzZXQ9IjEiIHN0b3AtY29sb3I9IiMyQjM0M0IiLz4KICAgIDwvbGluZWFyR3JhZGllbnQ+CiAgICA8bGluZWFyR3JhZGllbnQgaWQ9ImlubmVyR2xvdyIgeDE9IjAiIHkxPSIwIiB4Mj0iMzIwIiB5Mj0iMCIgZ3JhZGllbnRVbml0cz0idXNlclNwYWNlT25Vc2UiPgogICAgICA8c3RvcCBvZmZzZXQ9IjAiIHN0b3AtY29sb3I9IiNBMDVENDIiIHN0b3Atb3BhY2l0eT0iMC4xMiIvPgogICAgICA8c3RvcCBvZmZzZXQ9IjAuNSIgc3RvcC1jb2xvcj0iI0YwRDhDNyIgc3RvcC1vcGFjaXR5PSIwLjE4Ii8+CiAgICAgIDxzdG9wIG9mZnNldD0iMSIgc3RvcC1jb2xvcj0iI0EwNUQ0MiIgc3RvcC1vcGFjaXR5PSIwLjEyIi8+CiAgICA8L2xpbmVhckdyYWRpZW50PgogICAgPGZpbHRlciBpZD0ic2hhZG93IiB4PSItMjAiIHk9Ii0yMCIgd2lkdGg9IjM2MCIgaGVpZ2h0PSIxNTAiIGZpbHRlclVuaXRzPSJ1c2VyU3BhY2VPblVzZSI+CiAgICAgIDxmZURyb3BTaGFkb3cgZHg9IjAiIGR5PSI4IiBzdGREZXZpYXRpb249IjgiIGZsb29kLWNvbG9yPSIjMTQxODFCIiBmbG9vZC1vcGFjaXR5PSIwLjM1Ii8+CiAgICA8L2ZpbHRlcj4KICA8L2RlZnM+CiAgPGcgZmlsdGVyPSJ1cmwoI3NoYWRvdykiPgogICAgPHJlY3QgeD0iOCIgeT0iOCIgd2lkdGg9IjMwNCIgaGVpZ2h0PSI5NCIgcng9IjIyIiBmaWxsPSIjMjAyNjJCIi8+CiAgICA8cmVjdCB4PSIxMCIgeT0iMTAiIHdpZHRoPSIzMDAiIGhlaWdodD0iOTAiIHJ4PSIyMCIgZmlsbD0iI0I0NkE0QSIvPgogICAgPHJlY3QgeD0iMTMiIHk9IjEzIiB3aWR0aD0iMjk0IiBoZWlnaHQ9Ijg0IiByeD0iMTgiIGZpbGw9InVybCgjYmcpIi8+CiAgICA8cGF0aCBkPSJNMjUgMjBIMjk1QzMwMSAyMCAzMDYgMjUgMzA2IDMxVjQwSDE0VjMxQzE0IDI1IDE5IDIwIDI1IDIwWiIgZmlsbD0id2hpdGUiIGZpbGwtb3BhY2l0eT0iMC4wOCIvPgogICAgPHJlY3QgeD0iMTgiIHk9IjE4IiB3aWR0aD0iMjg0IiBoZWlnaHQ9Ijc0IiByeD0iMTQiIHN0cm9rZT0idXJsKCNpbm5lckdsb3cpIiBzdHJva2Utd2lkdGg9IjIiLz4KICAgIDxwYXRoIGQ9Ik0yOCA4NkgyOTIiIHN0cm9rZT0iIzE0MTgxQiIgc3Ryb2tlLW9wYWNpdHk9IjAuNTUiIHN0cm9rZS13aWR0aD0iMiIgc3Ryb2tlLWxpbmVjYXA9InJvdW5kIi8+CiAgPC9nPgo8L3N2Zz4K\",\"srcOrientation\":\"Right\"},\"label\":{\"color\":[0.9647058823529412,0.9490196078431372,0.9137254901960784],\"icon\":{\"size\":[0,0],\"src\":\"default\",\"srcOrientation\":\"Right\"},\"iconOffset\":0,\"iconPlacement\":\"left\",\"opacity\":1,\"show\":true,\"text\":{\"content\":\"#\",\"font\":\"Helvetica\"}},\"labelOffset\":[-0.025,0],\"verticalAlignment\":\"middle\"},{\"horizontalAlignment\":\"center\",\"image\":{\"position\":[0.05,0.015,0.98,0.9],\"size\":[0.98,0.9],\"src\":\"data:image\\/svg+xml;base64,PHN2ZyB4bWxucz0iaHR0cDovL3d3dy53My5vcmcvMjAwMC9zdmciIHhtbG5zOnhsaW5rPSJodHRwOi8vd3d3LnczLm9yZy8xOTk5L3hsaW5rIiB2aWV3Qm94PSIwIDAgMTc3LjI1IDQwLjg4Ij48ZGVmcz48c3R5bGU+LmNscy0xe2ZpbGw6dXJsKCNyYWRpYWwtZ3JhZGllbnQpO30uY2xzLTJ7ZmlsbDp1cmwoI2xpbmVhci1ncmFkaWVudCk7fS5jbHMtM3tmaWxsOnVybCgjbGluZWFyLWdyYWRpZW50LTIpO308L3N0eWxlPjxyYWRpYWxHcmFkaWVudCBpZD0icmFkaWFsLWdyYWRpZW50IiBjeD0iOTAuMDkiIGN5PSIyMi42NiIgcj0i ...(+2216 chars)\",\"srcOrientation\":\"Right\"},\"label\":{\"color\":[1,1,0.78,1],\"icon\":{\"size\":[1.2,1.2],\"src\":\"data:image\\/svg+xml;base64,PHN2ZyB4bWxucz0iaHR0cDovL3d3dy53My5vcmcvMjAwMC9zdmciIHhtbG5zOnhsaW5rPSJodHRwOi8vd3d3LnczLm9yZy8xOTk5L3hsaW5rIiB2aWV3Qm94PSIwIDAgNTAgNTAiPjxkZWZzPjxzdHlsZT4uY2xzLTF7ZmlsbDojNmFiZDQ1O3N0cm9rZTojMjcyNjI2O3N0cm9rZS1taXRlcmxpbWl0OjEwO3N0cm9rZS13aWR0aDozcHg7fS5jbHMtMntmaWxsOnVybCgjbGluZWFyLWdyYWRpZW50KTt9PC9zdHlsZT48bGluZWFyR3JhZGllbnQgaWQ9ImxpbmVhci1ncmFkaWVudCIgeDE9IjI1IiB5MT0iOSIgeDI9IjI1IiB5Mj0iMzciIGdyYWRpZW50VW5pdHM9InVzZXJTcGFjZU9uVXNlIj48c3RvcCBvZmZzZXQ9IjAiIHN0b3AtY29sb3I9IiNmZmYiIHN0b3Atb3BhY2l0eT0iMC43NSIvPjxzdG9wIG9mZnNldD0iMSIgc3RvcC1jb2xvcj0iI2ZmZiIgc3RvcC1vcGFjaXR5PSIwIi8+PC9saW5lYXJHcmFkaWVudD48L2RlZnM+PGcgaWQ9Ik9uIj48Y2lyY2xlIGNsYXNzPSJjbHMtMSIgY3g9IjI1IiBjeT0iMjUiIHI9IjIwIi8+PGNpcmNsZSBjbGFzcz0iY2xzLTIiIGN4PSIyNSIgY3k9IjIzIiByPSIxNCIvPjwvZz48L3N2Zz4=\",\"srcOrientation\":\"Right\"},\"iconOffset\":0,\"iconPlacement\":\"left\",\"opacity\":1,\"show\":true,\"text\":{\"content\":\"#\",\"font\":\"Helvetica\"}},\"labelOffset\":[0,0],\"verticalAlignment\":\"middle\"},{\"horizontalAlignment\":\"center\",\"image\":{\"position\":[0.05,0.015,0.98,0.9],\"size\":[0.98,0.9],\"src\":\"data:image\\/svg+xml;base64,PHN2ZyB4bWxucz0iaHR0cDovL3d3dy53My5vcmcvMjAwMC9zdmciIHhtbG5zOnhsaW5rPSJodHRwOi8vd3d3LnczLm9yZy8xOTk5L3hsaW5rIiB2aWV3Qm94PSIwIDAgMTc3LjI1IDQwLjg4Ij48ZGVmcz48c3R5bGU+LmNscy0xe2ZpbGw6dXJsKCNyYWRpYWwtZ3JhZGllbnQpO30uY2xzLTJ7ZmlsbDp1cmwoI2xpbmVhci1ncmFkaWVudCk7fS5jbHMtM3tmaWxsOnVybCgjbGluZWFyLWdyYWRpZW50LTIpO308L3N0eWxlPjxyYWRpYWxHcmFkaWVudCBpZD0icmFkaWFsLWdyYWRpZW50IiBjeD0iOTAuMDkiIGN5PSIyMi42NiIgcj0i ...(+2212 chars)\",\"srcOrientation\":\"Right\"},\"label\":{\"color\":[1,1,0.78,1],\"icon\":{\"size\":[1.2,1.2],\"src\":\"data:image\\/svg+xml;base64,PHN2ZyB4bWxucz0iaHR0cDovL3d3dy53My5vcmcvMjAwMC9zdmciIHhtbG5zOnhsaW5rPSJodHRwOi8vd3d3LnczLm9yZy8xOTk5L3hsaW5rIiB2aWV3Qm94PSIwIDAgNTAgNTAiPjxkZWZzPjxzdHlsZT4uY2xzLTF7ZmlsbDojNmFiZDQ1O3N0cm9rZTojMjcyNjI2O3N0cm9rZS1taXRlcmxpbWl0OjEwO3N0cm9rZS13aWR0aDozcHg7fS5jbHMtMntmaWxsOnVybCgjbGluZWFyLWdyYWRpZW50KTt9PC9zdHlsZT48bGluZWFyR3JhZGllbnQgaWQ9ImxpbmVhci1ncmFkaWVudCIgeDE9IjI1IiB5MT0iOSIgeDI9IjI1IiB5Mj0iMzciIGdyYWRpZW50VW5pdHM9InVzZXJTcGFjZU9uVXNlIj48c3RvcCBvZmZzZXQ9IjAiIHN0b3AtY29sb3I9IiNmZmYiIHN0b3Atb3BhY2l0eT0iMC43NSIvPjxzdG9wIG9mZnNldD0iMSIgc3RvcC1jb2xvcj0iI2ZmZiIgc3RvcC1vcGFjaXR5PSIwIi8+PC9saW5lYXJHcmFkaWVudD48L2RlZnM+PGcgaWQ9Ik9uIj48Y2lyY2xlIGNsYXNzPSJjbHMtMSIgY3g9IjI1IiBjeT0iMjUiIHI9IjIwIi8+PGNpcmNsZSBjbGFzcz0iY2xzLTIiIGN4PSIyNSIgY3k9IjIzIiByPSIxNCIvPjwvZz48L3N2Zz4=\",\"srcOrientation\":\"Right\"},\"iconOffset\":0,\"iconPlacement\":\"left\",\"opacity\":1,\"show\":true,\"text\":{\"content\":\"#\",\"font\":\"Helvetica\"}},\"labelOffset\":[-0.025,0],\"verticalAlignment\":\"middle\"},{\"horizontalAlignment\":\"center\",\"image\":{\"position\":[0.05,0.015,0.98,0.9],\"size\":[0.98,0.9],\"src\":\"data:image\\/svg+xml;base64,PHN2ZyB4bWxucz0iaHR0cDovL3d3dy53My5vcmcvMjAwMC9zdmciIHhtbG5zOnhsaW5rPSJodHRwOi8vd3d3LnczLm9yZy8xOTk5L3hsaW5rIiB2aWV3Qm94PSIwIDAgMTc3LjI1IDQwLjg4Ij48ZGVmcz48c3R5bGU+LmNscy0xe2ZpbGw6dXJsKCNyYWRpYWwtZ3JhZGllbnQpO30uY2xzLTJ7ZmlsbDp1cmwoI2xpbmVhci1ncmFkaWVudCk7fS5jbHMtM3tmaWxsOnVybCgjbGluZWFyLWdyYWRpZW50LTIpO308L3N0eWxlPjxyYWRpYWxHcmFkaWVudCBpZD0icmFkaWFsLWdyYWRpZW50IiBjeD0iOTAuMDkiIGN5PSIyMi42NiIgcj0i ...(+2216 chars)\",\"srcOrientation\":\"Right\"},\"label\":{\"color\":[1,1,0.78,1],\"icon\":{\"size\":[1.2,1.2],\"src\":\"data:image\\/svg+xml;base64,PHN2ZyBpZD0iT2ZmIiB4bWxucz0iaHR0cDovL3d3dy53My5vcmcvMjAwMC9zdmciIHhtbG5zOnhsaW5rPSJodHRwOi8vd3d3LnczLm9yZy8xOTk5L3hsaW5rIiB2aWV3Qm94PSIwIDAgNTAgNTAiPjxkZWZzPjxzdHlsZT4uY2xzLTF7ZmlsbDojN2Y4MDgwO3N0cm9rZTojMjcyNjI2O3N0cm9rZS1taXRlcmxpbWl0OjEwO3N0cm9rZS13aWR0aDozcHg7fS5jbHMtMntmaWxsOnVybCgjbGluZWFyLWdyYWRpZW50KTt9PC9zdHlsZT48bGluZWFyR3JhZGllbnQgaWQ9ImxpbmVhci1ncmFkaWVudCIgeDE9IjI1IiB5MT0iOSIgeDI9IjI1IiB5Mj0iMzciIGdyYWRpZW50VW5pdHM9InVzZXJTcGFjZU9uVXNlIj48c3RvcCBvZmZzZXQ9IjAiIHN0b3AtY29sb3I9IiNmZmYiIHN0b3Atb3BhY2l0eT0iMC43NSIvPjxzdG9wIG9mZnNldD0iMSIgc3RvcC1jb2xvcj0iI2ZmZiIgc3RvcC1vcGFjaXR5PSIwIi8+PC9saW5lYXJHcmFkaWVudD48L2RlZnM+PGNpcmNsZSBjbGFzcz0iY2xzLTEiIGN4PSIyNSIgY3k9IjI1IiByPSIyMCIvPjxjaXJjbGUgY2xhc3M9ImNscy0yIiBjeD0iMjUiIGN5PSIyMyIgcj0iMTQiLz48L3N2Zz4=\",\"srcOrientation\":\"Right\"},\"iconOffset\":0,\"iconPlacement\":\"left\",\"opacity\":1,\"show\":true,\"text\":{\"content\":\"#\",\"font\":\"Helvetica\"}},\"labelOffset\":[0,0],\"verticalAlignment\":\"middle\"}]}},{\"name\":\"ForegroundImageComponent\",\"settings\":{\"image\":{\"size\":[0,0],\"src\":\"default\",\"srcOrientation\":\"horizontal\"},\"isForeground\":1,\"position\":[0,0,1,1],\"scaleMode\":\"0\"}}],\"derived\":{\"blockParameters\":{\"AutoActivate\":false,\"ButtonText\":\"#\",\"ButtonType\":\"Momentary\",\"ClickFcn\":\"\",\"OnValue\":\"12\",\"PressDelay\":\"500\",\"PressFcn\":\"\",\"RepeatInterval\":\"0\",\"fixedAspectRatio\":\"on\"}},\"settings\":{\"BindingType\":\"param\",\"aspectRatio\":3.7777777777777777,\"autoActivate\":false,\"backgroundColor\":[0,0,0,\"1\"],\"backgroundOffset\":0,\"backgroundOpacity\":1,\"fixedAspectRatio\":\"on\",\"foregroundColor\":[252,252,196],\"showBackgroundColor\":false,\"variant\":\"push\",\"version\":\"R2025a\"},\"type\":\"Button\"}"
  Push Button12 : CustomTuningWebBlock  LabelPosition=Hide  ShowInitialText=on  Configuration="{\"components\":[{\"name\":\"BackgroundImageComponent\",\"settings\":{\"image\":{\"size\":[0,0],\"src\":\"default\",\"srcOrientation\":\"horizontal\"},\"position\":[0,0,1,1],\"scaleMode\":\"0\"}},{\"name\":\"ButtonStateComponent\",\"settings\":{\"buttonType\":\"momentary\",\"clickFcn\":\"\",\"image\":{\"size\":[180,45],\"srcOrientation\":\"Right\"},\"latched\":false,\"offValue\":[],\"onValue\":\"1\",\"position\":[0,0,1,1],\"pressDelay\":\"500\",\"pressFcn\":\"\",\"repeatInterval\":\"0\",\"states\":[{\"horizontalAlignment\":\"center\",\"image\":{\"position\":[0,0,1,1],\"size\":[1,1],\"src\":\"data:image\\/svg+xml;base64,PHN2ZyB3aWR0aD0iNDIwIiBoZWlnaHQ9IjEyMCIgdmlld0JveD0iMCAwIDQyMCAxMjAiIGZpbGw9Im5vbmUiIHhtbG5zPSJodHRwOi8vd3d3LnczLm9yZy8yMDAwL3N2ZyI+CiAgPGRlZnM+CiAgICA8bGluZWFyR3JhZGllbnQgaWQ9ImJnUGxhY2VkIiB4MT0iMCIgeTE9IjAiIHgyPSIwIiB5Mj0iMTIwIiBncmFkaWVudFVuaXRzPSJ1c2VyU3BhY2VPblVzZSI+CiAgICAgIDxzdG9wIG9mZnNldD0iMCIgc3RvcC1jb2xvcj0iIzMzNUM1NSIvPgogICAgICA8c3RvcCBvZmZzZXQ9IjAuNTIiIHN0b3AtY29sb3I9IiMyNzRBNDQiLz4K ...(+2372 chars)\",\"srcOrientation\":\"Right\"},\"label\":{\"color\":[0.9647058823529412,0.9490196078431372,0.9137254901960784],\"icon\":{\"size\":[0,0],\"src\":\"default\",\"srcOrientation\":\"Right\"},\"iconOffset\":0,\"iconPlacement\":\"left\",\"opacity\":1,\"show\":true,\"text\":{\"content\":\"   Object Placed\",\"font\":\"Helvetica\"}},\"labelOffset\":[0,0.055],\"verticalAlignment\":\"middle\"},{\"horizontalAlignment\":\"center\",\"image\":{\"position\":[0,0,1,1],\"size\":[1,1],\"src\":\"data:image\\/svg+xml;base64,PHN2ZyB3aWR0aD0iNDIwIiBoZWlnaHQ9IjEyMCIgdmlld0JveD0iMCAwIDQyMCAxMjAiIGZpbGw9Im5vbmUiIHhtbG5zPSJodHRwOi8vd3d3LnczLm9yZy8yMDAwL3N2ZyI+CiAgPGRlZnM+CiAgICA8bGluZWFyR3JhZGllbnQgaWQ9ImJnUGxhY2VkUHJlc3NlZCIgeDE9IjAiIHkxPSIwIiB4Mj0iMCIgeTI9IjEyMCIgZ3JhZGllbnRVbml0cz0idXNlclNwYWNlT25Vc2UiPgogICAgICA8c3RvcCBvZmZzZXQ9IjAiIHN0b3AtY29sb3I9IiM1QThFODQiLz4KICAgICAgPHN0b3Agb2Zmc2V0PSIwLjUyIiBzdG9wLWNvbG9yPSIjNDQ3 ...(+1996 chars)\",\"srcOrientation\":\"Right\"},\"label\":{\"color\":[1,1,0.78,1],\"icon\":{\"size\":[0,0],\"src\":\"default\",\"srcOrientation\":\"Right\"},\"iconOffset\":0,\"iconPlacement\":\"left\",\"opacity\":1,\"show\":true,\"text\":{\"content\":\"Object Placed\",\"font\":\"Helvetica\"}},\"labelOffset\":[0,0.055],\"verticalAlignment\":\"middle\"},{\"horizontalAlignment\":\"center\",\"image\":{\"position\":[0.05,0.015,0.98,0.9],\"size\":[0.98,0.9],\"src\":\"data:image\\/svg+xml;base64,PHN2ZyB4bWxucz0iaHR0cDovL3d3dy53My5vcmcvMjAwMC9zdmciIHhtbG5zOnhsaW5rPSJodHRwOi8vd3d3LnczLm9yZy8xOTk5L3hsaW5rIiB2aWV3Qm94PSIwIDAgMTc3LjI1IDQwLjg4Ij48ZGVmcz48c3R5bGU+LmNscy0xe2ZpbGw6dXJsKCNyYWRpYWwtZ3JhZGllbnQpO30uY2xzLTJ7ZmlsbDp1cmwoI2xpbmVhci1ncmFkaWVudCk7fS5jbHMtM3tmaWxsOnVybCgjbGluZWFyLWdyYWRpZW50LTIpO308L3N0eWxlPjxyYWRpYWxHcmFkaWVudCBpZD0icmFkaWFsLWdyYWRpZW50IiBjeD0iOTAuMDkiIGN5PSIyMi42NiIgcj0i ...(+2212 chars)\",\"srcOrientation\":\"Right\"},\"label\":{\"color\":[1,1,0.78,1],\"icon\":{\"size\":[1.2,1.2],\"src\":\"data:image\\/svg+xml;base64,PHN2ZyB4bWxucz0iaHR0cDovL3d3dy53My5vcmcvMjAwMC9zdmciIHhtbG5zOnhsaW5rPSJodHRwOi8vd3d3LnczLm9yZy8xOTk5L3hsaW5rIiB2aWV3Qm94PSIwIDAgNTAgNTAiPjxkZWZzPjxzdHlsZT4uY2xzLTF7ZmlsbDojNmFiZDQ1O3N0cm9rZTojMjcyNjI2O3N0cm9rZS1taXRlcmxpbWl0OjEwO3N0cm9rZS13aWR0aDozcHg7fS5jbHMtMntmaWxsOnVybCgjbGluZWFyLWdyYWRpZW50KTt9PC9zdHlsZT48bGluZWFyR3JhZGllbnQgaWQ9ImxpbmVhci1ncmFkaWVudCIgeDE9IjI1IiB5MT0iOSIgeDI9IjI1IiB5Mj0iMzciIGdyYWRpZW50VW5pdHM9InVzZXJTcGFjZU9uVXNlIj48c3RvcCBvZmZzZXQ9IjAiIHN0b3AtY29sb3I9IiNmZmYiIHN0b3Atb3BhY2l0eT0iMC43NSIvPjxzdG9wIG9mZnNldD0iMSIgc3RvcC1jb2xvcj0iI2ZmZiIgc3RvcC1vcGFjaXR5PSIwIi8+PC9saW5lYXJHcmFkaWVudD48L2RlZnM+PGcgaWQ9Ik9uIj48Y2lyY2xlIGNsYXNzPSJjbHMtMSIgY3g9IjI1IiBjeT0iMjUiIHI9IjIwIi8+PGNpcmNsZSBjbGFzcz0iY2xzLTIiIGN4PSIyNSIgY3k9IjIzIiByPSIxNCIvPjwvZz48L3N2Zz4=\",\"srcOrientation\":\"Right\"},\"iconOffset\":0,\"iconPlacement\":\"left\",\"opacity\":1,\"show\":true,\"text\":{\"content\":\"object_placed\",\"font\":\"Helvetica\"}},\"labelOffset\":[-0.025,0],\"verticalAlignment\":\"middle\"},{\"horizontalAlignment\":\"center\",\"image\":{\"position\":[0.05,0.015,0.98,0.9],\"size\":[0.98,0.9],\"src\":\"data:image\\/svg+xml;base64,PHN2ZyB4bWxucz0iaHR0cDovL3d3dy53My5vcmcvMjAwMC9zdmciIHhtbG5zOnhsaW5rPSJodHRwOi8vd3d3LnczLm9yZy8xOTk5L3hsaW5rIiB2aWV3Qm94PSIwIDAgMTc3LjI1IDQwLjg4Ij48ZGVmcz48c3R5bGU+LmNscy0xe2ZpbGw6dXJsKCNyYWRpYWwtZ3JhZGllbnQpO30uY2xzLTJ7ZmlsbDp1cmwoI2xpbmVhci1ncmFkaWVudCk7fS5jbHMtM3tmaWxsOnVybCgjbGluZWFyLWdyYWRpZW50LTIpO308L3N0eWxlPjxyYWRpYWxHcmFkaWVudCBpZD0icmFkaWFsLWdyYWRpZW50IiBjeD0iOTAuMDkiIGN5PSIyMi42NiIgcj0i ...(+2216 chars)\",\"srcOrientation\":\"Right\"},\"label\":{\"color\":[1,1,0.78,1],\"icon\":{\"size\":[1.2,1.2],\"src\":\"data:image\\/svg+xml;base64,PHN2ZyBpZD0iT2ZmIiB4bWxucz0iaHR0cDovL3d3dy53My5vcmcvMjAwMC9zdmciIHhtbG5zOnhsaW5rPSJodHRwOi8vd3d3LnczLm9yZy8xOTk5L3hsaW5rIiB2aWV3Qm94PSIwIDAgNTAgNTAiPjxkZWZzPjxzdHlsZT4uY2xzLTF7ZmlsbDojN2Y4MDgwO3N0cm9rZTojMjcyNjI2O3N0cm9rZS1taXRlcmxpbWl0OjEwO3N0cm9rZS13aWR0aDozcHg7fS5jbHMtMntmaWxsOnVybCgjbGluZWFyLWdyYWRpZW50KTt9PC9zdHlsZT48bGluZWFyR3JhZGllbnQgaWQ9ImxpbmVhci1ncmFkaWVudCIgeDE9IjI1IiB5MT0iOSIgeDI9IjI1IiB5Mj0iMzciIGdyYWRpZW50VW5pdHM9InVzZXJTcGFjZU9uVXNlIj48c3RvcCBvZmZzZXQ9IjAiIHN0b3AtY29sb3I9IiNmZmYiIHN0b3Atb3BhY2l0eT0iMC43NSIvPjxzdG9wIG9mZnNldD0iMSIgc3RvcC1jb2xvcj0iI2ZmZiIgc3RvcC1vcGFjaXR5PSIwIi8+PC9saW5lYXJHcmFkaWVudD48L2RlZnM+PGNpcmNsZSBjbGFzcz0iY2xzLTEiIGN4PSIyNSIgY3k9IjI1IiByPSIyMCIvPjxjaXJjbGUgY2xhc3M9ImNscy0yIiBjeD0iMjUiIGN5PSIyMyIgcj0iMTQiLz48L3N2Zz4=\",\"srcOrientation\":\"Right\"},\"iconOffset\":0,\"iconPlacement\":\"left\",\"opacity\":1,\"show\":true,\"text\":{\"content\":\"object_placed\",\"font\":\"Helvetica\"}},\"labelOffset\":[0,0],\"verticalAlignment\":\"middle\"}]}},{\"name\":\"ForegroundImageComponent\",\"settings\":{\"image\":{\"size\":[0,0],\"src\":\"default\",\"srcOrientation\":\"horizontal\"},\"isForeground\":1,\"position\":[0,0,1,1],\"scaleMode\":\"0\"}}],\"derived\":{\"blockParameters\":{\"AutoActivate\":false,\"ButtonText\":\"   Object Placed\",\"ButtonType\":\"Momentary\",\"ClickFcn\":\"\",\"OnValue\":\"1\",\"PressDelay\":\"500\",\"PressFcn\":\"\",\"RepeatInterval\":\"0\",\"fixedAspectRatio\":\"on\"}},\"settings\":{\"BindingType\":\"param\",\"aspectRatio\":3.7777777777777777,\"autoActivate\":false,\"backgroundColor\":[0,0,0,\"1\"],\"backgroundOffset\":0,\"backgroundOpacity\":1,\"fixedAspectRatio\":\"on\",\"foregroundColor\":[252,252,196],\"showBackgroundColor\":false,\"variant\":\"push\",\"version\":\"R2025a\"},\"type\":\"Button\"}"
  Push Button13 : CustomTuningWebBlock  LabelPosition=Hide  ShowInitialText=on  Configuration="{\"components\":[{\"name\":\"BackgroundImageComponent\",\"settings\":{\"image\":{\"size\":[0,0],\"src\":\"default\",\"srcOrientation\":\"horizontal\"},\"position\":[0,0,1,1],\"scaleMode\":\"0\"}},{\"name\":\"ButtonStateComponent\",\"settings\":{\"buttonType\":\"momentary\",\"clickFcn\":\"\",\"image\":{\"size\":[180,45],\"srcOrientation\":\"Right\"},\"latched\":false,\"offValue\":[],\"onValue\":\"0\",\"position\":[0,0,1,1],\"pressDelay\":\"500\",\"pressFcn\":\"\",\"repeatInterval\":\"0\",\"states\":[{\"horizontalAlignment\":\"center\",\"image\":{\"position\":[0,0,1,1],\"size\":[1,1],\"src\":\"data:image\\/svg+xml;base64,PHN2ZyB3aWR0aD0iNDIwIiBoZWlnaHQ9IjEyMCIgdmlld0JveD0iMCAwIDQyMCAxMjAiIGZpbGw9Im5vbmUiIHhtbG5zPSJodHRwOi8vd3d3LnczLm9yZy8yMDAwL3N2ZyI+CiAgPGRlZnM+CiAgICA8bGluZWFyR3JhZGllbnQgaWQ9ImJnUmVtb3ZlZCIgeDE9IjAiIHkxPSIwIiB4Mj0iMCIgeTI9IjEyMCIgZ3JhZGllbnRVbml0cz0idXNlclNwYWNlT25Vc2UiPgogICAgICA8c3RvcCBvZmZzZXQ9IjAiIHN0b3AtY29sb3I9IiM2QTUzM0EiLz4KICAgICAgPHN0b3Agb2Zmc2V0PSIwLjUyIiBzdG9wLWNvbG9yPSIjNTY0MzJGIi8+ ...(+2696 chars)\",\"srcOrientation\":\"Right\"},\"label\":{\"color\":[1,1,0.78,1],\"icon\":{\"size\":[0,0],\"src\":\"default\",\"srcOrientation\":\"Right\"},\"iconOffset\":0,\"iconPlacement\":\"left\",\"opacity\":1,\"show\":true,\"text\":{\"content\":\"Object Removed\",\"font\":\"Helvetica\"}},\"labelOffset\":[0,0.12],\"verticalAlignment\":\"middle\"},{\"horizontalAlignment\":\"center\",\"image\":{\"position\":[0,0,1,1],\"size\":[1,1],\"src\":\"data:image\\/svg+xml;base64,PHN2ZyB3aWR0aD0iNDIwIiBoZWlnaHQ9IjEyMCIgdmlld0JveD0iMCAwIDQyMCAxMjAiIGZpbGw9Im5vbmUiIHhtbG5zPSJodHRwOi8vd3d3LnczLm9yZy8yMDAwL3N2ZyI+CiAgPGRlZnM+CiAgICA8bGluZWFyR3JhZGllbnQgaWQ9ImJnUmVtb3ZlZFByZXNzZWQiIHgxPSIwIiB5MT0iMCIgeDI9IjAiIHkyPSIxMjAiIGdyYWRpZW50VW5pdHM9InVzZXJTcGFjZU9uVXNlIj4KICAgICAgPHN0b3Agb2Zmc2V0PSIwIiBzdG9wLWNvbG9yPSIjQjg4QjU5Ii8+CiAgICAgIDxzdG9wIG9mZnNldD0iMC41MiIgc3RvcC1jb2xvcj0iIzlE ...(+2004 chars)\",\"srcOrientation\":\"Right\"},\"label\":{\"color\":[1,1,0.78,1],\"icon\":{\"size\":[0,0],\"src\":\"default\",\"srcOrientation\":\"Right\"},\"iconOffset\":0,\"iconPlacement\":\"left\",\"opacity\":1,\"show\":true,\"text\":{\"content\":\"Object Removed\",\"font\":\"Helvetica\"}},\"labelOffset\":[0,0.12],\"verticalAlignment\":\"middle\"},{\"horizontalAlignment\":\"center\",\"image\":{\"position\":[0.05,0.015,0.98,0.9],\"size\":[0.98,0.9],\"src\":\"data:image\\/svg+xml;base64,PHN2ZyB4bWxucz0iaHR0cDovL3d3dy53My5vcmcvMjAwMC9zdmciIHhtbG5zOnhsaW5rPSJodHRwOi8vd3d3LnczLm9yZy8xOTk5L3hsaW5rIiB2aWV3Qm94PSIwIDAgMTc3LjI1IDQwLjg4Ij48ZGVmcz48c3R5bGU+LmNscy0xe2ZpbGw6dXJsKCNyYWRpYWwtZ3JhZGllbnQpO30uY2xzLTJ7ZmlsbDp1cmwoI2xpbmVhci1ncmFkaWVudCk7fS5jbHMtM3tmaWxsOnVybCgjbGluZWFyLWdyYWRpZW50LTIpO308L3N0eWxlPjxyYWRpYWxHcmFkaWVudCBpZD0icmFkaWFsLWdyYWRpZW50IiBjeD0iOTAuMDkiIGN5PSIyMi42NiIgcj0i ...(+2212 chars)\",\"srcOrientation\":\"Right\"},\"label\":{\"color\":[1,1,0.78,1],\"icon\":{\"size\":[1.2,1.2],\"src\":\"data:image\\/svg+xml;base64,PHN2ZyB4bWxucz0iaHR0cDovL3d3dy53My5vcmcvMjAwMC9zdmciIHhtbG5zOnhsaW5rPSJodHRwOi8vd3d3LnczLm9yZy8xOTk5L3hsaW5rIiB2aWV3Qm94PSIwIDAgNTAgNTAiPjxkZWZzPjxzdHlsZT4uY2xzLTF7ZmlsbDojNmFiZDQ1O3N0cm9rZTojMjcyNjI2O3N0cm9rZS1taXRlcmxpbWl0OjEwO3N0cm9rZS13aWR0aDozcHg7fS5jbHMtMntmaWxsOnVybCgjbGluZWFyLWdyYWRpZW50KTt9PC9zdHlsZT48bGluZWFyR3JhZGllbnQgaWQ9ImxpbmVhci1ncmFkaWVudCIgeDE9IjI1IiB5MT0iOSIgeDI9IjI1IiB5Mj0iMzciIGdyYWRpZW50VW5pdHM9InVzZXJTcGFjZU9uVXNlIj48c3RvcCBvZmZzZXQ9IjAiIHN0b3AtY29sb3I9IiNmZmYiIHN0b3Atb3BhY2l0eT0iMC43NSIvPjxzdG9wIG9mZnNldD0iMSIgc3RvcC1jb2xvcj0iI2ZmZiIgc3RvcC1vcGFjaXR5PSIwIi8+PC9saW5lYXJHcmFkaWVudD48L2RlZnM+PGcgaWQ9Ik9uIj48Y2lyY2xlIGNsYXNzPSJjbHMtMSIgY3g9IjI1IiBjeT0iMjUiIHI9IjIwIi8+PGNpcmNsZSBjbGFzcz0iY2xzLTIiIGN4PSIyNSIgY3k9IjIzIiByPSIxNCIvPjwvZz48L3N2Zz4=\",\"srcOrientation\":\"Right\"},\"iconOffset\":0,\"iconPlacement\":\"left\",\"opacity\":1,\"show\":true,\"text\":{\"content\":\"object_removed\",\"font\":\"Helvetica\"}},\"labelOffset\":[-0.025,0],\"verticalAlignment\":\"middle\"},{\"horizontalAlignment\":\"center\",\"image\":{\"position\":[0.05,0.015,0.98,0.9],\"size\":[0.98,0.9],\"src\":\"data:image\\/svg+xml;base64,PHN2ZyB4bWxucz0iaHR0cDovL3d3dy53My5vcmcvMjAwMC9zdmciIHhtbG5zOnhsaW5rPSJodHRwOi8vd3d3LnczLm9yZy8xOTk5L3hsaW5rIiB2aWV3Qm94PSIwIDAgMTc3LjI1IDQwLjg4Ij48ZGVmcz48c3R5bGU+LmNscy0xe2ZpbGw6dXJsKCNyYWRpYWwtZ3JhZGllbnQpO30uY2xzLTJ7ZmlsbDp1cmwoI2xpbmVhci1ncmFkaWVudCk7fS5jbHMtM3tmaWxsOnVybCgjbGluZWFyLWdyYWRpZW50LTIpO308L3N0eWxlPjxyYWRpYWxHcmFkaWVudCBpZD0icmFkaWFsLWdyYWRpZW50IiBjeD0iOTAuMDkiIGN5PSIyMi42NiIgcj0i ...(+2216 chars)\",\"srcOrientation\":\"Right\"},\"label\":{\"color\":[1,1,0.78,1],\"icon\":{\"size\":[1.2,1.2],\"src\":\"data:image\\/svg+xml;base64,PHN2ZyBpZD0iT2ZmIiB4bWxucz0iaHR0cDovL3d3dy53My5vcmcvMjAwMC9zdmciIHhtbG5zOnhsaW5rPSJodHRwOi8vd3d3LnczLm9yZy8xOTk5L3hsaW5rIiB2aWV3Qm94PSIwIDAgNTAgNTAiPjxkZWZzPjxzdHlsZT4uY2xzLTF7ZmlsbDojN2Y4MDgwO3N0cm9rZTojMjcyNjI2O3N0cm9rZS1taXRlcmxpbWl0OjEwO3N0cm9rZS13aWR0aDozcHg7fS5jbHMtMntmaWxsOnVybCgjbGluZWFyLWdyYWRpZW50KTt9PC9zdHlsZT48bGluZWFyR3JhZGllbnQgaWQ9ImxpbmVhci1ncmFkaWVudCIgeDE9IjI1IiB5MT0iOSIgeDI9IjI1IiB5Mj0iMzciIGdyYWRpZW50VW5pdHM9InVzZXJTcGFjZU9uVXNlIj48c3RvcCBvZmZzZXQ9IjAiIHN0b3AtY29sb3I9IiNmZmYiIHN0b3Atb3BhY2l0eT0iMC43NSIvPjxzdG9wIG9mZnNldD0iMSIgc3RvcC1jb2xvcj0iI2ZmZiIgc3RvcC1vcGFjaXR5PSIwIi8+PC9saW5lYXJHcmFkaWVudD48L2RlZnM+PGNpcmNsZSBjbGFzcz0iY2xzLTEiIGN4PSIyNSIgY3k9IjI1IiByPSIyMCIvPjxjaXJjbGUgY2xhc3M9ImNscy0yIiBjeD0iMjUiIGN5PSIyMyIgcj0iMTQiLz48L3N2Zz4=\",\"srcOrientation\":\"Right\"},\"iconOffset\":0,\"iconPlacement\":\"left\",\"opacity\":1,\"show\":true,\"text\":{\"content\":\"object_removed\",\"font\":\"Helvetica\"}},\"labelOffset\":[0,0],\"verticalAlignment\":\"middle\"}]}},{\"name\":\"ForegroundImageComponent\",\"settings\":{\"image\":{\"size\":[0,0],\"src\":\"default\",\"srcOrientation\":\"horizontal\"},\"isForeground\":1,\"position\":[0,0,1,1],\"scaleMode\":\"0\"}}],\"derived\":{\"blockParameters\":{\"AutoActivate\":false,\"ButtonText\":\"Object Removed\",\"ButtonType\":\"Momentary\",\"ClickFcn\":\"\",\"OnValue\":\"0\",\"PressDelay\":\"500\",\"PressFcn\":\"\",\"RepeatInterval\":\"0\",\"fixedAspectRatio\":\"on\"}},\"settings\":{\"BindingType\":\"param\",\"aspectRatio\":3.7777777777777777,\"autoActivate\":false,\"backgroundColor\":[0,0,0,\"1\"],\"backgroundOffset\":0,\"backgroundOpacity\":1,\"fixedAspectRatio\":\"on\",\"foregroundColor\":[252,252,196],\"showBackgroundColor\":false,\"variant\":\"push\",\"version\":\"R2025a\"},\"type\":\"Button\"}"
  Push Button14 : CustomTuningWebBlock  LabelPosition=Hide  ShowInitialText=on  Configuration="{\"components\":[{\"name\":\"BackgroundImageComponent\",\"settings\":{\"image\":{\"size\":[0,0],\"src\":\"default\",\"srcOrientation\":\"horizontal\"},\"position\":[0,0,1,1],\"scaleMode\":\"0\"}},{\"name\":\"ButtonStateComponent\",\"settings\":{\"buttonType\":\"momentary\",\"clickFcn\":\"\",\"image\":{\"size\":[180,45],\"srcOrientation\":\"Right\"},\"latched\":false,\"offValue\":[],\"onValue\":\"1\",\"position\":[0,0,1,1],\"pressDelay\":\"500\",\"pressFcn\":\"\",\"repeatInterval\":\"0\",\"states\":[{\"horizontalAlignment\":\"center\",\"image\":{\"position\":[0.05,0.015,0.98,0.9],\"size\":[0.98,0.9],\"src\":\"data:image\\/svg+xml;base64,PHN2ZyB4bWxucz0iaHR0cDovL3d3dy53My5vcmcvMjAwMC9zdmciIHhtbG5zOnhsaW5rPSJodHRwOi8vd3d3LnczLm9yZy8xOTk5L3hsaW5rIiB2aWV3Qm94PSIwIDAgMTc3LjI1IDQwLjg4Ij48ZGVmcz48c3R5bGU+LmNscy0xe2ZpbGw6dXJsKCNyYWRpYWwtZ3JhZGllbnQpO30uY2xzLTJ7ZmlsbDp1cmwoI2xpbmVhci1ncmFkaWVudCk7fS5jbHMtM3tmaWxsOnVybCgjbGluZWFyLWdyYWRpZW50LTIpO308L3N0eWxlPjxyYWRpYWxHcmFkaWVudCBpZD0icmFkaWFsLWdyYWRpZW50IiBjeD0iOTAuMDkiIGN5PSIyMi42NiIgcj0i ...(+2212 chars)\",\"srcOrientation\":\"Right\"},\"label\":{\"color\":[1,1,0.78,1],\"icon\":{\"size\":[1.2,1.2],\"src\":\"data:image\\/svg+xml;base64,PHN2ZyBpZD0iT2ZmIiB4bWxucz0iaHR0cDovL3d3dy53My5vcmcvMjAwMC9zdmciIHhtbG5zOnhsaW5rPSJodHRwOi8vd3d3LnczLm9yZy8xOTk5L3hsaW5rIiB2aWV3Qm94PSIwIDAgNTAgNTAiPjxkZWZzPjxzdHlsZT4uY2xzLTF7ZmlsbDojN2Y4MDgwO3N0cm9rZTojMjcyNjI2O3N0cm9rZS1taXRlcmxpbWl0OjEwO3N0cm9rZS13aWR0aDozcHg7fS5jbHMtMntmaWxsOnVybCgjbGluZWFyLWdyYWRpZW50KTt9PC9zdHlsZT48bGluZWFyR3JhZGllbnQgaWQ9ImxpbmVhci1ncmFkaWVudCIgeDE9IjI1IiB5MT0iOSIgeDI9IjI1IiB5Mj0iMzciIGdyYWRpZW50VW5pdHM9InVzZXJTcGFjZU9uVXNlIj48c3RvcCBvZmZzZXQ9IjAiIHN0b3AtY29sb3I9IiNmZmYiIHN0b3Atb3BhY2l0eT0iMC43NSIvPjxzdG9wIG9mZnNldD0iMSIgc3RvcC1jb2xvcj0iI2ZmZiIgc3RvcC1vcGFjaXR5PSIwIi8+PC9saW5lYXJHcmFkaWVudD48L2RlZnM+PGNpcmNsZSBjbGFzcz0iY2xzLTEiIGN4PSIyNSIgY3k9IjI1IiByPSIyMCIvPjxjaXJjbGUgY2xhc3M9ImNscy0yIiBjeD0iMjUiIGN5PSIyMyIgcj0iMTQiLz48L3N2Zz4=\",\"srcOrientation\":\"Right\"},\"iconOffset\":0,\"iconPlacement\":\"left\",\"opacity\":1,\"show\":true,\"text\":{\"content\":\"Scan 1\",\"font\":\"Helvetica\"}},\"labelOffset\":[-0.025,0],\"verticalAlignment\":\"middle\"},{\"horizontalAlignment\":\"center\",\"image\":{\"position\":[0.05,0.015,0.98,0.9],\"size\":[0.98,0.9],\"src\":\"data:image\\/svg+xml;base64,PHN2ZyB4bWxucz0iaHR0cDovL3d3dy53My5vcmcvMjAwMC9zdmciIHhtbG5zOnhsaW5rPSJodHRwOi8vd3d3LnczLm9yZy8xOTk5L3hsaW5rIiB2aWV3Qm94PSIwIDAgMTc3LjI1IDQwLjg4Ij48ZGVmcz48c3R5bGU+LmNscy0xe2ZpbGw6dXJsKCNyYWRpYWwtZ3JhZGllbnQpO30uY2xzLTJ7ZmlsbDp1cmwoI2xpbmVhci1ncmFkaWVudCk7fS5jbHMtM3tmaWxsOnVybCgjbGluZWFyLWdyYWRpZW50LTIpO308L3N0eWxlPjxyYWRpYWxHcmFkaWVudCBpZD0icmFkaWFsLWdyYWRpZW50IiBjeD0iOTAuMDkiIGN5PSIyMi42NiIgcj0i ...(+2216 chars)\",\"srcOrientation\":\"Right\"},\"label\":{\"color\":[1,1,0.78,1],\"icon\":{\"size\":[1.2,1.2],\"src\":\"data:image\\/svg+xml;base64,PHN2ZyB4bWxucz0iaHR0cDovL3d3dy53My5vcmcvMjAwMC9zdmciIHhtbG5zOnhsaW5rPSJodHRwOi8vd3d3LnczLm9yZy8xOTk5L3hsaW5rIiB2aWV3Qm94PSIwIDAgNTAgNTAiPjxkZWZzPjxzdHlsZT4uY2xzLTF7ZmlsbDojNmFiZDQ1O3N0cm9rZTojMjcyNjI2O3N0cm9rZS1taXRlcmxpbWl0OjEwO3N0cm9rZS13aWR0aDozcHg7fS5jbHMtMntmaWxsOnVybCgjbGluZWFyLWdyYWRpZW50KTt9PC9zdHlsZT48bGluZWFyR3JhZGllbnQgaWQ9ImxpbmVhci1ncmFkaWVudCIgeDE9IjI1IiB5MT0iOSIgeDI9IjI1IiB5Mj0iMzciIGdyYWRpZW50VW5pdHM9InVzZXJTcGFjZU9uVXNlIj48c3RvcCBvZmZzZXQ9IjAiIHN0b3AtY29sb3I9IiNmZmYiIHN0b3Atb3BhY2l0eT0iMC43NSIvPjxzdG9wIG9mZnNldD0iMSIgc3RvcC1jb2xvcj0iI2ZmZiIgc3RvcC1vcGFjaXR5PSIwIi8+PC9saW5lYXJHcmFkaWVudD48L2RlZnM+PGcgaWQ9Ik9uIj48Y2lyY2xlIGNsYXNzPSJjbHMtMSIgY3g9IjI1IiBjeT0iMjUiIHI9IjIwIi8+PGNpcmNsZSBjbGFzcz0iY2xzLTIiIGN4PSIyNSIgY3k9IjIzIiByPSIxNCIvPjwvZz48L3N2Zz4=\",\"srcOrientation\":\"Right\"},\"iconOffset\":0,\"iconPlacement\":\"left\",\"opacity\":1,\"show\":true,\"text\":{\"content\":\"Scan 1\",\"font\":\"Helvetica\"}},\"labelOffset\":[0,0],\"verticalAlignment\":\"middle\"},{\"horizontalAlignment\":\"center\",\"image\":{\"position\":[0.05,0.015,0.98,0.9],\"size\":[0.98,0.9],\"src\":\"data:image\\/svg+xml;base64,PHN2ZyB4bWxucz0iaHR0cDovL3d3dy53My5vcmcvMjAwMC9zdmciIHhtbG5zOnhsaW5rPSJodHRwOi8vd3d3LnczLm9yZy8xOTk5L3hsaW5rIiB2aWV3Qm94PSIwIDAgMTc3LjI1IDQwLjg4Ij48ZGVmcz48c3R5bGU+LmNscy0xe2ZpbGw6dXJsKCNyYWRpYWwtZ3JhZGllbnQpO30uY2xzLTJ7ZmlsbDp1cmwoI2xpbmVhci1ncmFkaWVudCk7fS5jbHMtM3tmaWxsOnVybCgjbGluZWFyLWdyYWRpZW50LTIpO308L3N0eWxlPjxyYWRpYWxHcmFkaWVudCBpZD0icmFkaWFsLWdyYWRpZW50IiBjeD0iOTAuMDkiIGN5PSIyMi42NiIgcj0i ...(+2212 chars)\",\"srcOrientation\":\"Right\"},\"label\":{\"color\":[1,1,0.78,1],\"icon\":{\"size\":[1.2,1.2],\"src\":\"data:image\\/svg+xml;base64,PHN2ZyB4bWxucz0iaHR0cDovL3d3dy53My5vcmcvMjAwMC9zdmciIHhtbG5zOnhsaW5rPSJodHRwOi8vd3d3LnczLm9yZy8xOTk5L3hsaW5rIiB2aWV3Qm94PSIwIDAgNTAgNTAiPjxkZWZzPjxzdHlsZT4uY2xzLTF7ZmlsbDojNmFiZDQ1O3N0cm9rZTojMjcyNjI2O3N0cm9rZS1taXRlcmxpbWl0OjEwO3N0cm9rZS13aWR0aDozcHg7fS5jbHMtMntmaWxsOnVybCgjbGluZWFyLWdyYWRpZW50KTt9PC9zdHlsZT48bGluZWFyR3JhZGllbnQgaWQ9ImxpbmVhci1ncmFkaWVudCIgeDE9IjI1IiB5MT0iOSIgeDI9IjI1IiB5Mj0iMzciIGdyYWRpZW50VW5pdHM9InVzZXJTcGFjZU9uVXNlIj48c3RvcCBvZmZzZXQ9IjAiIHN0b3AtY29sb3I9IiNmZmYiIHN0b3Atb3BhY2l0eT0iMC43NSIvPjxzdG9wIG9mZnNldD0iMSIgc3RvcC1jb2xvcj0iI2ZmZiIgc3RvcC1vcGFjaXR5PSIwIi8+PC9saW5lYXJHcmFkaWVudD48L2RlZnM+PGcgaWQ9Ik9uIj48Y2lyY2xlIGNsYXNzPSJjbHMtMSIgY3g9IjI1IiBjeT0iMjUiIHI9IjIwIi8+PGNpcmNsZSBjbGFzcz0iY2xzLTIiIGN4PSIyNSIgY3k9IjIzIiByPSIxNCIvPjwvZz48L3N2Zz4=\",\"srcOrientation\":\"Right\"},\"iconOffset\":0,\"iconPlacement\":\"left\",\"opacity\":1,\"show\":true,\"text\":{\"content\":\"Scan 1\",\"font\":\"Helvetica\"}},\"labelOffset\":[-0.025,0],\"verticalAlignment\":\"middle\"},{\"horizontalAlignment\":\"center\",\"image\":{\"position\":[0.05,0.015,0.98,0.9],\"size\":[0.98,0.9],\"src\":\"data:image\\/svg+xml;base64,PHN2ZyB4bWxucz0iaHR0cDovL3d3dy53My5vcmcvMjAwMC9zdmciIHhtbG5zOnhsaW5rPSJodHRwOi8vd3d3LnczLm9yZy8xOTk5L3hsaW5rIiB2aWV3Qm94PSIwIDAgMTc3LjI1IDQwLjg4Ij48ZGVmcz48c3R5bGU+LmNscy0xe2ZpbGw6dXJsKCNyYWRpYWwtZ3JhZGllbnQpO30uY2xzLTJ7ZmlsbDp1cmwoI2xpbmVhci1ncmFkaWVudCk7fS5jbHMtM3tmaWxsOnVybCgjbGluZWFyLWdyYWRpZW50LTIpO308L3N0eWxlPjxyYWRpYWxHcmFkaWVudCBpZD0icmFkaWFsLWdyYWRpZW50IiBjeD0iOTAuMDkiIGN5PSIyMi42NiIgcj0i ...(+2216 chars)\",\"srcOrientation\":\"Right\"},\"label\":{\"color\":[1,1,0.78,1],\"icon\":{\"size\":[1.2,1.2],\"src\":\"data:image\\/svg+xml;base64,PHN2ZyBpZD0iT2ZmIiB4bWxucz0iaHR0cDovL3d3dy53My5vcmcvMjAwMC9zdmciIHhtbG5zOnhsaW5rPSJodHRwOi8vd3d3LnczLm9yZy8xOTk5L3hsaW5rIiB2aWV3Qm94PSIwIDAgNTAgNTAiPjxkZWZzPjxzdHlsZT4uY2xzLTF7ZmlsbDojN2Y4MDgwO3N0cm9rZTojMjcyNjI2O3N0cm9rZS1taXRlcmxpbWl0OjEwO3N0cm9rZS13aWR0aDozcHg7fS5jbHMtMntmaWxsOnVybCgjbGluZWFyLWdyYWRpZW50KTt9PC9zdHlsZT48bGluZWFyR3JhZGllbnQgaWQ9ImxpbmVhci1ncmFkaWVudCIgeDE9IjI1IiB5MT0iOSIgeDI9IjI1IiB5Mj0iMzciIGdyYWRpZW50VW5pdHM9InVzZXJTcGFjZU9uVXNlIj48c3RvcCBvZmZzZXQ9IjAiIHN0b3AtY29sb3I9IiNmZmYiIHN0b3Atb3BhY2l0eT0iMC43NSIvPjxzdG9wIG9mZnNldD0iMSIgc3RvcC1jb2xvcj0iI2ZmZiIgc3RvcC1vcGFjaXR5PSIwIi8+PC9saW5lYXJHcmFkaWVudD48L2RlZnM+PGNpcmNsZSBjbGFzcz0iY2xzLTEiIGN4PSIyNSIgY3k9IjI1IiByPSIyMCIvPjxjaXJjbGUgY2xhc3M9ImNscy0yIiBjeD0iMjUiIGN5PSIyMyIgcj0iMTQiLz48L3N2Zz4=\",\"srcOrientation\":\"Right\"},\"iconOffset\":0,\"iconPlacement\":\"left\",\"opacity\":1,\"show\":true,\"text\":{\"content\":\"Scan 1\",\"font\":\"Helvetica\"}},\"labelOffset\":[0,0],\"verticalAlignment\":\"middle\"}]}},{\"name\":\"ForegroundImageComponent\",\"settings\":{\"image\":{\"size\":[0,0],\"src\":\"default\",\"srcOrientation\":\"horizontal\"},\"isForeground\":1,\"position\":[0,0,1,1],\"scaleMode\":\"0\"}}],\"derived\":{\"blockParameters\":{\"AutoActivate\":false,\"ButtonText\":\"Scan 1\",\"ButtonType\":\"Momentary\",\"ClickFcn\":\"\",\"OnValue\":\"1\",\"PressDelay\":\"500\",\"PressFcn\":\"\",\"RepeatInterval\":\"0\",\"fixedAspectRatio\":\"on\"}},\"settings\":{\"BindingType\":\"param\",\"aspectRatio\":3.7777777777777777,\"autoActivate\":false,\"backgroundColor\":[0,0,0,\"1\"],\"backgroundOffset\":0,\"backgroundOpacity\":1,\"fixedAspectRatio\":\"on\",\"foregroundColor\":[252,252,196],\"showBackgroundColor\":false,\"variant\":\"push\",\"version\":\"R2025a\"},\"type\":\"Button\"}"
  Push Button15 : CustomTuningWebBlock  LabelPosition=Hide  ShowInitialText=on  Configuration="{\"components\":[{\"name\":\"BackgroundImageComponent\",\"settings\":{\"image\":{\"size\":[0,0],\"src\":\"default\",\"srcOrientation\":\"horizontal\"},\"position\":[0,0,1,1],\"scaleMode\":\"0\"}},{\"name\":\"ButtonStateComponent\",\"settings\":{\"buttonType\":\"momentary\",\"clickFcn\":\"\",\"image\":{\"size\":[180,45],\"srcOrientation\":\"Right\"},\"latched\":false,\"offValue\":[],\"onValue\":\"2\",\"position\":[0,0,1,1],\"pressDelay\":\"500\",\"pressFcn\":\"\",\"repeatInterval\":\"0\",\"states\":[{\"horizontalAlignment\":\"center\",\"image\":{\"position\":[0.05,0.015,0.98,0.9],\"size\":[0.98,0.9],\"src\":\"data:image\\/svg+xml;base64,PHN2ZyB4bWxucz0iaHR0cDovL3d3dy53My5vcmcvMjAwMC9zdmciIHhtbG5zOnhsaW5rPSJodHRwOi8vd3d3LnczLm9yZy8xOTk5L3hsaW5rIiB2aWV3Qm94PSIwIDAgMTc3LjI1IDQwLjg4Ij48ZGVmcz48c3R5bGU+LmNscy0xe2ZpbGw6dXJsKCNyYWRpYWwtZ3JhZGllbnQpO30uY2xzLTJ7ZmlsbDp1cmwoI2xpbmVhci1ncmFkaWVudCk7fS5jbHMtM3tmaWxsOnVybCgjbGluZWFyLWdyYWRpZW50LTIpO308L3N0eWxlPjxyYWRpYWxHcmFkaWVudCBpZD0icmFkaWFsLWdyYWRpZW50IiBjeD0iOTAuMDkiIGN5PSIyMi42NiIgcj0i ...(+2212 chars)\",\"srcOrientation\":\"Right\"},\"label\":{\"color\":[1,1,0.78,1],\"icon\":{\"size\":[1.2,1.2],\"src\":\"data:image\\/svg+xml;base64,PHN2ZyBpZD0iT2ZmIiB4bWxucz0iaHR0cDovL3d3dy53My5vcmcvMjAwMC9zdmciIHhtbG5zOnhsaW5rPSJodHRwOi8vd3d3LnczLm9yZy8xOTk5L3hsaW5rIiB2aWV3Qm94PSIwIDAgNTAgNTAiPjxkZWZzPjxzdHlsZT4uY2xzLTF7ZmlsbDojN2Y4MDgwO3N0cm9rZTojMjcyNjI2O3N0cm9rZS1taXRlcmxpbWl0OjEwO3N0cm9rZS13aWR0aDozcHg7fS5jbHMtMntmaWxsOnVybCgjbGluZWFyLWdyYWRpZW50KTt9PC9zdHlsZT48bGluZWFyR3JhZGllbnQgaWQ9ImxpbmVhci1ncmFkaWVudCIgeDE9IjI1IiB5MT0iOSIgeDI9IjI1IiB5Mj0iMzciIGdyYWRpZW50VW5pdHM9InVzZXJTcGFjZU9uVXNlIj48c3RvcCBvZmZzZXQ9IjAiIHN0b3AtY29sb3I9IiNmZmYiIHN0b3Atb3BhY2l0eT0iMC43NSIvPjxzdG9wIG9mZnNldD0iMSIgc3RvcC1jb2xvcj0iI2ZmZiIgc3RvcC1vcGFjaXR5PSIwIi8+PC9saW5lYXJHcmFkaWVudD48L2RlZnM+PGNpcmNsZSBjbGFzcz0iY2xzLTEiIGN4PSIyNSIgY3k9IjI1IiByPSIyMCIvPjxjaXJjbGUgY2xhc3M9ImNscy0yIiBjeD0iMjUiIGN5PSIyMyIgcj0iMTQiLz48L3N2Zz4=\",\"srcOrientation\":\"Right\"},\"iconOffset\":0,\"iconPlacement\":\"left\",\"opacity\":1,\"show\":true,\"text\":{\"content\":\"Scan 2\",\"font\":\"Helvetica\"}},\"labelOffset\":[-0.025,0],\"verticalAlignment\":\"middle\"},{\"horizontalAlignment\":\"center\",\"image\":{\"position\":[0.05,0.015,0.98,0.9],\"size\":[0.98,0.9],\"src\":\"data:image\\/svg+xml;base64,PHN2ZyB4bWxucz0iaHR0cDovL3d3dy53My5vcmcvMjAwMC9zdmciIHhtbG5zOnhsaW5rPSJodHRwOi8vd3d3LnczLm9yZy8xOTk5L3hsaW5rIiB2aWV3Qm94PSIwIDAgMTc3LjI1IDQwLjg4Ij48ZGVmcz48c3R5bGU+LmNscy0xe2ZpbGw6dXJsKCNyYWRpYWwtZ3JhZGllbnQpO30uY2xzLTJ7ZmlsbDp1cmwoI2xpbmVhci1ncmFkaWVudCk7fS5jbHMtM3tmaWxsOnVybCgjbGluZWFyLWdyYWRpZW50LTIpO308L3N0eWxlPjxyYWRpYWxHcmFkaWVudCBpZD0icmFkaWFsLWdyYWRpZW50IiBjeD0iOTAuMDkiIGN5PSIyMi42NiIgcj0i ...(+2216 chars)\",\"srcOrientation\":\"Right\"},\"label\":{\"color\":[1,1,0.78,1],\"icon\":{\"size\":[1.2,1.2],\"src\":\"data:image\\/svg+xml;base64,PHN2ZyB4bWxucz0iaHR0cDovL3d3dy53My5vcmcvMjAwMC9zdmciIHhtbG5zOnhsaW5rPSJodHRwOi8vd3d3LnczLm9yZy8xOTk5L3hsaW5rIiB2aWV3Qm94PSIwIDAgNTAgNTAiPjxkZWZzPjxzdHlsZT4uY2xzLTF7ZmlsbDojNmFiZDQ1O3N0cm9rZTojMjcyNjI2O3N0cm9rZS1taXRlcmxpbWl0OjEwO3N0cm9rZS13aWR0aDozcHg7fS5jbHMtMntmaWxsOnVybCgjbGluZWFyLWdyYWRpZW50KTt9PC9zdHlsZT48bGluZWFyR3JhZGllbnQgaWQ9ImxpbmVhci1ncmFkaWVudCIgeDE9IjI1IiB5MT0iOSIgeDI9IjI1IiB5Mj0iMzciIGdyYWRpZW50VW5pdHM9InVzZXJTcGFjZU9uVXNlIj48c3RvcCBvZmZzZXQ9IjAiIHN0b3AtY29sb3I9IiNmZmYiIHN0b3Atb3BhY2l0eT0iMC43NSIvPjxzdG9wIG9mZnNldD0iMSIgc3RvcC1jb2xvcj0iI2ZmZiIgc3RvcC1vcGFjaXR5PSIwIi8+PC9saW5lYXJHcmFkaWVudD48L2RlZnM+PGcgaWQ9Ik9uIj48Y2lyY2xlIGNsYXNzPSJjbHMtMSIgY3g9IjI1IiBjeT0iMjUiIHI9IjIwIi8+PGNpcmNsZSBjbGFzcz0iY2xzLTIiIGN4PSIyNSIgY3k9IjIzIiByPSIxNCIvPjwvZz48L3N2Zz4=\",\"srcOrientation\":\"Right\"},\"iconOffset\":0,\"iconPlacement\":\"left\",\"opacity\":1,\"show\":true,\"text\":{\"content\":\"Scan 2\",\"font\":\"Helvetica\"}},\"labelOffset\":[0,0],\"verticalAlignment\":\"middle\"},{\"horizontalAlignment\":\"center\",\"image\":{\"position\":[0.05,0.015,0.98,0.9],\"size\":[0.98,0.9],\"src\":\"data:image\\/svg+xml;base64,PHN2ZyB4bWxucz0iaHR0cDovL3d3dy53My5vcmcvMjAwMC9zdmciIHhtbG5zOnhsaW5rPSJodHRwOi8vd3d3LnczLm9yZy8xOTk5L3hsaW5rIiB2aWV3Qm94PSIwIDAgMTc3LjI1IDQwLjg4Ij48ZGVmcz48c3R5bGU+LmNscy0xe2ZpbGw6dXJsKCNyYWRpYWwtZ3JhZGllbnQpO30uY2xzLTJ7ZmlsbDp1cmwoI2xpbmVhci1ncmFkaWVudCk7fS5jbHMtM3tmaWxsOnVybCgjbGluZWFyLWdyYWRpZW50LTIpO308L3N0eWxlPjxyYWRpYWxHcmFkaWVudCBpZD0icmFkaWFsLWdyYWRpZW50IiBjeD0iOTAuMDkiIGN5PSIyMi42NiIgcj0i ...(+2212 chars)\",\"srcOrientation\":\"Right\"},\"label\":{\"color\":[1,1,0.78,1],\"icon\":{\"size\":[1.2,1.2],\"src\":\"data:image\\/svg+xml;base64,PHN2ZyB4bWxucz0iaHR0cDovL3d3dy53My5vcmcvMjAwMC9zdmciIHhtbG5zOnhsaW5rPSJodHRwOi8vd3d3LnczLm9yZy8xOTk5L3hsaW5rIiB2aWV3Qm94PSIwIDAgNTAgNTAiPjxkZWZzPjxzdHlsZT4uY2xzLTF7ZmlsbDojNmFiZDQ1O3N0cm9rZTojMjcyNjI2O3N0cm9rZS1taXRlcmxpbWl0OjEwO3N0cm9rZS13aWR0aDozcHg7fS5jbHMtMntmaWxsOnVybCgjbGluZWFyLWdyYWRpZW50KTt9PC9zdHlsZT48bGluZWFyR3JhZGllbnQgaWQ9ImxpbmVhci1ncmFkaWVudCIgeDE9IjI1IiB5MT0iOSIgeDI9IjI1IiB5Mj0iMzciIGdyYWRpZW50VW5pdHM9InVzZXJTcGFjZU9uVXNlIj48c3RvcCBvZmZzZXQ9IjAiIHN0b3AtY29sb3I9IiNmZmYiIHN0b3Atb3BhY2l0eT0iMC43NSIvPjxzdG9wIG9mZnNldD0iMSIgc3RvcC1jb2xvcj0iI2ZmZiIgc3RvcC1vcGFjaXR5PSIwIi8+PC9saW5lYXJHcmFkaWVudD48L2RlZnM+PGcgaWQ9Ik9uIj48Y2lyY2xlIGNsYXNzPSJjbHMtMSIgY3g9IjI1IiBjeT0iMjUiIHI9IjIwIi8+PGNpcmNsZSBjbGFzcz0iY2xzLTIiIGN4PSIyNSIgY3k9IjIzIiByPSIxNCIvPjwvZz48L3N2Zz4=\",\"srcOrientation\":\"Right\"},\"iconOffset\":0,\"iconPlacement\":\"left\",\"opacity\":1,\"show\":true,\"text\":{\"content\":\"Scan 2\",\"font\":\"Helvetica\"}},\"labelOffset\":[-0.025,0],\"verticalAlignment\":\"middle\"},{\"horizontalAlignment\":\"center\",\"image\":{\"position\":[0.05,0.015,0.98,0.9],\"size\":[0.98,0.9],\"src\":\"data:image\\/svg+xml;base64,PHN2ZyB4bWxucz0iaHR0cDovL3d3dy53My5vcmcvMjAwMC9zdmciIHhtbG5zOnhsaW5rPSJodHRwOi8vd3d3LnczLm9yZy8xOTk5L3hsaW5rIiB2aWV3Qm94PSIwIDAgMTc3LjI1IDQwLjg4Ij48ZGVmcz48c3R5bGU+LmNscy0xe2ZpbGw6dXJsKCNyYWRpYWwtZ3JhZGllbnQpO30uY2xzLTJ7ZmlsbDp1cmwoI2xpbmVhci1ncmFkaWVudCk7fS5jbHMtM3tmaWxsOnVybCgjbGluZWFyLWdyYWRpZW50LTIpO308L3N0eWxlPjxyYWRpYWxHcmFkaWVudCBpZD0icmFkaWFsLWdyYWRpZW50IiBjeD0iOTAuMDkiIGN5PSIyMi42NiIgcj0i ...(+2216 chars)\",\"srcOrientation\":\"Right\"},\"label\":{\"color\":[1,1,0.78,1],\"icon\":{\"size\":[1.2,1.2],\"src\":\"data:image\\/svg+xml;base64,PHN2ZyBpZD0iT2ZmIiB4bWxucz0iaHR0cDovL3d3dy53My5vcmcvMjAwMC9zdmciIHhtbG5zOnhsaW5rPSJodHRwOi8vd3d3LnczLm9yZy8xOTk5L3hsaW5rIiB2aWV3Qm94PSIwIDAgNTAgNTAiPjxkZWZzPjxzdHlsZT4uY2xzLTF7ZmlsbDojN2Y4MDgwO3N0cm9rZTojMjcyNjI2O3N0cm9rZS1taXRlcmxpbWl0OjEwO3N0cm9rZS13aWR0aDozcHg7fS5jbHMtMntmaWxsOnVybCgjbGluZWFyLWdyYWRpZW50KTt9PC9zdHlsZT48bGluZWFyR3JhZGllbnQgaWQ9ImxpbmVhci1ncmFkaWVudCIgeDE9IjI1IiB5MT0iOSIgeDI9IjI1IiB5Mj0iMzciIGdyYWRpZW50VW5pdHM9InVzZXJTcGFjZU9uVXNlIj48c3RvcCBvZmZzZXQ9IjAiIHN0b3AtY29sb3I9IiNmZmYiIHN0b3Atb3BhY2l0eT0iMC43NSIvPjxzdG9wIG9mZnNldD0iMSIgc3RvcC1jb2xvcj0iI2ZmZiIgc3RvcC1vcGFjaXR5PSIwIi8+PC9saW5lYXJHcmFkaWVudD48L2RlZnM+PGNpcmNsZSBjbGFzcz0iY2xzLTEiIGN4PSIyNSIgY3k9IjI1IiByPSIyMCIvPjxjaXJjbGUgY2xhc3M9ImNscy0yIiBjeD0iMjUiIGN5PSIyMyIgcj0iMTQiLz48L3N2Zz4=\",\"srcOrientation\":\"Right\"},\"iconOffset\":0,\"iconPlacement\":\"left\",\"opacity\":1,\"show\":true,\"text\":{\"content\":\"Scan 2\",\"font\":\"Helvetica\"}},\"labelOffset\":[0,0],\"verticalAlignment\":\"middle\"}]}},{\"name\":\"ForegroundImageComponent\",\"settings\":{\"image\":{\"size\":[0,0],\"src\":\"default\",\"srcOrientation\":\"horizontal\"},\"isForeground\":1,\"position\":[0,0,1,1],\"scaleMode\":\"0\"}}],\"derived\":{\"blockParameters\":{\"AutoActivate\":false,\"ButtonText\":\"Scan 2\",\"ButtonType\":\"Momentary\",\"ClickFcn\":\"\",\"OnValue\":\"2\",\"PressDelay\":\"500\",\"PressFcn\":\"\",\"RepeatInterval\":\"0\",\"fixedAspectRatio\":\"on\"}},\"settings\":{\"BindingType\":\"param\",\"aspectRatio\":3.7777777777777777,\"autoActivate\":false,\"backgroundColor\":[0,0,0,\"1\"],\"backgroundOffset\":0,\"backgroundOpacity\":1,\"fixedAspectRatio\":\"on\",\"foregroundColor\":[252,252,196],\"showBackgroundColor\":false,\"variant\":\"push\",\"version\":\"R2025a\"},\"type\":\"Button\"}"
